simulink model "final"  (R2020a)
(part 7 of 10)

  "IW{1,1}(873,:)'" : Constant  Value=[-9.8027652668789784229375072754919528961181640625;-8.181515964342761293437433778308331966400146484375;5.7461951088779432694764182087965309619903564453125]
      mask Display: e = 0.06;c1 = [120 150 230]/255;c2 = ([120 150 230]+0)/383;c3 = ([120 150 230]+128)/383;patch([0 1 1 0],[0 0 1 1],c1);patch([0 1 1 1-e 1-e 0+e],[0 0 1 1-e 0+e 0+e],c2);patch([0 0 1 1-e 0+e 0+e],[0 1 1 1-e 1-e 0+e],c3);plot([0 1 1 0 0],[0 0 1 1 0]);disp('Weights');
  "IW{1,1}(874,:)'" : Constant  Value=[-5.7445898955294705245933073456399142742156982421875;11.1345368451311177437901278608478605747222900390625;-6.17189644151374494640549528412520885467529296875]
      mask Display: e = 0.06;c1 = [120 150 230]/255;c2 = ([120 150 230]+0)/383;c3 = ([120 150 230]+128)/383;patch([0 1 1 0],[0 0 1 1],c1);patch([0 1 1 1-e 1-e 0+e],[0 0 1 1-e 0+e 0+e],c2);patch([0 0 1 1-e 0+e 0+e],[0 1 1 1-e 1-e 0+e],c3);plot([0 1 1 0 0],[0 0 1 1 0]);disp('Weights');
  "IW{1,1}(875,:)'" : Constant  Value=[-10.2893978529146945533057078137062489986419677734375;4.09259600744367180169547282275743782520294189453125;8.5661448372303485854217797168530523777008056640625]
      mask Display: e = 0.06;c1 = [120 150 230]/255;c2 = ([120 150 230]+0)/383;c3 = ([120 150 230]+128)/383;patch([0 1 1 0],[0 0 1 1],c1);patch([0 1 1 1-e 1-e 0+e],[0 0 1 1-e 0+e 0+e],c2);patch([0 0 1 1-e 0+e 0+e],[0 1 1 1-e 1-e 0+e],c3);plot([0 1 1 0 0],[0 0 1 1 0]);disp('Weights');
  "IW{1,1}(876,:)'" : Constant  Value=[9.80930660810105337077402509748935699462890625;-6.20453554052230149551405702368356287479400634765625;-7.82823397239459506380399034242145717144012451171875]
      mask Display: e = 0.06;c1 = [120 150 230]/255;c2 = ([120 150 230]+0)/383;c3 = ([120 150 230]+128)/383;patch([0 1 1 0],[0 0 1 1],c1);patch([0 1 1 1-e 1-e 0+e],[0 0 1 1-e 0+e 0+e],c2);patch([0 0 1 1-e 0+e 0+e],[0 1 1 1-e 1-e 0+e],c3);plot([0 1 1 0 0],[0 0 1 1 0]);disp('Weights');
  "IW{1,1}(877,:)'" : Constant  Value=[2.200413892218112010823460877873003482818603515625;-8.73546808790955964241220499388873577117919921875;-10.7167992974565589037183599430136382579803466796875]
      mask Display: e = 0.06;c1 = [120 150 230]/255;c2 = ([120 150 230]+0)/383;c3 = ([120 150 230]+128)/383;patch([0 1 1 0],[0 0 1 1],c1);patch([0 1 1 1-e 1-e 0+e],[0 0 1 1-e 0+e 0+e],c2);patch([0 0 1 1-e 0+e 0+e],[0 1 1 1-e 1-e 0+e],c3);plot([0 1 1 0 0],[0 0 1 1 0]);disp('Weights');
  "IW{1,1}(878,:)'" : Constant  Value=[6.01489267863071130904017991269938647747039794921875;-12.1962535648401608767699144664220511913299560546875;-2.99566370474825927061601760215125977993011474609375]
      mask Display: e = 0.06;c1 = [120 150 230]/255;c2 = ([120 150 230]+0)/383;c3 = ([120 150 230]+128)/383;patch([0 1 1 0],[0 0 1 1],c1);patch([0 1 1 1-e 1-e 0+e],[0 0 1 1-e 0+e 0+e],c2);patch([0 0 1 1-e 0+e 0+e],[0 1 1 1-e 1-e 0+e],c3);plot([0 1 1 0 0],[0 0 1 1 0]);disp('Weights');
  "IW{1,1}(879,:)'" : Constant  Value=[-2.56788966638844495804505640990100800991058349609375;-2.485447747803971818569834795198403298854827880859375;13.5410023272345227951518609188497066497802734375]
      mask Display: e = 0.06;c1 = [120 150 230]/255;c2 = ([120 150 230]+0)/383;c3 = ([120 150 230]+128)/383;patch([0 1 1 0],[0 0 1 1],c1);patch([0 1 1 1-e 1-e 0+e],[0 0 1 1-e 0+e 0+e],c2);patch([0 0 1 1-e 0+e 0+e],[0 1 1 1-e 1-e 0+e],c3);plot([0 1 1 0 0],[0 0 1 1 0]);disp('Weights');
  "IW{1,1}(88,:)'" : Constant  Value=[-13.0007109058881713536948154796846210956573486328125;-4.45296506195250163528953635250218212604522705078125;-2.107556792437728088174253571196459233760833740234375]
      mask Display: e = 0.06;c1 = [120 150 230]/255;c2 = ([120 150 230]+0)/383;c3 = ([120 150 230]+128)/383;patch([0 1 1 0],[0 0 1 1],c1);patch([0 1 1 1-e 1-e 0+e],[0 0 1 1-e 0+e 0+e],c2);patch([0 0 1 1-e 0+e 0+e],[0 1 1 1-e 1-e 0+e],c3);plot([0 1 1 0 0],[0 0 1 1 0]);disp('Weights');
  "IW{1,1}(880,:)'" : Constant  Value=[-6.63574751930846051806156538077630102634429931640625;12.2681000579207282186189331696368753910064697265625;1.21885326286112682936391138355247676372528076171875]
      mask Display: e = 0.06;c1 = [120 150 230]/255;c2 = ([120 150 230]+0)/383;c3 = ([120 150 230]+128)/383;patch([0 1 1 0],[0 0 1 1],c1);patch([0 1 1 1-e 1-e 0+e],[0 0 1 1-e 0+e 0+e],c2);patch([0 0 1 1-e 0+e 0+e],[0 1 1 1-e 1-e 0+e],c3);plot([0 1 1 0 0],[0 0 1 1 0]);disp('Weights');
  "IW{1,1}(881,:)'" : Constant  Value=[-9.42565002354735526068907347507774829864501953125;7.09810269286810235911389099783264100551605224609375;-7.53811060296031687499862528056837618350982666015625]
      mask Display: e = 0.06;c1 = [120 150 230]/255;c2 = ([120 150 230]+0)/383;c3 = ([120 150 230]+128)/383;patch([0 1 1 0],[0 0 1 1],c1);patch([0 1 1 1-e 1-e 0+e],[0 0 1 1-e 0+e 0+e],c2);patch([0 0 1 1-e 0+e 0+e],[0 1 1 1-e 1-e 0+e],c3);plot([0 1 1 0 0],[0 0 1 1 0]);disp('Weights');
  "IW{1,1}(882,:)'" : Constant  Value=[-10.503026471660813712105664308182895183563232421875;7.87536749717003647930368970264680683612823486328125;4.86467625343957177364018207299523055553436279296875]
      mask Display: e = 0.06;c1 = [120 150 230]/255;c2 = ([120 150 230]+0)/383;c3 = ([120 150 230]+128)/383;patch([0 1 1 0],[0 0 1 1],c1);patch([0 1 1 1-e 1-e 0+e],[0 0 1 1-e 0+e 0+e],c2);patch([0 0 1 1-e 0+e 0+e],[0 1 1 1-e 1-e 0+e],c3);plot([0 1 1 0 0],[0 0 1 1 0]);disp('Weights');
  "IW{1,1}(883,:)'" : Constant  Value=[11.59889455159891014091044780798256397247314453125;-0.472588847062044459246266114860191009938716888427734375;7.90251551685965925031496226438321173191070556640625]
      mask Display: e = 0.06;c1 = [120 150 230]/255;c2 = ([120 150 230]+0)/383;c3 = ([120 150 230]+128)/383;patch([0 1 1 0],[0 0 1 1],c1);patch([0 1 1 1-e 1-e 0+e],[0 0 1 1-e 0+e 0+e],c2);patch([0 0 1 1-e 0+e 0+e],[0 1 1 1-e 1-e 0+e],c3);plot([0 1 1 0 0],[0 0 1 1 0]);disp('Weights');
  "IW{1,1}(884,:)'" : Constant  Value=[-7.8233264355279512614060877240262925624847412109375;-4.5123480679777987489842416835017502307891845703125;-10.6900295573040740038095464115031063556671142578125]
      mask Display: e = 0.06;c1 = [120 150 230]/255;c2 = ([120 150 230]+0)/383;c3 = ([120 150 230]+128)/383;patch([0 1 1 0],[0 0 1 1],c1);patch([0 1 1 1-e 1-e 0+e],[0 0 1 1-e 0+e 0+e],c2);patch([0 0 1 1-e 0+e 0+e],[0 1 1 1-e 1-e 0+e],c3);plot([0 1 1 0 0],[0 0 1 1 0]);disp('Weights');
  "IW{1,1}(885,:)'" : Constant  Value=[-10.0528205132678589706074490095488727092742919921875;2.28952938369679248609145361115224659442901611328125;9.47097011277430311793068540282547473907470703125]
      mask Display: e = 0.06;c1 = [120 150 230]/255;c2 = ([120 150 230]+0)/383;c3 = ([120 150 230]+128)/383;patch([0 1 1 0],[0 0 1 1],c1);patch([0 1 1 1-e 1-e 0+e],[0 0 1 1-e 0+e 0+e],c2);patch([0 0 1 1-e 0+e 0+e],[0 1 1 1-e 1-e 0+e],c3);plot([0 1 1 0 0],[0 0 1 1 0]);disp('Weights');
  "IW{1,1}(886,:)'" : Constant  Value=[5.18606746800024698274000911624170839786529541015625;12.4953529390770849971659117727540433406829833984375;3.601878552920694698258330390672199428081512451171875]
      mask Display: e = 0.06;c1 = [120 150 230]/255;c2 = ([120 150 230]+0)/383;c3 = ([120 150 230]+128)/383;patch([0 1 1 0],[0 0 1 1],c1);patch([0 1 1 1-e 1-e 0+e],[0 0 1 1-e 0+e 0+e],c2);patch([0 0 1 1-e 0+e 0+e],[0 1 1 1-e 1-e 0+e],c3);plot([0 1 1 0 0],[0 0 1 1 0]);disp('Weights');
  "IW{1,1}(887,:)'" : Constant  Value=[-1.6211095982892038680489577018306590616703033447265625;-8.6710083047681454360144925885833799839019775390625;10.8639394314123283180606449604965746402740478515625]
      mask Display: e = 0.06;c1 = [120 150 230]/255;c2 = ([120 150 230]+0)/383;c3 = ([120 150 230]+128)/383;patch([0 1 1 0],[0 0 1 1],c1);patch([0 1 1 1-e 1-e 0+e],[0 0 1 1-e 0+e 0+e],c2);patch([0 0 1 1-e 0+e 0+e],[0 1 1 1-e 1-e 0+e],c3);plot([0 1 1 0 0],[0 0 1 1 0]);disp('Weights');
  "IW{1,1}(888,:)'" : Constant  Value=[6.90013802371518192302346506039611995220184326171875;-12.139383490560522460555148427374660968780517578125;-1.010692573154347684294407372362911701202392578125]
      mask Display: e = 0.06;c1 = [120 150 230]/255;c2 = ([120 150 230]+0)/383;c3 = ([120 150 230]+128)/383;patch([0 1 1 0],[0 0 1 1],c1);patch([0 1 1 1-e 1-e 0+e],[0 0 1 1-e 0+e 0+e],c2);patch([0 0 1 1-e 0+e 0+e],[0 1 1 1-e 1-e 0+e],c3);plot([0 1 1 0 0],[0 0 1 1 0]);disp('Weights');
  "IW{1,1}(889,:)'" : Constant  Value=[-3.328354407273355075602694341796450316905975341796875;3.7640532156676496100544682121835649013519287109375;13.0622865083349051218419845099560916423797607421875]
      mask Display: e = 0.06;c1 = [120 150 230]/255;c2 = ([120 150 230]+0)/383;c3 = ([120 150 230]+128)/383;patch([0 1 1 0],[0 0 1 1],c1);patch([0 1 1 1-e 1-e 0+e],[0 0 1 1-e 0+e 0+e],c2);patch([0 0 1 1-e 0+e 0+e],[0 1 1 1-e 1-e 0+e],c3);plot([0 1 1 0 0],[0 0 1 1 0]);disp('Weights');
  "IW{1,1}(89,:)'" : Constant  Value=[-10.6442399539643215433670775382779538631439208984375;8.5703930102248619959937059320509433746337890625;3.03962852795012761220050379051826894283294677734375]
      mask Display: e = 0.06;c1 = [120 150 230]/255;c2 = ([120 150 230]+0)/383;c3 = ([120 150 230]+128)/383;patch([0 1 1 0],[0 0 1 1],c1);patch([0 1 1 1-e 1-e 0+e],[0 0 1 1-e 0+e 0+e],c2);patch([0 0 1 1-e 0+e 0+e],[0 1 1 1-e 1-e 0+e],c3);plot([0 1 1 0 0],[0 0 1 1 0]);disp('Weights');
  "IW{1,1}(890,:)'" : Constant  Value=[7.55991374883076705515350113273598253726959228515625;-11.169555353358713745137720252387225627899169921875;3.7468274148343372331737555214203894138336181640625]
      mask Display: e = 0.06;c1 = [120 150 230]/255;c2 = ([120 150 230]+0)/383;c3 = ([120 150 230]+128)/383;patch([0 1 1 0],[0 0 1 1],c1);patch([0 1 1 1-e 1-e 0+e],[0 0 1 1-e 0+e 0+e],c2);patch([0 0 1 1-e 0+e 0+e],[0 1 1 1-e 1-e 0+e],c3);plot([0 1 1 0 0],[0 0 1 1 0]);disp('Weights');
  "IW{1,1}(891,:)'" : Constant  Value=[-1.8380103381601846646020703701651655137538909912109375;13.92634572211004950759161147288978099822998046875;-1.2000628577076482006447122330428101122379302978515625]
      mask Display: e = 0.06;c1 = [120 150 230]/255;c2 = ([120 150 230]+0)/383;c3 = ([120 150 230]+128)/383;patch([0 1 1 0],[0 0 1 1],c1);patch([0 1 1 1-e 1-e 0+e],[0 0 1 1-e 0+e 0+e],c2);patch([0 0 1 1-e 0+e 0+e],[0 1 1 1-e 1-e 0+e],c3);plot([0 1 1 0 0],[0 0 1 1 0]);disp('Weights');
  "IW{1,1}(892,:)'" : Constant  Value=[7.488711085657055122055680840276181697845458984375;-4.72483464117714735408526394166983664035797119140625;-10.84817452639412493908821488730609416961669921875]
      mask Display: e = 0.06;c1 = [120 150 230]/255;c2 = ([120 150 230]+0)/383;c3 = ([120 150 230]+128)/383;patch([0 1 1 0],[0 0 1 1],c1);patch([0 1 1 1-e 1-e 0+e],[0 0 1 1-e 0+e 0+e],c2);patch([0 0 1 1-e 0+e 0+e],[0 1 1 1-e 1-e 0+e],c3);plot([0 1 1 0 0],[0 0 1 1 0]);disp('Weights');
  "IW{1,1}(893,:)'" : Constant  Value=[8.136717651057740141595786553807556629180908203125;-3.017278169304517643212193434010259807109832763671875;10.9859096183062536766783523489721119403839111328125]
      mask Display: e = 0.06;c1 = [120 150 230]/255;c2 = ([120 150 230]+0)/383;c3 = ([120 150 230]+128)/383;patch([0 1 1 0],[0 0 1 1],c1);patch([0 1 1 1-e 1-e 0+e],[0 0 1 1-e 0+e 0+e],c2);patch([0 0 1 1-e 0+e 0+e],[0 1 1 1-e 1-e 0+e],c3);plot([0 1 1 0 0],[0 0 1 1 0]);disp('Weights');
  "IW{1,1}(894,:)'" : Constant  Value=[-7.78308222446040343101003600168041884899139404296875;10.038484120077104222445996128953993320465087890625;5.89362524115581987160794597002677619457244873046875]
      mask Display: e = 0.06;c1 = [120 150 230]/255;c2 = ([120 150 230]+0)/383;c3 = ([120 150 230]+128)/383;patch([0 1 1 0],[0 0 1 1],c1);patch([0 1 1 1-e 1-e 0+e],[0 0 1 1-e 0+e 0+e],c2);patch([0 0 1 1-e 0+e 0+e],[0 1 1 1-e 1-e 0+e],c3);plot([0 1 1 0 0],[0 0 1 1 0]);disp('Weights');
  "IW{1,1}(895,:)'" : Constant  Value=[2.32278357868067519831356548820622265338897705078125;-3.56836155980005020893486289423890411853790283203125;-13.334159874566534398354633594863116741180419921875]
      mask Display: e = 0.06;c1 = [120 150 230]/255;c2 = ([120 150 230]+0)/383;c3 = ([120 150 230]+128)/383;patch([0 1 1 0],[0 0 1 1],c1);patch([0 1 1 1-e 1-e 0+e],[0 0 1 1-e 0+e 0+e],c2);patch([0 0 1 1-e 0+e 0+e],[0 1 1 1-e 1-e 0+e],c3);plot([0 1 1 0 0],[0 0 1 1 0]);disp('Weights');
  "IW{1,1}(896,:)'" : Constant  Value=[6.95827300629331713111014323658309876918792724609375;8.05468047049127022773973294533789157867431640625;9.094225364258061716782322037033736705780029296875]
      mask Display: e = 0.06;c1 = [120 150 230]/255;c2 = ([120 150 230]+0)/383;c3 = ([120 150 230]+128)/383;patch([0 1 1 0],[0 0 1 1],c1);patch([0 1 1 1-e 1-e 0+e],[0 0 1 1-e 0+e 0+e],c2);patch([0 0 1 1-e 0+e 0+e],[0 1 1 1-e 1-e 0+e],c3);plot([0 1 1 0 0],[0 0 1 1 0]);disp('Weights');
  "IW{1,1}(897,:)'" : Constant  Value=[-8.6136429828129923436108583700843155384063720703125;-10.879247295266527117973964777775108814239501953125;1.8607910188423684161307392059825360774993896484375]
      mask Display: e = 0.06;c1 = [120 150 230]/255;c2 = ([120 150 230]+0)/383;c3 = ([120 150 230]+128)/383;patch([0 1 1 0],[0 0 1 1],c1);patch([0 1 1 1-e 1-e 0+e],[0 0 1 1-e 0+e 0+e],c2);patch([0 0 1 1-e 0+e 0+e],[0 1 1 1-e 1-e 0+e],c3);plot([0 1 1 0 0],[0 0 1 1 0]);disp('Weights');
  "IW{1,1}(898,:)'" : Constant  Value=[-10.1648432915615014593413434340618550777435302734375;0.406442693144960343065719143851310946047306060791015625;9.6125764278742362733964910148642957210540771484375]
      mask Display: e = 0.06;c1 = [120 150 230]/255;c2 = ([120 150 230]+0)/383;c3 = ([120 150 230]+128)/383;patch([0 1 1 0],[0 0 1 1],c1);patch([0 1 1 1-e 1-e 0+e],[0 0 1 1-e 0+e 0+e],c2);patch([0 0 1 1-e 0+e 0+e],[0 1 1 1-e 1-e 0+e],c3);plot([0 1 1 0 0],[0 0 1 1 0]);disp('Weights');
  "IW{1,1}(899,:)'" : Constant  Value=[-0.390214419826295344506661422201432287693023681640625;-13.9942636404640143865663048927672207355499267578125;0.11990369897692454426163521929993294179439544677734375]
      mask Display: e = 0.06;c1 = [120 150 230]/255;c2 = ([120 150 230]+0)/383;c3 = ([120 150 230]+128)/383;patch([0 1 1 0],[0 0 1 1],c1);patch([0 1 1 1-e 1-e 0+e],[0 0 1 1-e 0+e 0+e],c2);patch([0 0 1 1-e 0+e 0+e],[0 1 1 1-e 1-e 0+e],c3);plot([0 1 1 0 0],[0 0 1 1 0]);disp('Weights');
  "IW{1,1}(9,:)'" : Constant  Value=[9.688376769642996322318140300922095775604248046875;-10.038655541071417331977499998174607753753662109375;1.1655779423384007298380993233877234160900115966796875]
      mask Display: e = 0.06;c1 = [120 150 230]/255;c2 = ([120 150 230]+0)/383;c3 = ([120 150 230]+128)/383;patch([0 1 1 0],[0 0 1 1],c1);patch([0 1 1 1-e 1-e 0+e],[0 0 1 1-e 0+e 0+e],c2);patch([0 0 1 1-e 0+e 0+e],[0 1 1 1-e 1-e 0+e],c3);plot([0 1 1 0 0],[0 0 1 1 0]);disp('Weights');
  "IW{1,1}(90,:)'" : Constant  Value=[6.53300337557219190642854300676845014095306396484375;-0.86259394507942588337101597062428481876850128173828125;-12.3525189506012811335722290095873177051544189453125]
      mask Display: e = 0.06;c1 = [120 150 230]/255;c2 = ([120 150 230]+0)/383;c3 = ([120 150 230]+128)/383;patch([0 1 1 0],[0 0 1 1],c1);patch([0 1 1 1-e 1-e 0+e],[0 0 1 1-e 0+e 0+e],c2);patch([0 0 1 1-e 0+e 0+e],[0 1 1 1-e 1-e 0+e],c3);plot([0 1 1 0 0],[0 0 1 1 0]);disp('Weights');
  "IW{1,1}(900,:)'" : Constant  Value=[-10.8025181840935058374952859594486653804779052734375;-3.368850064855162695920398618909530341625213623046875;8.24358075803985457241651602089405059814453125]
      mask Display: e = 0.06;c1 = [120 150 230]/255;c2 = ([120 150 230]+0)/383;c3 = ([120 150 230]+128)/383;patch([0 1 1 0],[0 0 1 1],c1);patch([0 1 1 1-e 1-e 0+e],[0 0 1 1-e 0+e 0+e],c2);patch([0 0 1 1-e 0+e 0+e],[0 1 1 1-e 1-e 0+e],c3);plot([0 1 1 0 0],[0 0 1 1 0]);disp('Weights');
  "IW{1,1}(901,:)'" : Constant  Value=[-0.76866160684172513128942227922379970550537109375;9.2111038925345294359203762724064290523529052734375;10.5149866903311863808312409673817455768585205078125]
      mask Display: e = 0.06;c1 = [120 150 230]/255;c2 = ([120 150 230]+0)/383;c3 = ([120 150 230]+128)/383;patch([0 1 1 0],[0 0 1 1],c1);patch([0 1 1 1-e 1-e 0+e],[0 0 1 1-e 0+e 0+e],c2);patch([0 0 1 1-e 0+e 0+e],[0 1 1 1-e 1-e 0+e],c3);plot([0 1 1 0 0],[0 0 1 1 0]);disp('Weights');
  "IW{1,1}(902,:)'" : Constant  Value=[-3.70479587984004776757274157716892659664154052734375;-5.5042567546616769647016553790308535099029541015625;12.3134688525722939544948530965484678745269775390625]
      mask Display: e = 0.06;c1 = [120 150 230]/255;c2 = ([120 150 230]+0)/383;c3 = ([120 150 230]+128)/383;patch([0 1 1 0],[0 0 1 1],c1);patch([0 1 1 1-e 1-e 0+e],[0 0 1 1-e 0+e 0+e],c2);patch([0 0 1 1-e 0+e 0+e],[0 1 1 1-e 1-e 0+e],c3);plot([0 1 1 0 0],[0 0 1 1 0]);disp('Weights');
  "IW{1,1}(903,:)'" : Constant  Value=[2.803501602330331632373372485744766891002655029296875;-13.474408161413379048099159263074398040771484375;-2.81160374085950959255342240794561803340911865234375]
      mask Display: e = 0.06;c1 = [120 150 230]/255;c2 = ([120 150 230]+0)/383;c3 = ([120 150 230]+128)/383;patch([0 1 1 0],[0 0 1 1],c1);patch([0 1 1 1-e 1-e 0+e],[0 0 1 1-e 0+e 0+e],c2);patch([0 0 1 1-e 0+e 0+e],[0 1 1 1-e 1-e 0+e],c3);plot([0 1 1 0 0],[0 0 1 1 0]);disp('Weights');
  "IW{1,1}(904,:)'" : Constant  Value=[-1.066780166753863223760845357901416718959808349609375;10.895749823181404281058348715305328369140625;8.7260825883228445576378362602554261684417724609375]
      mask Display: e = 0.06;c1 = [120 150 230]/255;c2 = ([120 150 230]+0)/383;c3 = ([120 150 230]+128)/383;patch([0 1 1 0],[0 0 1 1],c1);patch([0 1 1 1-e 1-e 0+e],[0 0 1 1-e 0+e 0+e],c2);patch([0 0 1 1-e 0+e 0+e],[0 1 1 1-e 1-e 0+e],c3);plot([0 1 1 0 0],[0 0 1 1 0]);disp('Weights');
  "IW{1,1}(905,:)'" : Constant  Value=[10.6968454989216059658474478055723011493682861328125;2.817139616075630126346140968962572515010833740234375;-8.5792652176447372625034404336474835872650146484375]
      mask Display: e = 0.06;c1 = [120 150 230]/255;c2 = ([120 150 230]+0)/383;c3 = ([120 150 230]+128)/383;patch([0 1 1 0],[0 0 1 1],c1);patch([0 1 1 1-e 1-e 0+e],[0 0 1 1-e 0+e 0+e],c2);patch([0 0 1 1-e 0+e 0+e],[0 1 1 1-e 1-e 0+e],c3);plot([0 1 1 0 0],[0 0 1 1 0]);disp('Weights');
  "IW{1,1}(906,:)'" : Constant  Value=[-3.1491781345618559129206914803944528102874755859375;-2.768592637041312087831101962365210056304931640625;13.3104424411612658474268755526281893253326416015625]
      mask Display: e = 0.06;c1 = [120 150 230]/255;c2 = ([120 150 230]+0)/383;c3 = ([120 150 230]+128)/383;patch([0 1 1 0],[0 0 1 1],c1);patch([0 1 1 1-e 1-e 0+e],[0 0 1 1-e 0+e 0+e],c2);patch([0 0 1 1-e 0+e 0+e],[0 1 1 1-e 1-e 0+e],c3);plot([0 1 1 0 0],[0 0 1 1 0]);disp('Weights');
  "IW{1,1}(907,:)'" : Constant  Value=[1.6069139472749707220344816960277967154979705810546875;9.14982282195177987205170211382210254669189453125;10.472493515332050861843526945449411869049072265625]
      mask Display: e = 0.06;c1 = [120 150 230]/255;c2 = ([120 150 230]+0)/383;c3 = ([120 150 230]+128)/383;patch([0 1 1 0],[0 0 1 1],c1);patch([0 1 1 1-e 1-e 0+e],[0 0 1 1-e 0+e 0+e],c2);patch([0 0 1 1-e 0+e 0+e],[0 1 1 1-e 1-e 0+e],c3);plot([0 1 1 0 0],[0 0 1 1 0]);disp('Weights');
  "IW{1,1}(908,:)'" : Constant  Value=[11.2693052845972747633140897960402071475982666015625;7.867863309541196059626599890179932117462158203125;2.654025860023144556265606297529302537441253662109375]
      mask Display: e = 0.06;c1 = [120 150 230]/255;c2 = ([120 150 230]+0)/383;c3 = ([120 150 230]+128)/383;patch([0 1 1 0],[0 0 1 1],c1);patch([0 1 1 1-e 1-e 0+e],[0 0 1 1-e 0+e 0+e],c2);patch([0 0 1 1-e 0+e 0+e],[0 1 1 1-e 1-e 0+e],c3);plot([0 1 1 0 0],[0 0 1 1 0]);disp('Weights');
  "IW{1,1}(909,:)'" : Constant  Value=[8.4700836988912744374147223425097763538360595703125;8.9019279561255615362824755720794200897216796875;-6.73020319532403465956349464249797165393829345703125]
      mask Display: e = 0.06;c1 = [120 150 230]/255;c2 = ([120 150 230]+0)/383;c3 = ([120 150 230]+128)/383;patch([0 1 1 0],[0 0 1 1],c1);patch([0 1 1 1-e 1-e 0+e],[0 0 1 1-e 0+e 0+e],c2);patch([0 0 1 1-e 0+e 0+e],[0 1 1 1-e 1-e 0+e],c3);plot([0 1 1 0 0],[0 0 1 1 0]);disp('Weights');
  "IW{1,1}(91,:)'" : Constant  Value=[9.685584545070614836959066451527178287506103515625;8.6939351024627189445936892298050224781036376953125;5.1640799118561222513790198718197643756866455078125]
      mask Display: e = 0.06;c1 = [120 150 230]/255;c2 = ([120 150 230]+0)/383;c3 = ([120 150 230]+128)/383;patch([0 1 1 0],[0 0 1 1],c1);patch([0 1 1 1-e 1-e 0+e],[0 0 1 1-e 0+e 0+e],c2);patch([0 0 1 1-e 0+e 0+e],[0 1 1 1-e 1-e 0+e],c3);plot([0 1 1 0 0],[0 0 1 1 0]);disp('Weights');
  "IW{1,1}(910,:)'" : Constant  Value=[1.2397532912573734353856025336426682770252227783203125;-12.3610048970112398336596015724353492259979248046875;6.4523855454746676940658289822749793529510498046875]
      mask Display: e = 0.06;c1 = [120 150 230]/255;c2 = ([120 150 230]+0)/383;c3 = ([120 150 230]+128)/383;patch([0 1 1 0],[0 0 1 1],c1);patch([0 1 1 1-e 1-e 0+e],[0 0 1 1-e 0+e 0+e],c2);patch([0 0 1 1-e 0+e 0+e],[0 1 1 1-e 1-e 0+e],c3);plot([0 1 1 0 0],[0 0 1 1 0]);disp('Weights');
  "IW{1,1}(911,:)'" : Constant  Value=[-5.924831144793220261135502369143068790435791015625;8.2445246882423521839200475369580090045928955078125;-9.6147247852049151362052725744433701038360595703125]
      mask Display: e = 0.06;c1 = [120 150 230]/255;c2 = ([120 150 230]+0)/383;c3 = ([120 150 230]+128)/383;patch([0 1 1 0],[0 0 1 1],c1);patch([0 1 1 1-e 1-e 0+e],[0 0 1 1-e 0+e 0+e],c2);patch([0 0 1 1-e 0+e 0+e],[0 1 1 1-e 1-e 0+e],c3);plot([0 1 1 0 0],[0 0 1 1 0]);disp('Weights');
  "IW{1,1}(912,:)'" : Constant  Value=[-3.653212682315569281854550354182720184326171875;9.056267292606111851682726410217583179473876953125;10.0318341443112064581555387121625244617462158203125]
      mask Display: e = 0.06;c1 = [120 150 230]/255;c2 = ([120 150 230]+0)/383;c3 = ([120 150 230]+128)/383;patch([0 1 1 0],[0 0 1 1],c1);patch([0 1 1 1-e 1-e 0+e],[0 0 1 1-e 0+e 0+e],c2);patch([0 0 1 1-e 0+e 0+e],[0 1 1 1-e 1-e 0+e],c3);plot([0 1 1 0 0],[0 0 1 1 0]);disp('Weights');
  "IW{1,1}(913,:)'" : Constant  Value=[7.11187516767271432627239846624433994293212890625;-2.889804948245539240048174178809858858585357666015625;11.7073213071604964596872378024272620677947998046875]
      mask Display: e = 0.06;c1 = [120 150 230]/255;c2 = ([120 150 230]+0)/383;c3 = ([120 150 230]+128)/383;patch([0 1 1 0],[0 0 1 1],c1);patch([0 1 1 1-e 1-e 0+e],[0 0 1 1-e 0+e 0+e],c2);patch([0 0 1 1-e 0+e 0+e],[0 1 1 1-e 1-e 0+e],c3);plot([0 1 1 0 0],[0 0 1 1 0]);disp('Weights');
  "IW{1,1}(914,:)'" : Constant  Value=[11.525345665528529792709377943538129329681396484375;-0.614496525731584863905254678684286773204803466796875;-7.92530564785023017293497105129063129425048828125]
      mask Display: e = 0.06;c1 = [120 150 230]/255;c2 = ([120 150 230]+0)/383;c3 = ([120 150 230]+128)/383;patch([0 1 1 0],[0 0 1 1],c1);patch([0 1 1 1-e 1-e 0+e],[0 0 1 1-e 0+e 0+e],c2);patch([0 0 1 1-e 0+e 0+e],[0 1 1 1-e 1-e 0+e],c3);plot([0 1 1 0 0],[0 0 1 1 0]);disp('Weights');
  "IW{1,1}(915,:)'" : Constant  Value=[-0.9905336661941586129387360415421426296234130859375;-12.2117643064288170506870301323942840099334716796875;6.77484823617582687660387819050811231136322021484375]
      mask Display: e = 0.06;c1 = [120 150 230]/255;c2 = ([120 150 230]+0)/383;c3 = ([120 150 230]+128)/383;patch([0 1 1 0],[0 0 1 1],c1);patch([0 1 1 1-e 1-e 0+e],[0 0 1 1-e 0+e 0+e],c2);patch([0 0 1 1-e 0+e 0+e],[0 1 1 1-e 1-e 0+e],c3);plot([0 1 1 0 0],[0 0 1 1 0]);disp('Weights');
  "IW{1,1}(916,:)'" : Constant  Value=[10.9259783267315828680921185878105461597442626953125;-2.155774361408119066396693597198463976383209228515625;8.483241762343144642954939627088606357574462890625]
      mask Display: e = 0.06;c1 = [120 150 230]/255;c2 = ([120 150 230]+0)/383;c3 = ([120 150 230]+128)/383;patch([0 1 1 0],[0 0 1 1],c1);patch([0 1 1 1-e 1-e 0+e],[0 0 1 1-e 0+e 0+e],c2);patch([0 0 1 1-e 0+e 0+e],[0 1 1 1-e 1-e 0+e],c3);plot([0 1 1 0 0],[0 0 1 1 0]);disp('Weights');
  "IW{1,1}(917,:)'" : Constant  Value=[-1.5145512795781110870763086495571769773960113525390625;8.1430708152556849910297387395985424518585205078125;-11.2907473797893356248778218287043273448944091796875]
      mask Display: e = 0.06;c1 = [120 150 230]/255;c2 = ([120 150 230]+0)/383;c3 = ([120 150 230]+128)/383;patch([0 1 1 0],[0 0 1 1],c1);patch([0 1 1 1-e 1-e 0+e],[0 0 1 1-e 0+e 0+e],c2);patch([0 0 1 1-e 0+e 0+e],[0 1 1 1-e 1-e 0+e],c3);plot([0 1 1 0 0],[0 0 1 1 0]);disp('Weights');
  "IW{1,1}(918,:)'" : Constant  Value=[-11.5802204299811677401521592400968074798583984375;-5.7988101601208033031298327841795980930328369140625;5.24684290791995433522743041976355016231536865234375]
      mask Display: e = 0.06;c1 = [120 150 230]/255;c2 = ([120 150 230]+0)/383;c3 = ([120 150 230]+128)/383;patch([0 1 1 0],[0 0 1 1],c1);patch([0 1 1 1-e 1-e 0+e],[0 0 1 1-e 0+e 0+e],c2);patch([0 0 1 1-e 0+e 0+e],[0 1 1 1-e 1-e 0+e],c3);plot([0 1 1 0 0],[0 0 1 1 0]);disp('Weights');
  "IW{1,1}(919,:)'" : Constant  Value=[-10.4195268211922158485549516626633703708648681640625;-2.619403194665216094705328941927291452884674072265625;-8.9425686567243598545928762177936732769012451171875]
      mask Display: e = 0.06;c1 = [120 150 230]/255;c2 = ([120 150 230]+0)/383;c3 = ([120 150 230]+128)/383;patch([0 1 1 0],[0 0 1 1],c1);patch([0 1 1 1-e 1-e 0+e],[0 0 1 1-e 0+e 0+e],c2);patch([0 0 1 1-e 0+e 0+e],[0 1 1 1-e 1-e 0+e],c3);plot([0 1 1 0 0],[0 0 1 1 0]);disp('Weights');
  "IW{1,1}(92,:)'" : Constant  Value=[3.697169645974185403503042834927327930927276611328125;9.43340525091827686310352873988449573516845703125;-9.661357896094411756848785444162786006927490234375]
      mask Display: e = 0.06;c1 = [120 150 230]/255;c2 = ([120 150 230]+0)/383;c3 = ([120 150 230]+128)/383;patch([0 1 1 0],[0 0 1 1],c1);patch([0 1 1 1-e 1-e 0+e],[0 0 1 1-e 0+e 0+e],c2);patch([0 0 1 1-e 0+e 0+e],[0 1 1 1-e 1-e 0+e],c3);plot([0 1 1 0 0],[0 0 1 1 0]);disp('Weights');
  "IW{1,1}(920,:)'" : Constant  Value=[-4.5356686788240363483737382921390235424041748046875;-11.3963221737081408235781054827384650707244873046875;6.783471210860216871196826105006039142608642578125]
      mask Display: e = 0.06;c1 = [120 150 230]/255;c2 = ([120 150 230]+0)/383;c3 = ([120 150 230]+128)/383;patch([0 1 1 0],[0 0 1 1],c1);patch([0 1 1 1-e 1-e 0+e],[0 0 1 1-e 0+e 0+e],c2);patch([0 0 1 1-e 0+e 0+e],[0 1 1 1-e 1-e 0+e],c3);plot([0 1 1 0 0],[0 0 1 1 0]);disp('Weights');
  "IW{1,1}(921,:)'" : Constant  Value=[7.5673434272360555752356958691962063312530517578125;10.70721326099781123275533900596201419830322265625;4.86442063186388917728208980406634509563446044921875]
      mask Display: e = 0.06;c1 = [120 150 230]/255;c2 = ([120 150 230]+0)/383;c3 = ([120 150 230]+128)/383;patch([0 1 1 0],[0 0 1 1],c1);patch([0 1 1 1-e 1-e 0+e],[0 0 1 1-e 0+e 0+e],c2);patch([0 0 1 1-e 0+e 0+e],[0 1 1 1-e 1-e 0+e],c3);plot([0 1 1 0 0],[0 0 1 1 0]);disp('Weights');
  "IW{1,1}(922,:)'" : Constant  Value=[-8.474813930141568363296755705960094928741455078125;-8.6597167780356247845929829054512083530426025390625;-7.0132671053710975428430174360983073711395263671875]
      mask Display: e = 0.06;c1 = [120 150 230]/255;c2 = ([120 150 230]+0)/383;c3 = ([120 150 230]+128)/383;patch([0 1 1 0],[0 0 1 1],c1);patch([0 1 1 1-e 1-e 0+e],[0 0 1 1-e 0+e 0+e],c2);patch([0 0 1 1-e 0+e 0+e],[0 1 1 1-e 1-e 0+e],c3);plot([0 1 1 0 0],[0 0 1 1 0]);disp('Weights');
  "IW{1,1}(923,:)'" : Constant  Value=[12.781316439431204656784757389687001705169677734375;-1.0139294360035695508059916392085142433643341064453125;-5.49759165655075943135443594655953347682952880859375]
      mask Display: e = 0.06;c1 = [120 150 230]/255;c2 = ([120 150 230]+0)/383;c3 = ([120 150 230]+128)/383;patch([0 1 1 0],[0 0 1 1],c1);patch([0 1 1 1-e 1-e 0+e],[0 0 1 1-e 0+e 0+e],c2);patch([0 0 1 1-e 0+e 0+e],[0 1 1 1-e 1-e 0+e],c3);plot([0 1 1 0 0],[0 0 1 1 0]);disp('Weights');
  "IW{1,1}(924,:)'" : Constant  Value=[-3.680484384278277953939095823443494737148284912109375;-12.7545399399119094852039779652841389179229736328125;-4.44714219913414421370134732569567859172821044921875]
      mask Display: e = 0.06;c1 = [120 150 230]/255;c2 = ([120 150 230]+0)/383;c3 = ([120 150 230]+128)/383;patch([0 1 1 0],[0 0 1 1],c1);patch([0 1 1 1-e 1-e 0+e],[0 0 1 1-e 0+e 0+e],c2);patch([0 0 1 1-e 0+e 0+e],[0 1 1 1-e 1-e 0+e],c3);plot([0 1 1 0 0],[0 0 1 1 0]);disp('Weights');
  "IW{1,1}(925,:)'" : Constant  Value=[7.16499115985981749332722756662406027317047119140625;-9.9246306787782341274350983439944684505462646484375;-6.7902089757849797280186976422555744647979736328125]
      mask Display: e = 0.06;c1 = [120 150 230]/255;c2 = ([120 150 230]+0)/383;c3 = ([120 150 230]+128)/383;patch([0 1 1 0],[0 0 1 1],c1);patch([0 1 1 1-e 1-e 0+e],[0 0 1 1-e 0+e 0+e],c2);patch([0 0 1 1-e 0+e 0+e],[0 1 1 1-e 1-e 0+e],c3);plot([0 1 1 0 0],[0 0 1 1 0]);disp('Weights');
  "IW{1,1}(926,:)'" : Constant  Value=[-6.93633441218447188703066785819828510284423828125;-1.5119477301327821638921022895374335348606109619140625;12.066459604768471791658157599158585071563720703125]
      mask Display: e = 0.06;c1 = [120 150 230]/255;c2 = ([120 150 230]+0)/383;c3 = ([120 150 230]+128)/383;patch([0 1 1 0],[0 0 1 1],c1);patch([0 1 1 1-e 1-e 0+e],[0 0 1 1-e 0+e 0+e],c2);patch([0 0 1 1-e 0+e 0+e],[0 1 1 1-e 1-e 0+e],c3);plot([0 1 1 0 0],[0 0 1 1 0]);disp('Weights');
  "IW{1,1}(927,:)'" : Constant  Value=[4.01548700812378012159342688391916453838348388671875;5.47349129554760427396331579075194895267486572265625;-12.207766596957302596138106309808790683746337890625]
      mask Display: e = 0.06;c1 = [120 150 230]/255;c2 = ([120 150 230]+0)/383;c3 = ([120 150 230]+128)/383;patch([0 1 1 0],[0 0 1 1],c1);patch([0 1 1 1-e 1-e 0+e],[0 0 1 1-e 0+e 0+e],c2);patch([0 0 1 1-e 0+e 0+e],[0 1 1 1-e 1-e 0+e],c3);plot([0 1 1 0 0],[0 0 1 1 0]);disp('Weights');
  "IW{1,1}(928,:)'" : Constant  Value=[7.3154305425002377205601078458130359649658203125;-7.590445547334088161051113274879753589630126953125;-9.21170254208840333376429043710231781005859375]
      mask Display: e = 0.06;c1 = [120 150 230]/255;c2 = ([120 150 230]+0)/383;c3 = ([120 150 230]+128)/383;patch([0 1 1 0],[0 0 1 1],c1);patch([0 1 1 1-e 1-e 0+e],[0 0 1 1-e 0+e 0+e],c2);patch([0 0 1 1-e 0+e 0+e],[0 1 1 1-e 1-e 0+e],c3);plot([0 1 1 0 0],[0 0 1 1 0]);disp('Weights');
  "IW{1,1}(929,:)'" : Constant  Value=[-3.8517529529626610695913768722675740718841552734375;-10.2855173528930965431982258451171219348907470703125;-8.7019707211736250229705547099001705646514892578125]
      mask Display: e = 0.06;c1 = [120 150 230]/255;c2 = ([120 150 230]+0)/383;c3 = ([120 150 230]+128)/383;patch([0 1 1 0],[0 0 1 1],c1);patch([0 1 1 1-e 1-e 0+e],[0 0 1 1-e 0+e 0+e],c2);patch([0 0 1 1-e 0+e 0+e],[0 1 1 1-e 1-e 0+e],c3);plot([0 1 1 0 0],[0 0 1 1 0]);disp('Weights');
  "IW{1,1}(93,:)'" : Constant  Value=[-5.79945408804851059159091164474375545978546142578125;2.05254933921406834684830755577422678470611572265625;12.57630390558579591697707655839622020721435546875]
      mask Display: e = 0.06;c1 = [120 150 230]/255;c2 = ([120 150 230]+0)/383;c3 = ([120 150 230]+128)/383;patch([0 1 1 0],[0 0 1 1],c1);patch([0 1 1 1-e 1-e 0+e],[0 0 1 1-e 0+e 0+e],c2);patch([0 0 1 1-e 0+e 0+e],[0 1 1 1-e 1-e 0+e],c3);plot([0 1 1 0 0],[0 0 1 1 0]);disp('Weights');
  "IW{1,1}(930,:)'" : Constant  Value=[-6.80356971503967589143258010153658688068389892578125;9.2142956760537941818256513215601444244384765625;8.060977350672768437789272866211831569671630859375]
      mask Display: e = 0.06;c1 = [120 150 230]/255;c2 = ([120 150 230]+0)/383;c3 = ([120 150 230]+128)/383;patch([0 1 1 0],[0 0 1 1],c1);patch([0 1 1 1-e 1-e 0+e],[0 0 1 1-e 0+e 0+e],c2);patch([0 0 1 1-e 0+e 0+e],[0 1 1 1-e 1-e 0+e],c3);plot([0 1 1 0 0],[0 0 1 1 0]);disp('Weights');
  "IW{1,1}(931,:)'" : Constant  Value=[13.1151471006181878919960581697523593902587890625;4.73336813536885703257439672597683966159820556640625;-1.12578837776077733678903314284980297088623046875]
      mask Display: e = 0.06;c1 = [120 150 230]/255;c2 = ([120 150 230]+0)/383;c3 = ([120 150 230]+128)/383;patch([0 1 1 0],[0 0 1 1],c1);patch([0 1 1 1-e 1-e 0+e],[0 0 1 1-e 0+e 0+e],c2);patch([0 0 1 1-e 0+e 0+e],[0 1 1 1-e 1-e 0+e],c3);plot([0 1 1 0 0],[0 0 1 1 0]);disp('Weights');
  "IW{1,1}(932,:)'" : Constant  Value=[-5.52401554301332264884649703162722289562225341796875;11.2878394977545344346481215325184166431427001953125;6.08124620630011225586031287093646824359893798828125]
      mask Display: e = 0.06;c1 = [120 150 230]/255;c2 = ([120 150 230]+0)/383;c3 = ([120 150 230]+128)/383;patch([0 1 1 0],[0 0 1 1],c1);patch([0 1 1 1-e 1-e 0+e],[0 0 1 1-e 0+e 0+e],c2);patch([0 0 1 1-e 0+e 0+e],[0 1 1 1-e 1-e 0+e],c3);plot([0 1 1 0 0],[0 0 1 1 0]);disp('Weights');
  "IW{1,1}(933,:)'" : Constant  Value=[-7.64265844916061443115040674456395208835601806640625;9.6460448426971669988461144384928047657012939453125;6.6734026681342459852430692990310490131378173828125]
      mask Display: e = 0.06;c1 = [120 150 230]/255;c2 = ([120 150 230]+0)/383;c3 = ([120 150 230]+128)/383;patch([0 1 1 0],[0 0 1 1],c1);patch([0 1 1 1-e 1-e 0+e],[0 0 1 1-e 0+e 0+e],c2);patch([0 0 1 1-e 0+e 0+e],[0 1 1 1-e 1-e 0+e],c3);plot([0 1 1 0 0],[0 0 1 1 0]);disp('Weights');
  "IW{1,1}(934,:)'" : Constant  Value=[3.726440911476270212432382322731427848339080810546875;3.870757082153959860448821928002871572971343994140625;12.927925352635060818329293397255241870880126953125]
      mask Display: e = 0.06;c1 = [120 150 230]/255;c2 = ([120 150 230]+0)/383;c3 = ([120 150 230]+128)/383;patch([0 1 1 0],[0 0 1 1],c1);patch([0 1 1 1-e 1-e 0+e],[0 0 1 1-e 0+e 0+e],c2);patch([0 0 1 1-e 0+e 0+e],[0 1 1 1-e 1-e 0+e],c3);plot([0 1 1 0 0],[0 0 1 1 0]);disp('Weights');
  "IW{1,1}(935,:)'" : Constant  Value=[2.3376881038063803686100072809495031833648681640625;-13.7787745695464156625575924408622086048126220703125;-1.1998179413161607076432346730143763124942779541015625]
      mask Display: e = 0.06;c1 = [120 150 230]/255;c2 = ([120 150 230]+0)/383;c3 = ([120 150 230]+128)/383;patch([0 1 1 0],[0 0 1 1],c1);patch([0 1 1 1-e 1-e 0+e],[0 0 1 1-e 0+e 0+e],c2);patch([0 0 1 1-e 0+e 0+e],[0 1 1 1-e 1-e 0+e],c3);plot([0 1 1 0 0],[0 0 1 1 0]);disp('Weights');
  "IW{1,1}(936,:)'" : Constant  Value=[-0.869837296885993094264222236233763396739959716796875;-10.712564666585702610746011487208306789398193359375;-8.99076670371186992269940674304962158203125]
      mask Display: e = 0.06;c1 = [120 150 230]/255;c2 = ([120 150 230]+0)/383;c3 = ([120 150 230]+128)/383;patch([0 1 1 0],[0 0 1 1],c1);patch([0 1 1 1-e 1-e 0+e],[0 0 1 1-e 0+e 0+e],c2);patch([0 0 1 1-e 0+e 0+e],[0 1 1 1-e 1-e 0+e],c3);plot([0 1 1 0 0],[0 0 1 1 0]);disp('Weights');
  "IW{1,1}(937,:)'" : Constant  Value=[-9.8853570318157011342918849550187587738037109375;-9.4968230248517375713390720193274319171905517578125;2.8443825414661016992567965644411742687225341796875]
      mask Display: e = 0.06;c1 = [120 150 230]/255;c2 = ([120 150 230]+0)/383;c3 = ([120 150 230]+128)/383;patch([0 1 1 0],[0 0 1 1],c1);patch([0 1 1 1-e 1-e 0+e],[0 0 1 1-e 0+e 0+e],c2);patch([0 0 1 1-e 0+e 0+e],[0 1 1 1-e 1-e 0+e],c3);plot([0 1 1 0 0],[0 0 1 1 0]);disp('Weights');
  "IW{1,1}(938,:)'" : Constant  Value=[0.485148563697484380696778316632844507694244384765625;-4.8896183463110585165622978820465505123138427734375;13.105373448596441932068046298809349536895751953125]
      mask Display: e = 0.06;c1 = [120 150 230]/255;c2 = ([120 150 230]+0)/383;c3 = ([120 150 230]+128)/383;patch([0 1 1 0],[0 0 1 1],c1);patch([0 1 1 1-e 1-e 0+e],[0 0 1 1-e 0+e 0+e],c2);patch([0 0 1 1-e 0+e 0+e],[0 1 1 1-e 1-e 0+e],c3);plot([0 1 1 0 0],[0 0 1 1 0]);disp('Weights');
  "IW{1,1}(939,:)'" : Constant  Value=[-9.1494805089451975987913101562298834323883056640625;-10.4115395269174424441871451563201844692230224609375;1.9714888034109383507797019774443469941616058349609375]
      mask Display: e = 0.06;c1 = [120 150 230]/255;c2 = ([120 150 230]+0)/383;c3 = ([120 150 230]+128)/383;patch([0 1 1 0],[0 0 1 1],c1);patch([0 1 1 1-e 1-e 0+e],[0 0 1 1-e 0+e 0+e],c2);patch([0 0 1 1-e 0+e 0+e],[0 1 1 1-e 1-e 0+e],c3);plot([0 1 1 0 0],[0 0 1 1 0]);disp('Weights');
  "IW{1,1}(94,:)'" : Constant  Value=[-7.43277876426049743940893677063286304473876953125;-9.2285918214847928453536951565183699131011962890625;7.4130998663877267773614221368916332721710205078125]
      mask Display: e = 0.06;c1 = [120 150 230]/255;c2 = ([120 150 230]+0)/383;c3 = ([120 150 230]+128)/383;patch([0 1 1 0],[0 0 1 1],c1);patch([0 1 1 1-e 1-e 0+e],[0 0 1 1-e 0+e 0+e],c2);patch([0 0 1 1-e 0+e 0+e],[0 1 1 1-e 1-e 0+e],c3);plot([0 1 1 0 0],[0 0 1 1 0]);disp('Weights');
  "IW{1,1}(940,:)'" : Constant  Value=[-7.3050357007082329374725304660387337207794189453125;-8.669837521361490217941536684520542621612548828125;-8.2142810390229410444362656562589108943939208984375]
      mask Display: e = 0.06;c1 = [120 150 230]/255;c2 = ([120 150 230]+0)/383;c3 = ([120 150 230]+128)/383;patch([0 1 1 0],[0 0 1 1],c1);patch([0 1 1 1-e 1-e 0+e],[0 0 1 1-e 0+e 0+e],c2);patch([0 0 1 1-e 0+e 0+e],[0 1 1 1-e 1-e 0+e],c3);plot([0 1 1 0 0],[0 0 1 1 0]);disp('Weights');
  "IW{1,1}(941,:)'" : Constant  Value=[0.564881880843600914232638388057239353656768798828125;13.6131061980209739914471356314606964588165283203125;-3.22038092123971164681961454334668815135955810546875]
      mask Display: e = 0.06;c1 = [120 150 230]/255;c2 = ([120 150 230]+0)/383;c3 = ([120 150 230]+128)/383;patch([0 1 1 0],[0 0 1 1],c1);patch([0 1 1 1-e 1-e 0+e],[0 0 1 1-e 0+e 0+e],c2);patch([0 0 1 1-e 0+e 0+e],[0 1 1 1-e 1-e 0+e],c3);plot([0 1 1 0 0],[0 0 1 1 0]);disp('Weights');
  "IW{1,1}(942,:)'" : Constant  Value=[13.193773490384383961782077676616609096527099609375;-0.48129504747560358790536838569096289575099945068359375;-4.5173118423758413797486355178989470005035400390625]
      mask Display: e = 0.06;c1 = [120 150 230]/255;c2 = ([120 150 230]+0)/383;c3 = ([120 150 230]+128)/383;patch([0 1 1 0],[0 0 1 1],c1);patch([0 1 1 1-e 1-e 0+e],[0 0 1 1-e 0+e 0+e],c2);patch([0 0 1 1-e 0+e 0+e],[0 1 1 1-e 1-e 0+e],c3);plot([0 1 1 0 0],[0 0 1 1 0]);disp('Weights');
  "IW{1,1}(943,:)'" : Constant  Value=[-6.02649623048657989698995152139104902744293212890625;-10.492334964578443390337270102463662624359130859375;7.02482305802035256192539236508309841156005859375]
      mask Display: e = 0.06;c1 = [120 150 230]/255;c2 = ([120 150 230]+0)/383;c3 = ([120 150 230]+128)/383;patch([0 1 1 0],[0 0 1 1],c1);patch([0 1 1 1-e 1-e 0+e],[0 0 1 1-e 0+e 0+e],c2);patch([0 0 1 1-e 0+e 0+e],[0 1 1 1-e 1-e 0+e],c3);plot([0 1 1 0 0],[0 0 1 1 0]);disp('Weights');
  "IW{1,1}(944,:)'" : Constant  Value=[-9.624994717840838376332612824626266956329345703125;-5.52106344860899067583659416413865983486175537109375;-8.5418010255466665370249756961129605770111083984375]
      mask Display: e = 0.06;c1 = [120 150 230]/255;c2 = ([120 150 230]+0)/383;c3 = ([120 150 230]+128)/383;patch([0 1 1 0],[0 0 1 1],c1);patch([0 1 1 1-e 1-e 0+e],[0 0 1 1-e 0+e 0+e],c2);patch([0 0 1 1-e 0+e 0+e],[0 1 1 1-e 1-e 0+e],c3);plot([0 1 1 0 0],[0 0 1 1 0]);disp('Weights');
  "IW{1,1}(945,:)'" : Constant  Value=[-8.46351659960472346710957936011254787445068359375;-10.24129231161145270334600354544818401336669921875;4.42061236514401745267832666286267340183258056640625]
      mask Display: e = 0.06;c1 = [120 150 230]/255;c2 = ([120 150 230]+0)/383;c3 = ([120 150 230]+128)/383;patch([0 1 1 0],[0 0 1 1],c1);patch([0 1 1 1-e 1-e 0+e],[0 0 1 1-e 0+e 0+e],c2);patch([0 0 1 1-e 0+e 0+e],[0 1 1 1-e 1-e 0+e],c3);plot([0 1 1 0 0],[0 0 1 1 0]);disp('Weights');
  "IW{1,1}(946,:)'" : Constant  Value=[-9.7125431665115780077712770435027778148651123046875;8.9229474247134472619791267788968980312347412109375;-4.686541158912238103084746398963034152984619140625]
      mask Display: e = 0.06;c1 = [120 150 230]/255;c2 = ([120 150 230]+0)/383;c3 = ([120 150 230]+128)/383;patch([0 1 1 0],[0 0 1 1],c1);patch([0 1 1 1-e 1-e 0+e],[0 0 1 1-e 0+e 0+e],c2);patch([0 0 1 1-e 0+e 0+e],[0 1 1 1-e 1-e 0+e],c3);plot([0 1 1 0 0],[0 0 1 1 0]);disp('Weights');
  "IW{1,1}(947,:)'" : Constant  Value=[-2.220228550627661778804622372263111174106597900390625;-9.5068491357218878334833789267577230930328369140625;-10.087857712076992555694232578389346599578857421875]
      mask Display: e = 0.06;c1 = [120 150 230]/255;c2 = ([120 150 230]+0)/383;c3 = ([120 150 230]+128)/383;patch([0 1 1 0],[0 0 1 1],c1);patch([0 1 1 1-e 1-e 0+e],[0 0 1 1-e 0+e 0+e],c2);patch([0 0 1 1-e 0+e 0+e],[0 1 1 1-e 1-e 0+e],c3);plot([0 1 1 0 0],[0 0 1 1 0]);disp('Weights');
  "IW{1,1}(948,:)'" : Constant  Value=[3.162102476540123330295273262890987098217010498046875;13.4773975966344181642853072844445705413818359375;2.089504771641769398371479837805964052677154541015625]
      mask Display: e = 0.06;c1 = [120 150 230]/255;c2 = ([120 150 230]+0)/383;c3 = ([120 150 230]+128)/383;patch([0 1 1 0],[0 0 1 1],c1);patch([0 1 1 1-e 1-e 0+e],[0 0 1 1-e 0+e 0+e],c2);patch([0 0 1 1-e 0+e 0+e],[0 1 1 1-e 1-e 0+e],c3);plot([0 1 1 0 0],[0 0 1 1 0]);disp('Weights');
  "IW{1,1}(949,:)'" : Constant  Value=[2.573684164112929551038178033195436000823974609375;8.4026412825643461701474734582006931304931640625;10.910772071987754117117219720967113971710205078125]
      mask Display: e = 0.06;c1 = [120 150 230]/255;c2 = ([120 150 230]+0)/383;c3 = ([120 150 230]+128)/383;patch([0 1 1 0],[0 0 1 1],c1);patch([0 1 1 1-e 1-e 0+e],[0 0 1 1-e 0+e 0+e],c2);patch([0 0 1 1-e 0+e 0+e],[0 1 1 1-e 1-e 0+e],c3);plot([0 1 1 0 0],[0 0 1 1 0]);disp('Weights');
  "IW{1,1}(95,:)'" : Constant  Value=[-10.2503068154948291379469083040021359920501708984375;7.6384682744860636915973373106680810451507568359375;-5.70018506474521213789330431609414517879486083984375]
      mask Display: e = 0.06;c1 = [120 150 230]/255;c2 = ([120 150 230]+0)/383;c3 = ([120 150 230]+128)/383;patch([0 1 1 0],[0 0 1 1],c1);patch([0 1 1 1-e 1-e 0+e],[0 0 1 1-e 0+e 0+e],c2);patch([0 0 1 1-e 0+e 0+e],[0 1 1 1-e 1-e 0+e],c3);plot([0 1 1 0 0],[0 0 1 1 0]);disp('Weights');
  "IW{1,1}(950,:)'" : Constant  Value=[2.092468103760958708647876846953295171260833740234375;-0.472062413630418842291902592478436417877674102783203125;13.8229389195747405238989813369698822498321533203125]
      mask Display: e = 0.06;c1 = [120 150 230]/255;c2 = ([120 150 230]+0)/383;c3 = ([120 150 230]+128)/383;patch([0 1 1 0],[0 0 1 1],c1);patch([0 1 1 1-e 1-e 0+e],[0 0 1 1-e 0+e 0+e],c2);patch([0 0 1 1-e 0+e 0+e],[0 1 1 1-e 1-e 0+e],c3);plot([0 1 1 0 0],[0 0 1 1 0]);disp('Weights');
  "IW{1,1}(951,:)'" : Constant  Value=[-12.9669590134701433470354459132067859172821044921875;4.273578065338927700622662086971104145050048828125;-3.149778442887320561993647061171941459178924560546875]
      mask Display: e = 0.06;c1 = [120 150 230]/255;c2 = ([120 150 230]+0)/383;c3 = ([120 150 230]+128)/383;patch([0 1 1 0],[0 0 1 1],c1);patch([0 1 1 1-e 1-e 0+e],[0 0 1 1-e 0+e 0+e],c2);patch([0 0 1 1-e 0+e 0+e],[0 1 1 1-e 1-e 0+e],c3);plot([0 1 1 0 0],[0 0 1 1 0]);disp('Weights');
  "IW{1,1}(952,:)'" : Constant  Value=[-10.254106459530181183481545303948223590850830078125;-9.24230602324272609848776482976973056793212890625;-2.188069176916740854466070231865160167217254638671875]
      mask Display: e = 0.06;c1 = [120 150 230]/255;c2 = ([120 150 230]+0)/383;c3 = ([120 150 230]+128)/383;patch([0 1 1 0],[0 0 1 1],c1);patch([0 1 1 1-e 1-e 0+e],[0 0 1 1-e 0+e 0+e],c2);patch([0 0 1 1-e 0+e 0+e],[0 1 1 1-e 1-e 0+e],c3);plot([0 1 1 0 0],[0 0 1 1 0]);disp('Weights');
  "IW{1,1}(953,:)'" : Constant  Value=[10.35171579011882414533829432912170886993408203125;-3.22306527132439324390134061104618012905120849609375;-8.857415587568976178545199218206107616424560546875]
      mask Display: e = 0.06;c1 = [120 150 230]/255;c2 = ([120 150 230]+0)/383;c3 = ([120 150 230]+128)/383;patch([0 1 1 0],[0 0 1 1],c1);patch([0 1 1 1-e 1-e 0+e],[0 0 1 1-e 0+e 0+e],c2);patch([0 0 1 1-e 0+e 0+e],[0 1 1 1-e 1-e 0+e],c3);plot([0 1 1 0 0],[0 0 1 1 0]);disp('Weights');
  "IW{1,1}(954,:)'" : Constant  Value=[2.213432017844668475703429066925309598445892333984375;8.0742309387535815545788864255882799625396728515625;11.1908144528279382967639321577735245227813720703125]
      mask Display: e = 0.06;c1 = [120 150 230]/255;c2 = ([120 150 230]+0)/383;c3 = ([120 150 230]+128)/383;patch([0 1 1 0],[0 0 1 1],c1);patch([0 1 1 1-e 1-e 0+e],[0 0 1 1-e 0+e 0+e],c2);patch([0 0 1 1-e 0+e 0+e],[0 1 1 1-e 1-e 0+e],c3);plot([0 1 1 0 0],[0 0 1 1 0]);disp('Weights');
  "IW{1,1}(955,:)'" : Constant  Value=[-8.3521142123529017453620326705276966094970703125;-4.2918624852432589733552958932705223560333251953125;-10.417944601136067461766288033686578273773193359375]
      mask Display: e = 0.06;c1 = [120 150 230]/255;c2 = ([120 150 230]+0)/383;c3 = ([120 150 230]+128)/383;patch([0 1 1 0],[0 0 1 1],c1);patch([0 1 1 1-e 1-e 0+e],[0 0 1 1-e 0+e 0+e],c2);patch([0 0 1 1-e 0+e 0+e],[0 1 1 1-e 1-e 0+e],c3);plot([0 1 1 0 0],[0 0 1 1 0]);disp('Weights');
  "IW{1,1}(956,:)'" : Constant  Value=[-6.32468894519089186445626182830892503261566162109375;9.320159674629739043894005590118467807769775390625;-8.3017449023471971969456717488355934619903564453125]
      mask Display: e = 0.06;c1 = [120 150 230]/255;c2 = ([120 150 230]+0)/383;c3 = ([120 150 230]+128)/383;patch([0 1 1 0],[0 0 1 1],c1);patch([0 1 1 1-e 1-e 0+e],[0 0 1 1-e 0+e 0+e],c2);patch([0 0 1 1-e 0+e 0+e],[0 1 1 1-e 1-e 0+e],c3);plot([0 1 1 0 0],[0 0 1 1 0]);disp('Weights');
  "IW{1,1}(957,:)'" : Constant  Value=[2.14086711231366155772093406994827091693878173828125;-13.773480047003136661487587844021618366241455078125;1.4110522375625877966598409329890273511409759521484375]
      mask Display: e = 0.06;c1 = [120 150 230]/255;c2 = ([120 150 230]+0)/383;c3 = ([120 150 230]+128)/383;patch([0 1 1 0],[0 0 1 1],c1);patch([0 1 1 1-e 1-e 0+e],[0 0 1 1-e 0+e 0+e],c2);patch([0 0 1 1-e 0+e 0+e],[0 1 1 1-e 1-e 0+e],c3);plot([0 1 1 0 0],[0 0 1 1 0]);disp('Weights');
  "IW{1,1}(958,:)'" : Constant  Value=[-7.2605625027462270537625954602845013141632080078125;11.7945070341616204956380897783674299716949462890625;2.042936511855849790464390025590546429157257080078125]
      mask Display: e = 0.06;c1 = [120 150 230]/255;c2 = ([120 150 230]+0)/383;c3 = ([120 150 230]+128)/383;patch([0 1 1 0],[0 0 1 1],c1);patch([0 1 1 1-e 1-e 0+e],[0 0 1 1-e 0+e 0+e],c2);patch([0 0 1 1-e 0+e 0+e],[0 1 1 1-e 1-e 0+e],c3);plot([0 1 1 0 0],[0 0 1 1 0]);disp('Weights');
  "IW{1,1}(959,:)'" : Constant  Value=[1.561190850570778554384787639719434082508087158203125;1.336005458454973204851512491586618125438690185546875;13.8561456670244655953183610108681023120880126953125]
      mask Display: e = 0.06;c1 = [120 150 230]/255;c2 = ([120 150 230]+0)/383;c3 = ([120 150 230]+128)/383;patch([0 1 1 0],[0 0 1 1],c1);patch([0 1 1 1-e 1-e 0+e],[0 0 1 1-e 0+e 0+e],c2);patch([0 0 1 1-e 0+e 0+e],[0 1 1 1-e 1-e 0+e],c3);plot([0 1 1 0 0],[0 0 1 1 0]);disp('Weights');
  "IW{1,1}(96,:)'" : Constant  Value=[7.99021824572595473767933071940205991268157958984375;7.89160831678095053831611949135549366474151611328125;8.3593624059695770256439573131501674652099609375]
      mask Display: e = 0.06;c1 = [120 150 230]/255;c2 = ([120 150 230]+0)/383;c3 = ([120 150 230]+128)/383;patch([0 1 1 0],[0 0 1 1],c1);patch([0 1 1 1-e 1-e 0+e],[0 0 1 1-e 0+e 0+e],c2);patch([0 0 1 1-e 0+e 0+e],[0 1 1 1-e 1-e 0+e],c3);plot([0 1 1 0 0],[0 0 1 1 0]);disp('Weights');
  "IW{1,1}(960,:)'" : Constant  Value=[-4.279271439381613362229472841136157512664794921875;8.6514891738825934197620881604962050914764404296875;-10.08670334232078147351785446517169475555419921875]
      mask Display: e = 0.06;c1 = [120 150 230]/255;c2 = ([120 150 230]+0)/383;c3 = ([120 150 230]+128)/383;patch([0 1 1 0],[0 0 1 1],c1);patch([0 1 1 1-e 1-e 0+e],[0 0 1 1-e 0+e 0+e],c2);patch([0 0 1 1-e 0+e 0+e],[0 1 1 1-e 1-e 0+e],c3);plot([0 1 1 0 0],[0 0 1 1 0]);disp('Weights');
  "IW{1,1}(961,:)'" : Constant  Value=[-5.7233798808120894818785018287599086761474609375;-11.49486381068663121141071314923465251922607421875;5.6014116952276964411794324405491352081298828125]
      mask Display: e = 0.06;c1 = [120 150 230]/255;c2 = ([120 150 230]+0)/383;c3 = ([120 150 230]+128)/383;patch([0 1 1 0],[0 0 1 1],c1);patch([0 1 1 1-e 1-e 0+e],[0 0 1 1-e 0+e 0+e],c2);patch([0 0 1 1-e 0+e 0+e],[0 1 1 1-e 1-e 0+e],c3);plot([0 1 1 0 0],[0 0 1 1 0]);disp('Weights');
  "IW{1,1}(962,:)'" : Constant  Value=[-4.2223334006116743921666056849062442779541015625;-13.273286421278580604621311067603528499603271484375;1.441260108894922620237366572837345302104949951171875]
      mask Display: e = 0.06;c1 = [120 150 230]/255;c2 = ([120 150 230]+0)/383;c3 = ([120 150 230]+128)/383;patch([0 1 1 0],[0 0 1 1],c1);patch([0 1 1 1-e 1-e 0+e],[0 0 1 1-e 0+e 0+e],c2);patch([0 0 1 1-e 0+e 0+e],[0 1 1 1-e 1-e 0+e],c3);plot([0 1 1 0 0],[0 0 1 1 0]);disp('Weights');
  "IW{1,1}(963,:)'" : Constant  Value=[-7.19238093744871687107433899655006825923919677734375;10.0202167954885990042157573043368756771087646484375;6.62238486617158006453109919675625860691070556640625]
      mask Display: e = 0.06;c1 = [120 150 230]/255;c2 = ([120 150 230]+0)/383;c3 = ([120 150 230]+128)/383;patch([0 1 1 0],[0 0 1 1],c1);patch([0 1 1 1-e 1-e 0+e],[0 0 1 1-e 0+e 0+e],c2);patch([0 0 1 1-e 0+e 0+e],[0 1 1 1-e 1-e 0+e],c3);plot([0 1 1 0 0],[0 0 1 1 0]);disp('Weights');
  "IW{1,1}(964,:)'" : Constant  Value=[8.7600864159361861993602360598742961883544921875;4.8429679038274731084356972132809460163116455078125;9.75895419743645931021092110313475131988525390625]
      mask Display: e = 0.06;c1 = [120 150 230]/255;c2 = ([120 150 230]+0)/383;c3 = ([120 150 230]+128)/383;patch([0 1 1 0],[0 0 1 1],c1);patch([0 1 1 1-e 1-e 0+e],[0 0 1 1-e 0+e 0+e],c2);patch([0 0 1 1-e 0+e 0+e],[0 1 1 1-e 1-e 0+e],c3);plot([0 1 1 0 0],[0 0 1 1 0]);disp('Weights');
  "IW{1,1}(965,:)'" : Constant  Value=[7.7747860665158423643106289091520011425018310546875;-0.2452317718864230611242049917564145289361476898193359375;11.6366131424439007702176240854896605014801025390625]
      mask Display: e = 0.06;c1 = [120 150 230]/255;c2 = ([120 150 230]+0)/383;c3 = ([120 150 230]+128)/383;patch([0 1 1 0],[0 0 1 1],c1);patch([0 1 1 1-e 1-e 0+e],[0 0 1 1-e 0+e 0+e],c2);patch([0 0 1 1-e 0+e 0+e],[0 1 1 1-e 1-e 0+e],c3);plot([0 1 1 0 0],[0 0 1 1 0]);disp('Weights');
  "IW{1,1}(966,:)'" : Constant  Value=[9.415611847847532800415137899108231067657470703125;-2.759727184140187805638788631767965853214263916015625;-9.98649933621960173013576422818005084991455078125]
      mask Display: e = 0.06;c1 = [120 150 230]/255;c2 = ([120 150 230]+0)/383;c3 = ([120 150 230]+128)/383;patch([0 1 1 0],[0 0 1 1],c1);patch([0 1 1 1-e 1-e 0+e],[0 0 1 1-e 0+e 0+e],c2);patch([0 0 1 1-e 0+e 0+e],[0 1 1 1-e 1-e 0+e],c3);plot([0 1 1 0 0],[0 0 1 1 0]);disp('Weights');
  "IW{1,1}(967,:)'" : Constant  Value=[-1.4766613606056127050436543868272565305233001708984375;8.63523894075978404316629166714847087860107421875;-10.9311461277167563110879200394265353679656982421875]
      mask Display: e = 0.06;c1 = [120 150 230]/255;c2 = ([120 150 230]+0)/383;c3 = ([120 150 230]+128)/383;patch([0 1 1 0],[0 0 1 1],c1);patch([0 1 1 1-e 1-e 0+e],[0 0 1 1-e 0+e 0+e],c2);patch([0 0 1 1-e 0+e 0+e],[0 1 1 1-e 1-e 0+e],c3);plot([0 1 1 0 0],[0 0 1 1 0]);disp('Weights');
  "IW{1,1}(968,:)'" : Constant  Value=[-3.227736530736148079512304320815019309520721435546875;-6.347750161633900489732695859856903553009033203125;11.9808313789040301600152815808542072772979736328125]
      mask Display: e = 0.06;c1 = [120 150 230]/255;c2 = ([120 150 230]+0)/383;c3 = ([120 150 230]+128)/383;patch([0 1 1 0],[0 0 1 1],c1);patch([0 1 1 1-e 1-e 0+e],[0 0 1 1-e 0+e 0+e],c2);patch([0 0 1 1-e 0+e 0+e],[0 1 1 1-e 1-e 0+e],c3);plot([0 1 1 0 0],[0 0 1 1 0]);disp('Weights');
  "IW{1,1}(969,:)'" : Constant  Value=[5.0231887346260606364012346602976322174072265625;7.94589771545648826389651731005869805812835693359375;10.330561395517303679980614106170833110809326171875]
      mask Display: e = 0.06;c1 = [120 150 230]/255;c2 = ([120 150 230]+0)/383;c3 = ([120 150 230]+128)/383;patch([0 1 1 0],[0 0 1 1],c1);patch([0 1 1 1-e 1-e 0+e],[0 0 1 1-e 0+e 0+e],c2);patch([0 0 1 1-e 0+e 0+e],[0 1 1 1-e 1-e 0+e],c3);plot([0 1 1 0 0],[0 0 1 1 0]);disp('Weights');
  "IW{1,1}(97,:)'" : Constant  Value=[-8.9188976210585249049245248897932469844818115234375;-0.052737104276164160909790012965459027327597141265869140625;10.79026596502352930428969557397067546844482421875]
      mask Display: e = 0.06;c1 = [120 150 230]/255;c2 = ([120 150 230]+0)/383;c3 = ([120 150 230]+128)/383;patch([0 1 1 0],[0 0 1 1],c1);patch([0 1 1 1-e 1-e 0+e],[0 0 1 1-e 0+e 0+e],c2);patch([0 0 1 1-e 0+e 0+e],[0 1 1 1-e 1-e 0+e],c3);plot([0 1 1 0 0],[0 0 1 1 0]);disp('Weights');
  "IW{1,1}(970,:)'" : Constant  Value=[10.7486461624296811834256004658527672290802001953125;1.13772433057638533426825233618728816509246826171875;-8.9024480383470407929280554526485502719879150390625]
      mask Display: e = 0.06;c1 = [120 150 230]/255;c2 = ([120 150 230]+0)/383;c3 = ([120 150 230]+128)/383;patch([0 1 1 0],[0 0 1 1],c1);patch([0 1 1 1-e 1-e 0+e],[0 0 1 1-e 0+e 0+e],c2);patch([0 0 1 1-e 0+e 0+e],[0 1 1 1-e 1-e 0+e],c3);plot([0 1 1 0 0],[0 0 1 1 0]);disp('Weights');
  "IW{1,1}(971,:)'" : Constant  Value=[5.74839425562245676104566882713697850704193115234375;10.9207276192839852768656783155165612697601318359375;-6.61116944334044109865544669446535408496856689453125]
      mask Display: e = 0.06;c1 = [120 150 230]/255;c2 = ([120 150 230]+0)/383;c3 = ([120 150 230]+128)/383;patch([0 1 1 0],[0 0 1 1],c1);patch([0 1 1 1-e 1-e 0+e],[0 0 1 1-e 0+e 0+e],c2);patch([0 0 1 1-e 0+e 0+e],[0 1 1 1-e 1-e 0+e],c3);plot([0 1 1 0 0],[0 0 1 1 0]);disp('Weights');
  "IW{1,1}(972,:)'" : Constant  Value=[-7.24194694230854718597356622922234237194061279296875;4.57309198840666564223056411719880998134613037109375;-11.073121721164792319314074120484292507171630859375]
      mask Display: e = 0.06;c1 = [120 150 230]/255;c2 = ([120 150 230]+0)/383;c3 = ([120 150 230]+128)/383;patch([0 1 1 0],[0 0 1 1],c1);patch([0 1 1 1-e 1-e 0+e],[0 0 1 1-e 0+e 0+e],c2);patch([0 0 1 1-e 0+e 0+e],[0 1 1 1-e 1-e 0+e],c3);plot([0 1 1 0 0],[0 0 1 1 0]);disp('Weights');
  "IW{1,1}(973,:)'" : Constant  Value=[-1.7626328479272894700358165209763683378696441650390625;3.884732523540374682369247238966636359691619873046875;13.3177712775107384146622280240990221500396728515625]
      mask Display: e = 0.06;c1 = [120 150 230]/255;c2 = ([120 150 230]+0)/383;c3 = ([120 150 230]+128)/383;patch([0 1 1 0],[0 0 1 1],c1);patch([0 1 1 1-e 1-e 0+e],[0 0 1 1-e 0+e 0+e],c2);patch([0 0 1 1-e 0+e 0+e],[0 1 1 1-e 1-e 0+e],c3);plot([0 1 1 0 0],[0 0 1 1 0]);disp('Weights');
  "IW{1,1}(974,:)'" : Constant  Value=[4.31850836584723030142640709527768194675445556640625;-7.00471432249493464183842661441303789615631103515625;11.34444030034430994646754697896540164947509765625]
      mask Display: e = 0.06;c1 = [120 150 230]/255;c2 = ([120 150 230]+0)/383;c3 = ([120 150 230]+128)/383;patch([0 1 1 0],[0 0 1 1],c1);patch([0 1 1 1-e 1-e 0+e],[0 0 1 1-e 0+e 0+e],c2);patch([0 0 1 1-e 0+e 0+e],[0 1 1 1-e 1-e 0+e],c3);plot([0 1 1 0 0],[0 0 1 1 0]);disp('Weights');
  "IW{1,1}(975,:)'" : Constant  Value=[-9.087636226079897738827639841474592685699462890625;-8.5690901429797268207266824902035295963287353515625;6.32353700862198753185339228366501629352569580078125]
      mask Display: e = 0.06;c1 = [120 150 230]/255;c2 = ([120 150 230]+0)/383;c3 = ([120 150 230]+128)/383;patch([0 1 1 0],[0 0 1 1],c1);patch([0 1 1 1-e 1-e 0+e],[0 0 1 1-e 0+e 0+e],c2);patch([0 0 1 1-e 0+e 0+e],[0 1 1 1-e 1-e 0+e],c3);plot([0 1 1 0 0],[0 0 1 1 0]);disp('Weights');
  "IW{1,1}(976,:)'" : Constant  Value=[3.178228301883162743024513474665582180023193359375;5.59864826256277847704723171773366630077362060546875;-12.476391166542189381516436696983873844146728515625]
      mask Display: e = 0.06;c1 = [120 150 230]/255;c2 = ([120 150 230]+0)/383;c3 = ([120 150 230]+128)/383;patch([0 1 1 0],[0 0 1 1],c1);patch([0 1 1 1-e 1-e 0+e],[0 0 1 1-e 0+e 0+e],c2);patch([0 0 1 1-e 0+e 0+e],[0 1 1 1-e 1-e 0+e],c3);plot([0 1 1 0 0],[0 0 1 1 0]);disp('Weights');
  "IW{1,1}(977,:)'" : Constant  Value=[4.3720640471681218031108073773793876171112060546875;-7.16073023239321759803033273783512413501739501953125;-11.1978542599597172824132940149866044521331787109375]
      mask Display: e = 0.06;c1 = [120 150 230]/255;c2 = ([120 150 230]+0)/383;c3 = ([120 150 230]+128)/383;patch([0 1 1 0],[0 0 1 1],c1);patch([0 1 1 1-e 1-e 0+e],[0 0 1 1-e 0+e 0+e],c2);patch([0 0 1 1-e 0+e 0+e],[0 1 1 1-e 1-e 0+e],c3);plot([0 1 1 0 0],[0 0 1 1 0]);disp('Weights');
  "IW{1,1}(978,:)'" : Constant  Value=[-4.028201287575658540163203724659979343414306640625;13.3833132808669201807560966699384152889251708984375;-0.702762634883340009395169545314274728298187255859375]
      mask Display: e = 0.06;c1 = [120 150 230]/255;c2 = ([120 150 230]+0)/383;c3 = ([120 150 230]+128)/383;patch([0 1 1 0],[0 0 1 1],c1);patch([0 1 1 1-e 1-e 0+e],[0 0 1 1-e 0+e 0+e],c2);patch([0 0 1 1-e 0+e 0+e],[0 1 1 1-e 1-e 0+e],c3);plot([0 1 1 0 0],[0 0 1 1 0]);disp('Weights');
  "IW{1,1}(979,:)'" : Constant  Value=[1.09028105196910995999814986134879291057586669921875;-2.592834729772541368930660610203631222248077392578125;-13.582312744445335539467123453505337238311767578125]
      mask Display: e = 0.06;c1 = [120 150 230]/255;c2 = ([120 150 230]+0)/383;c3 = ([120 150 230]+128)/383;patch([0 1 1 0],[0 0 1 1],c1);patch([0 1 1 1-e 1-e 0+e],[0 0 1 1-e 0+e 0+e],c2);patch([0 0 1 1-e 0+e 0+e],[0 1 1 1-e 1-e 0+e],c3);plot([0 1 1 0 0],[0 0 1 1 0]);disp('Weights');
  "IW{1,1}(98,:)'" : Constant  Value=[-9.2523008891750908588846868951804935932159423828125;-6.17056965937887635931247132248245179653167724609375;-8.504157785230301414003406534902751445770263671875]
      mask Display: e = 0.06;c1 = [120 150 230]/255;c2 = ([120 150 230]+0)/383;c3 = ([120 150 230]+128)/383;patch([0 1 1 0],[0 0 1 1],c1);patch([0 1 1 1-e 1-e 0+e],[0 0 1 1-e 0+e 0+e],c2);patch([0 0 1 1-e 0+e 0+e],[0 1 1 1-e 1-e 0+e],c3);plot([0 1 1 0 0],[0 0 1 1 0]);disp('Weights');
  "IW{1,1}(980,:)'" : Constant  Value=[-9.190033205783837644275990896858274936676025390625;-6.8201748933675236941098773968406021595001220703125;8.0603740911418118031406265799887478351593017578125]
      mask Display: e = 0.06;c1 = [120 150 230]/255;c2 = ([120 150 230]+0)/383;c3 = ([120 150 230]+128)/383;patch([0 1 1 0],[0 0 1 1],c1);patch([0 1 1 1-e 1-e 0+e],[0 0 1 1-e 0+e 0+e],c2);patch([0 0 1 1-e 0+e 0+e],[0 1 1 1-e 1-e 0+e],c3);plot([0 1 1 0 0],[0 0 1 1 0]);disp('Weights');
  "IW{1,1}(981,:)'" : Constant  Value=[-12.3267619995172008628969706478528678417205810546875;4.66074037646290406655680271796882152557373046875;4.7252965901331602793788988492451608180999755859375]
      mask Display: e = 0.06;c1 = [120 150 230]/255;c2 = ([120 150 230]+0)/383;c3 = ([120 150 230]+128)/383;patch([0 1 1 0],[0 0 1 1],c1);patch([0 1 1 1-e 1-e 0+e],[0 0 1 1-e 0+e 0+e],c2);patch([0 0 1 1-e 0+e 0+e],[0 1 1 1-e 1-e 0+e],c3);plot([0 1 1 0 0],[0 0 1 1 0]);disp('Weights');
  "IW{1,1}(982,:)'" : Constant  Value=[-11.63839528962915181864445912651717662811279296875;-6.88843884937994754835699495743028819561004638671875;3.637886772037103977339711491367779672145843505859375]
      mask Display: e = 0.06;c1 = [120 150 230]/255;c2 = ([120 150 230]+0)/383;c3 = ([120 150 230]+128)/383;patch([0 1 1 0],[0 0 1 1],c1);patch([0 1 1 1-e 1-e 0+e],[0 0 1 1-e 0+e 0+e],c2);patch([0 0 1 1-e 0+e 0+e],[0 1 1 1-e 1-e 0+e],c3);plot([0 1 1 0 0],[0 0 1 1 0]);disp('Weights');
  "IW{1,1}(983,:)'" : Constant  Value=[-2.743220221673001280038306504138745367527008056640625;-13.6147606017818052492884817183949053287506103515625;-1.7636219792848619736247428591013886034488677978515625]
      mask Display: e = 0.06;c1 = [120 150 230]/255;c2 = ([120 150 230]+0)/383;c3 = ([120 150 230]+128)/383;patch([0 1 1 0],[0 0 1 1],c1);patch([0 1 1 1-e 1-e 0+e],[0 0 1 1-e 0+e 0+e],c2);patch([0 0 1 1-e 0+e 0+e],[0 1 1 1-e 1-e 0+e],c3);plot([0 1 1 0 0],[0 0 1 1 0]);disp('Weights');
  "IW{1,1}(984,:)'" : Constant  Value=[2.906647163207597639456025717663578689098358154296875;-9.91201491364953568563578301109373569488525390625;9.49340592160475438276989734731614589691162109375]
      mask Display: e = 0.06;c1 = [120 150 230]/255;c2 = ([120 150 230]+0)/383;c3 = ([120 150 230]+128)/383;patch([0 1 1 0],[0 0 1 1],c1);patch([0 1 1 1-e 1-e 0+e],[0 0 1 1-e 0+e 0+e],c2);patch([0 0 1 1-e 0+e 0+e],[0 1 1 1-e 1-e 0+e],c3);plot([0 1 1 0 0],[0 0 1 1 0]);disp('Weights');
  "IW{1,1}(985,:)'" : Constant  Value=[-8.1281047964410380046729187597520649433135986328125;-10.2480401688501725487867588526569306850433349609375;5.11249184006183821082913709688000380992889404296875]
      mask Display: e = 0.06;c1 = [120 150 230]/255;c2 = ([120 150 230]+0)/383;c3 = ([120 150 230]+128)/383;patch([0 1 1 0],[0 0 1 1],c1);patch([0 1 1 1-e 1-e 0+e],[0 0 1 1-e 0+e 0+e],c2);patch([0 0 1 1-e 0+e 0+e],[0 1 1 1-e 1-e 0+e],c3);plot([0 1 1 0 0],[0 0 1 1 0]);disp('Weights');
  "IW{1,1}(986,:)'" : Constant  Value=[-9.076821616073647902567245182581245899200439453125;-5.70930529834906064223787325317971408367156982421875;-8.9640851594675314828464252059347927570343017578125]
      mask Display: e = 0.06;c1 = [120 150 230]/255;c2 = ([120 150 230]+0)/383;c3 = ([120 150 230]+128)/383;patch([0 1 1 0],[0 0 1 1],c1);patch([0 1 1 1-e 1-e 0+e],[0 0 1 1-e 0+e 0+e],c2);patch([0 0 1 1-e 0+e 0+e],[0 1 1 1-e 1-e 0+e],c3);plot([0 1 1 0 0],[0 0 1 1 0]);disp('Weights');
  "IW{1,1}(987,:)'" : Constant  Value=[-1.0874634167096617343162279212265275418758392333984375;-3.099542179516940887396003745379857718944549560546875;-13.5997627628626513995868663187138736248016357421875]
      mask Display: e = 0.06;c1 = [120 150 230]/255;c2 = ([120 150 230]+0)/383;c3 = ([120 150 230]+128)/383;patch([0 1 1 0],[0 0 1 1],c1);patch([0 1 1 1-e 1-e 0+e],[0 0 1 1-e 0+e 0+e],c2);patch([0 0 1 1-e 0+e 0+e],[0 1 1 1-e 1-e 0+e],c3);plot([0 1 1 0 0],[0 0 1 1 0]);disp('Weights');
  "IW{1,1}(988,:)'" : Constant  Value=[-9.3517396176932976459283963777124881744384765625;-4.1655249890570740234352342667989432811737060546875;9.5114650653776049438192785601131618022918701171875]
      mask Display: e = 0.06;c1 = [120 150 230]/255;c2 = ([120 150 230]+0)/383;c3 = ([120 150 230]+128)/383;patch([0 1 1 0],[0 0 1 1],c1);patch([0 1 1 1-e 1-e 0+e],[0 0 1 1-e 0+e 0+e],c2);patch([0 0 1 1-e 0+e 0+e],[0 1 1 1-e 1-e 0+e],c3);plot([0 1 1 0 0],[0 0 1 1 0]);disp('Weights');
  "IW{1,1}(989,:)'" : Constant  Value=[-10.1136727457241288874456586199812591075897216796875;2.84589536496274408960971413762308657169342041015625;-9.2527643191561086410956704639829695224761962890625]
      mask Display: e = 0.06;c1 = [120 150 230]/255;c2 = ([120 150 230]+0)/383;c3 = ([120 150 230]+128)/383;patch([0 1 1 0],[0 0 1 1],c1);patch([0 1 1 1-e 1-e 0+e],[0 0 1 1-e 0+e 0+e],c2);patch([0 0 1 1-e 0+e 0+e],[0 1 1 1-e 1-e 0+e],c3);plot([0 1 1 0 0],[0 0 1 1 0]);disp('Weights');
  "IW{1,1}(99,:)'" : Constant  Value=[5.37902228575958130107892429805360734462738037109375;-5.842285206625557947290872107259929180145263671875;-11.5017842718597460560658873873762786388397216796875]
      mask Display: e = 0.06;c1 = [120 150 230]/255;c2 = ([120 150 230]+0)/383;c3 = ([120 150 230]+128)/383;patch([0 1 1 0],[0 0 1 1],c1);patch([0 1 1 1-e 1-e 0+e],[0 0 1 1-e 0+e 0+e],c2);patch([0 0 1 1-e 0+e 0+e],[0 1 1 1-e 1-e 0+e],c3);plot([0 1 1 0 0],[0 0 1 1 0]);disp('Weights');
  "IW{1,1}(990,:)'" : Constant  Value=[10.4296469460281766572506967349909245967864990234375;5.96447931747435955429637033375911414623260498046875;7.18983781648460595903316061594523489475250244140625]
      mask Display: e = 0.06;c1 = [120 150 230]/255;c2 = ([120 150 230]+0)/383;c3 = ([120 150 230]+128)/383;patch([0 1 1 0],[0 0 1 1],c1);patch([0 1 1 1-e 1-e 0+e],[0 0 1 1-e 0+e 0+e],c2);patch([0 0 1 1-e 0+e 0+e],[0 1 1 1-e 1-e 0+e],c3);plot([0 1 1 0 0],[0 0 1 1 0]);disp('Weights');
  "IW{1,1}(991,:)'" : Constant  Value=[7.01482174876300224042324771289713680744171142578125;-7.7079803678530378618916074628941714763641357421875;9.3472432902113524733067606575787067413330078125]
      mask Display: e = 0.06;c1 = [120 150 230]/255;c2 = ([120 150 230]+0)/383;c3 = ([120 150 230]+128)/383;patch([0 1 1 0],[0 0 1 1],c1);patch([0 1 1 1-e 1-e 0+e],[0 0 1 1-e 0+e 0+e],c2);patch([0 0 1 1-e 0+e 0+e],[0 1 1 1-e 1-e 0+e],c3);plot([0 1 1 0 0],[0 0 1 1 0]);disp('Weights');
  "IW{1,1}(992,:)'" : Constant  Value=[-11.91031636705891827432424179278314113616943359375;6.54732885779984830065814094268716871738433837890625;-3.28521421192799589761079914751462638378143310546875]
      mask Display: e = 0.06;c1 = [120 150 230]/255;c2 = ([120 150 230]+0)/383;c3 = ([120 150 230]+128)/383;patch([0 1 1 0],[0 0 1 1],c1);patch([0 1 1 1-e 1-e 0+e],[0 0 1 1-e 0+e 0+e],c2);patch([0 0 1 1-e 0+e 0+e],[0 1 1 1-e 1-e 0+e],c3);plot([0 1 1 0 0],[0 0 1 1 0]);disp('Weights');
  "IW{1,1}(993,:)'" : Constant  Value=[10.8816642606544125015943791368044912815093994140625;-3.7179839928613791499856233713217079639434814453125;7.99228619232222836643586560967378318309783935546875]
      mask Display: e = 0.06;c1 = [120 150 230]/255;c2 = ([120 150 230]+0)/383;c3 = ([120 150 230]+128)/383;patch([0 1 1 0],[0 0 1 1],c1);patch([0 1 1 1-e 1-e 0+e],[0 0 1 1-e 0+e 0+e],c2);patch([0 0 1 1-e 0+e 0+e],[0 1 1 1-e 1-e 0+e],c3);plot([0 1 1 0 0],[0 0 1 1 0]);disp('Weights');
  "IW{1,1}(994,:)'" : Constant  Value=[-1.7748512096031940910023649848881177604198455810546875;2.873986877751303570249774566036649048328399658203125;13.4608978726893457888991179061122238636016845703125]
      mask Display: e = 0.06;c1 = [120 150 230]/255;c2 = ([120 150 230]+0)/383;c3 = ([120 150 230]+128)/383;patch([0 1 1 0],[0 0 1 1],c1);patch([0 1 1 1-e 1-e 0+e],[0 0 1 1-e 0+e 0+e],c2);patch([0 0 1 1-e 0+e 0+e],[0 1 1 1-e 1-e 0+e],c3);plot([0 1 1 0 0],[0 0 1 1 0]);disp('Weights');
  "IW{1,1}(995,:)'" : Constant  Value=[-4.16383280783248199696799929370172321796417236328125;-10.40804576284276805608897120691835880279541015625;-8.402478424781865129489233368076384067535400390625]
      mask Display: e = 0.06;c1 = [120 150 230]/255;c2 = ([120 150 230]+0)/383;c3 = ([120 150 230]+128)/383;patch([0 1 1 0],[0 0 1 1],c1);patch([0 1 1 1-e 1-e 0+e],[0 0 1 1-e 0+e 0+e],c2);patch([0 0 1 1-e 0+e 0+e],[0 1 1 1-e 1-e 0+e],c3);plot([0 1 1 0 0],[0 0 1 1 0]);disp('Weights');
  "IW{1,1}(996,:)'" : Constant  Value=[-8.519940558079650116951597738079726696014404296875;8.484939349476146475126370205543935298919677734375;-7.16236074544130740804348533856682479381561279296875]
      mask Display: e = 0.06;c1 = [120 150 230]/255;c2 = ([120 150 230]+0)/383;c3 = ([120 150 230]+128)/383;patch([0 1 1 0],[0 0 1 1],c1);patch([0 1 1 1-e 1-e 0+e],[0 0 1 1-e 0+e 0+e],c2);patch([0 0 1 1-e 0+e 0+e],[0 1 1 1-e 1-e 0+e],c3);plot([0 1 1 0 0],[0 0 1 1 0]);disp('Weights');
  "IW{1,1}(997,:)'" : Constant  Value=[-3.388134165333909653128330319304950535297393798828125;-8.4846220126017346530034046736545860767364501953125;10.5667996596707514100899061304517090320587158203125]
      mask Display: e = 0.06;c1 = [120 150 230]/255;c2 = ([120 150 230]+0)/383;c3 = ([120 150 230]+128)/383;patch([0 1 1 0],[0 0 1 1],c1);patch([0 1 1 1-e 1-e 0+e],[0 0 1 1-e 0+e 0+e],c2);patch([0 0 1 1-e 0+e 0+e],[0 1 1 1-e 1-e 0+e],c3);plot([0 1 1 0 0],[0 0 1 1 0]);disp('Weights');
  "IW{1,1}(998,:)'" : Constant  Value=[7.67908293778316330957522950484417378902435302734375;4.48506536376214892669622713583521544933319091796875;10.81111172118220764559737290255725383758544921875]
      mask Display: e = 0.06;c1 = [120 150 230]/255;c2 = ([120 150 230]+0)/383;c3 = ([120 150 230]+128)/383;patch([0 1 1 0],[0 0 1 1],c1);patch([0 1 1 1-e 1-e 0+e],[0 0 1 1-e 0+e 0+e],c2);patch([0 0 1 1-e 0+e 0+e],[0 1 1 1-e 1-e 0+e],c3);plot([0 1 1 0 0],[0 0 1 1 0]);disp('Weights');
  "IW{1,1}(999,:)'" : Constant  Value=[-5.22640283694893081900545439566485583782196044921875;11.411696139749000877827711519785225391387939453125;-6.19908839369966369048370324890129268169403076171875]
      mask Display: e = 0.06;c1 = [120 150 230]/255;c2 = ([120 150 230]+0)/383;c3 = ([120 150 230]+128)/383;patch([0 1 1 0],[0 0 1 1],c1);patch([0 1 1 1-e 1-e 0+e],[0 0 1 1-e 0+e 0+e],c2);patch([0 0 1 1-e 0+e 0+e],[0 1 1 1-e 1-e 0+e],c3);plot([0 1 1 0 0],[0 0 1 1 0]);disp('Weights');
  Mux : Mux  Inputs=1000
      mask Display: e = 0.06;c1 = [120 150 230]/255;c2 = ([120 150 230]+0)/383;c3 = ([120 150 230]+128)/383;patch([0 1 1 0],[0 0 1 1],c1);patch([0 1 1 1-e 1-e 0+e],[0 0 1 1-e 0+e 0+e],c2);patch([0 0 1 1-e 0+e 0+e],[0 1 1 1-e 1-e 0+e],c3);plot([0 1 1 0 0],[0 0 1 1 0]);disp('Mux');
  dotprod{1..1000} (1000 alike) : neural/Weight Functions/dotprod
  "iz{1,1}" : Outport
      mask Display: e = 0.06;c1 = [120 230 180]/255;c2 = ([120 230 180]+0)/(256+128);c3 = ([120 230 180]+128)/(256+128);patch([0 1 1 0],[0 0 1 1],c1);patch([0 1 1 1-e 1-e 0+e],[0 0 1 1-e 0+e 0+e],c2);patch([0 0 1 1-e 0+e 0+e],[0 1 1 1-e 1-e 0+e],c3);plot([0 1 1 0 0],[0 0 1 1 0]);
  wires:
  Mux/1 -> "iz{1,1}"/1
  dotprod1000/1 -> Mux/1000
  "IW{1,1}(1000,:)'"/1 -> dotprod1000/1
  dotprod999/1 -> Mux/999
  "IW{1,1}(999,:)'"/1 -> dotprod999/1
  dotprod998/1 -> Mux/998
  "IW{1,1}(998,:)'"/1 -> dotprod998/1
  dotprod997/1 -> Mux/997
  "IW{1,1}(997,:)'"/1 -> dotprod997/1
  dotprod996/1 -> Mux/996
  "IW{1,1}(996,:)'"/1 -> dotprod996/1
  dotprod995/1 -> Mux/995
  "IW{1,1}(995,:)'"/1 -> dotprod995/1
  dotprod994/1 -> Mux/994
  "IW{1,1}(994,:)'"/1 -> dotprod994/1
  dotprod993/1 -> Mux/993
  "IW{1,1}(993,:)'"/1 -> dotprod993/1
  dotprod992/1 -> Mux/992
  "IW{1,1}(992,:)'"/1 -> dotprod992/1
  dotprod991/1 -> Mux/991
  "IW{1,1}(991,:)'"/1 -> dotprod991/1
  dotprod990/1 -> Mux/990
  "IW{1,1}(990,:)'"/1 -> dotprod990/1
  dotprod989/1 -> Mux/989
  "IW{1,1}(989,:)'"/1 -> dotprod989/1
  dotprod988/1 -> Mux/988
  "IW{1,1}(988,:)'"/1 -> dotprod988/1
  dotprod987/1 -> Mux/987
  "IW{1,1}(987,:)'"/1 -> dotprod987/1
  dotprod986/1 -> Mux/986
  "IW{1,1}(986,:)'"/1 -> dotprod986/1
  dotprod985/1 -> Mux/985
  "IW{1,1}(985,:)'"/1 -> dotprod985/1
  dotprod984/1 -> Mux/984
  "IW{1,1}(984,:)'"/1 -> dotprod984/1
  dotprod983/1 -> Mux/983
  "IW{1,1}(983,:)'"/1 -> dotprod983/1
  dotprod982/1 -> Mux/982
  "IW{1,1}(982,:)'"/1 -> dotprod982/1
  dotprod981/1 -> Mux/981
  "IW{1,1}(981,:)'"/1 -> dotprod981/1
  dotprod980/1 -> Mux/980
  "IW{1,1}(980,:)'"/1 -> dotprod980/1
  dotprod979/1 -> Mux/979
  "IW{1,1}(979,:)'"/1 -> dotprod979/1
  dotprod978/1 -> Mux/978
  "IW{1,1}(978,:)'"/1 -> dotprod978/1
  dotprod977/1 -> Mux/977
  "IW{1,1}(977,:)'"/1 -> dotprod977/1
  dotprod976/1 -> Mux/976
  "IW{1,1}(976,:)'"/1 -> dotprod976/1
  dotprod975/1 -> Mux/975
  "IW{1,1}(975,:)'"/1 -> dotprod975/1
  dotprod974/1 -> Mux/974
  "IW{1,1}(974,:)'"/1 -> dotprod974/1
  dotprod973/1 -> Mux/973
  "IW{1,1}(973,:)'"/1 -> dotprod973/1
  dotprod972/1 -> Mux/972
  "IW{1,1}(972,:)'"/1 -> dotprod972/1
  dotprod971/1 -> Mux/971
  "IW{1,1}(971,:)'"/1 -> dotprod971/1
  dotprod970/1 -> Mux/970
  "IW{1,1}(970,:)'"/1 -> dotprod970/1
  dotprod969/1 -> Mux/969
  "IW{1,1}(969,:)'"/1 -> dotprod969/1
  dotprod968/1 -> Mux/968
  "IW{1,1}(968,:)'"/1 -> dotprod968/1
  dotprod967/1 -> Mux/967
  "IW{1,1}(967,:)'"/1 -> dotprod967/1
  dotprod966/1 -> Mux/966
  "IW{1,1}(966,:)'"/1 -> dotprod966/1
  dotprod965/1 -> Mux/965
  "IW{1,1}(965,:)'"/1 -> dotprod965/1
  dotprod964/1 -> Mux/964
  "IW{1,1}(964,:)'"/1 -> dotprod964/1
  dotprod963/1 -> Mux/963
  "IW{1,1}(963,:)'"/1 -> dotprod963/1
  dotprod962/1 -> Mux/962
  "IW{1,1}(962,:)'"/1 -> dotprod962/1
  dotprod961/1 -> Mux/961
  "IW{1,1}(961,:)'"/1 -> dotprod961/1
  dotprod960/1 -> Mux/960
  "IW{1,1}(960,:)'"/1 -> dotprod960/1
  dotprod959/1 -> Mux/959
  "IW{1,1}(959,:)'"/1 -> dotprod959/1
  dotprod958/1 -> Mux/958
  "IW{1,1}(958,:)'"/1 -> dotprod958/1
  dotprod957/1 -> Mux/957
  "IW{1,1}(957,:)'"/1 -> dotprod957/1
  dotprod956/1 -> Mux/956
  "IW{1,1}(956,:)'"/1 -> dotprod956/1
  dotprod955/1 -> Mux/955
  "IW{1,1}(955,:)'"/1 -> dotprod955/1
  dotprod954/1 -> Mux/954
  "IW{1,1}(954,:)'"/1 -> dotprod954/1
  dotprod953/1 -> Mux/953
  "IW{1,1}(953,:)'"/1 -> dotprod953/1
  dotprod952/1 -> Mux/952
  "IW{1,1}(952,:)'"/1 -> dotprod952/1
  dotprod951/1 -> Mux/951
  "IW{1,1}(951,:)'"/1 -> dotprod951/1
  dotprod950/1 -> Mux/950
  "IW{1,1}(950,:)'"/1 -> dotprod950/1
  dotprod949/1 -> Mux/949
  "IW{1,1}(949,:)'"/1 -> dotprod949/1
  dotprod948/1 -> Mux/948
  "IW{1,1}(948,:)'"/1 -> dotprod948/1
  dotprod947/1 -> Mux/947
  "IW{1,1}(947,:)'"/1 -> dotprod947/1
  dotprod946/1 -> Mux/946
  "IW{1,1}(946,:)'"/1 -> dotprod946/1
  dotprod945/1 -> Mux/945
  "IW{1,1}(945,:)'"/1 -> dotprod945/1
  dotprod944/1 -> Mux/944
  "IW{1,1}(944,:)'"/1 -> dotprod944/1
  dotprod943/1 -> Mux/943
  "IW{1,1}(943,:)'"/1 -> dotprod943/1
  dotprod942/1 -> Mux/942
  "IW{1,1}(942,:)'"/1 -> dotprod942/1
  dotprod941/1 -> Mux/941
  "IW{1,1}(941,:)'"/1 -> dotprod941/1
  dotprod940/1 -> Mux/940
  "IW{1,1}(940,:)'"/1 -> dotprod940/1
  dotprod939/1 -> Mux/939
  "IW{1,1}(939,:)'"/1 -> dotprod939/1
  dotprod938/1 -> Mux/938
  "IW{1,1}(938,:)'"/1 -> dotprod938/1
  dotprod937/1 -> Mux/937
  "IW{1,1}(937,:)'"/1 -> dotprod937/1
  dotprod936/1 -> Mux/936
  "IW{1,1}(936,:)'"/1 -> dotprod936/1
  dotprod935/1 -> Mux/935
  "IW{1,1}(935,:)'"/1 -> dotprod935/1
  dotprod934/1 -> Mux/934
  "IW{1,1}(934,:)'"/1 -> dotprod934/1
  dotprod933/1 -> Mux/933
  "IW{1,1}(933,:)'"/1 -> dotprod933/1
  dotprod932/1 -> Mux/932
  "IW{1,1}(932,:)'"/1 -> dotprod932/1
  dotprod931/1 -> Mux/931
  "IW{1,1}(931,:)'"/1 -> dotprod931/1
  dotprod930/1 -> Mux/930
  "IW{1,1}(930,:)'"/1 -> dotprod930/1
  dotprod929/1 -> Mux/929
  "IW{1,1}(929,:)'"/1 -> dotprod929/1
  dotprod928/1 -> Mux/928
  "IW{1,1}(928,:)'"/1 -> dotprod928/1
  dotprod927/1 -> Mux/927
  "IW{1,1}(927,:)'"/1 -> dotprod927/1
  dotprod926/1 -> Mux/926
  "IW{1,1}(926,:)'"/1 -> dotprod926/1
  dotprod925/1 -> Mux/925
  "IW{1,1}(925,:)'"/1 -> dotprod925/1
  dotprod924/1 -> Mux/924
  "IW{1,1}(924,:)'"/1 -> dotprod924/1
  dotprod923/1 -> Mux/923
  "IW{1,1}(923,:)'"/1 -> dotprod923/1
  dotprod922/1 -> Mux/922
  "IW{1,1}(922,:)'"/1 -> dotprod922/1
  dotprod921/1 -> Mux/921
  "IW{1,1}(921,:)'"/1 -> dotprod921/1
  dotprod920/1 -> Mux/920
  "IW{1,1}(920,:)'"/1 -> dotprod920/1
  dotprod919/1 -> Mux/919
  "IW{1,1}(919,:)'"/1 -> dotprod919/1
  dotprod918/1 -> Mux/918
  "IW{1,1}(918,:)'"/1 -> dotprod918/1
  dotprod917/1 -> Mux/917
  "IW{1,1}(917,:)'"/1 -> dotprod917/1
  dotprod916/1 -> Mux/916
  "IW{1,1}(916,:)'"/1 -> dotprod916/1
  dotprod915/1 -> Mux/915
  "IW{1,1}(915,:)'"/1 -> dotprod915/1
  dotprod914/1 -> Mux/914
  "IW{1,1}(914,:)'"/1 -> dotprod914/1
  dotprod913/1 -> Mux/913
  "IW{1,1}(913,:)'"/1 -> dotprod913/1
  dotprod912/1 -> Mux/912
  "IW{1,1}(912,:)'"/1 -> dotprod912/1
  dotprod911/1 -> Mux/911
  "IW{1,1}(911,:)'"/1 -> dotprod911/1
  dotprod910/1 -> Mux/910
  "IW{1,1}(910,:)'"/1 -> dotprod910/1
  dotprod909/1 -> Mux/909
  "IW{1,1}(909,:)'"/1 -> dotprod909/1
  dotprod908/1 -> Mux/908
  "IW{1,1}(908,:)'"/1 -> dotprod908/1
  dotprod907/1 -> Mux/907
  "IW{1,1}(907,:)'"/1 -> dotprod907/1
  dotprod906/1 -> Mux/906
  "IW{1,1}(906,:)'"/1 -> dotprod906/1
  dotprod905/1 -> Mux/905
  "IW{1,1}(905,:)'"/1 -> dotprod905/1
  dotprod904/1 -> Mux/904
  "IW{1,1}(904,:)'"/1 -> dotprod904/1
  dotprod903/1 -> Mux/903
  "IW{1,1}(903,:)'"/1 -> dotprod903/1
  dotprod902/1 -> Mux/902
  "IW{1,1}(902,:)'"/1 -> dotprod902/1
  dotprod901/1 -> Mux/901
  "IW{1,1}(901,:)'"/1 -> dotprod901/1
  dotprod900/1 -> Mux/900
  "IW{1,1}(900,:)'"/1 -> dotprod900/1
  dotprod899/1 -> Mux/899
  "IW{1,1}(899,:)'"/1 -> dotprod899/1
  dotprod898/1 -> Mux/898
  "IW{1,1}(898,:)'"/1 -> dotprod898/1
  dotprod897/1 -> Mux/897
  "IW{1,1}(897,:)'"/1 -> dotprod897/1
  dotprod896/1 -> Mux/896
  "IW{1,1}(896,:)'"/1 -> dotprod896/1
  dotprod895/1 -> Mux/895
  "IW{1,1}(895,:)'"/1 -> dotprod895/1
  dotprod894/1 -> Mux/894
  "IW{1,1}(894,:)'"/1 -> dotprod894/1
  dotprod893/1 -> Mux/893
  "IW{1,1}(893,:)'"/1 -> dotprod893/1
  dotprod892/1 -> Mux/892
  "IW{1,1}(892,:)'"/1 -> dotprod892/1
  dotprod891/1 -> Mux/891
  "IW{1,1}(891,:)'"/1 -> dotprod891/1
  dotprod890/1 -> Mux/890
  "IW{1,1}(890,:)'"/1 -> dotprod890/1
  dotprod889/1 -> Mux/889
  "IW{1,1}(889,:)'"/1 -> dotprod889/1
  dotprod888/1 -> Mux/888
  "IW{1,1}(888,:)'"/1 -> dotprod888/1
  dotprod887/1 -> Mux/887
  "IW{1,1}(887,:)'"/1 -> dotprod887/1
  dotprod886/1 -> Mux/886
  "IW{1,1}(886,:)'"/1 -> dotprod886/1
  dotprod885/1 -> Mux/885
  "IW{1,1}(885,:)'"/1 -> dotprod885/1
  dotprod884/1 -> Mux/884
  "IW{1,1}(884,:)'"/1 -> dotprod884/1
  dotprod883/1 -> Mux/883
  "IW{1,1}(883,:)'"/1 -> dotprod883/1
  dotprod882/1 -> Mux/882
  "IW{1,1}(882,:)'"/1 -> dotprod882/1
  dotprod881/1 -> Mux/881
  "IW{1,1}(881,:)'"/1 -> dotprod881/1
  dotprod880/1 -> Mux/880
  "IW{1,1}(880,:)'"/1 -> dotprod880/1
  dotprod879/1 -> Mux/879
  "IW{1,1}(879,:)'"/1 -> dotprod879/1
  dotprod878/1 -> Mux/878
  "IW{1,1}(878,:)'"/1 -> dotprod878/1
  dotprod877/1 -> Mux/877
  "IW{1,1}(877,:)'"/1 -> dotprod877/1
  dotprod876/1 -> Mux/876
  "IW{1,1}(876,:)'"/1 -> dotprod876/1
  dotprod875/1 -> Mux/875
  "IW{1,1}(875,:)'"/1 -> dotprod875/1
  dotprod874/1 -> Mux/874
  "IW{1,1}(874,:)'"/1 -> dotprod874/1
  dotprod873/1 -> Mux/873
  "IW{1,1}(873,:)'"/1 -> dotprod873/1
  dotprod872/1 -> Mux/872
  "IW{1,1}(872,:)'"/1 -> dotprod872/1
  dotprod871/1 -> Mux/871
  "IW{1,1}(871,:)'"/1 -> dotprod871/1
  dotprod870/1 -> Mux/870
  "IW{1,1}(870,:)'"/1 -> dotprod870/1
  dotprod869/1 -> Mux/869
  "IW{1,1}(869,:)'"/1 -> dotprod869/1
  dotprod868/1 -> Mux/868
  "IW{1,1}(868,:)'"/1 -> dotprod868/1
  dotprod867/1 -> Mux/867
  "IW{1,1}(867,:)'"/1 -> dotprod867/1
  dotprod866/1 -> Mux/866
  "IW{1,1}(866,:)'"/1 -> dotprod866/1
  dotprod865/1 -> Mux/865
  "IW{1,1}(865,:)'"/1 -> dotprod865/1
  dotprod864/1 -> Mux/864
  "IW{1,1}(864,:)'"/1 -> dotprod864/1
  dotprod863/1 -> Mux/863
  "IW{1,1}(863,:)'"/1 -> dotprod863/1
  dotprod862/1 -> Mux/862
  "IW{1,1}(862,:)'"/1 -> dotprod862/1
  dotprod861/1 -> Mux/861
  "IW{1,1}(861,:)'"/1 -> dotprod861/1
  dotprod860/1 -> Mux/860
  "IW{1,1}(860,:)'"/1 -> dotprod860/1
  dotprod859/1 -> Mux/859
  "IW{1,1}(859,:)'"/1 -> dotprod859/1
  dotprod858/1 -> Mux/858
  "IW{1,1}(858,:)'"/1 -> dotprod858/1
  dotprod857/1 -> Mux/857
  "IW{1,1}(857,:)'"/1 -> dotprod857/1
  dotprod856/1 -> Mux/856
  "IW{1,1}(856,:)'"/1 -> dotprod856/1
  dotprod855/1 -> Mux/855
  "IW{1,1}(855,:)'"/1 -> dotprod855/1
  dotprod854/1 -> Mux/854
  "IW{1,1}(854,:)'"/1 -> dotprod854/1
  dotprod853/1 -> Mux/853
  "IW{1,1}(853,:)'"/1 -> dotprod853/1
  dotprod852/1 -> Mux/852
  "IW{1,1}(852,:)'"/1 -> dotprod852/1
  dotprod851/1 -> Mux/851
  "IW{1,1}(851,:)'"/1 -> dotprod851/1
  dotprod850/1 -> Mux/850
  "IW{1,1}(850,:)'"/1 -> dotprod850/1
  dotprod849/1 -> Mux/849
  "IW{1,1}(849,:)'"/1 -> dotprod849/1
  dotprod848/1 -> Mux/848
  "IW{1,1}(848,:)'"/1 -> dotprod848/1
  dotprod847/1 -> Mux/847
  "IW{1,1}(847,:)'"/1 -> dotprod847/1
  dotprod846/1 -> Mux/846
  "IW{1,1}(846,:)'"/1 -> dotprod846/1
  dotprod845/1 -> Mux/845
  "IW{1,1}(845,:)'"/1 -> dotprod845/1
  dotprod844/1 -> Mux/844
  "IW{1,1}(844,:)'"/1 -> dotprod844/1
  dotprod843/1 -> Mux/843
  "IW{1,1}(843,:)'"/1 -> dotprod843/1
  dotprod842/1 -> Mux/842
  "IW{1,1}(842,:)'"/1 -> dotprod842/1
  dotprod841/1 -> Mux/841
  "IW{1,1}(841,:)'"/1 -> dotprod841/1
  dotprod840/1 -> Mux/840
  "IW{1,1}(840,:)'"/1 -> dotprod840/1
  dotprod839/1 -> Mux/839
  "IW{1,1}(839,:)'"/1 -> dotprod839/1
  dotprod838/1 -> Mux/838
  "IW{1,1}(838,:)'"/1 -> dotprod838/1
  dotprod837/1 -> Mux/837
  "IW{1,1}(837,:)'"/1 -> dotprod837/1
  dotprod836/1 -> Mux/836
  "IW{1,1}(836,:)'"/1 -> dotprod836/1
  dotprod835/1 -> Mux/835
  "IW{1,1}(835,:)'"/1 -> dotprod835/1
  dotprod834/1 -> Mux/834
  "IW{1,1}(834,:)'"/1 -> dotprod834/1
  dotprod833/1 -> Mux/833
  "IW{1,1}(833,:)'"/1 -> dotprod833/1
  dotprod832/1 -> Mux/832
  "IW{1,1}(832,:)'"/1 -> dotprod832/1
  dotprod831/1 -> Mux/831
  "IW{1,1}(831,:)'"/1 -> dotprod831/1
  dotprod830/1 -> Mux/830
  "IW{1,1}(830,:)'"/1 -> dotprod830/1
  dotprod829/1 -> Mux/829
  "IW{1,1}(829,:)'"/1 -> dotprod829/1
  dotprod828/1 -> Mux/828
  "IW{1,1}(828,:)'"/1 -> dotprod828/1
  dotprod827/1 -> Mux/827
  "IW{1,1}(827,:)'"/1 -> dotprod827/1
  dotprod826/1 -> Mux/826
  "IW{1,1}(826,:)'"/1 -> dotprod826/1
  dotprod825/1 -> Mux/825
  "IW{1,1}(825,:)'"/1 -> dotprod825/1
  dotprod824/1 -> Mux/824
  "IW{1,1}(824,:)'"/1 -> dotprod824/1
  dotprod823/1 -> Mux/823
  "IW{1,1}(823,:)'"/1 -> dotprod823/1
  dotprod822/1 -> Mux/822
  "IW{1,1}(822,:)'"/1 -> dotprod822/1
  dotprod821/1 -> Mux/821
  "IW{1,1}(821,:)'"/1 -> dotprod821/1
  dotprod820/1 -> Mux/820
  "IW{1,1}(820,:)'"/1 -> dotprod820/1
  dotprod819/1 -> Mux/819
  "IW{1,1}(819,:)'"/1 -> dotprod819/1
  dotprod818/1 -> Mux/818
  "IW{1,1}(818,:)'"/1 -> dotprod818/1
  dotprod817/1 -> Mux/817
  "IW{1,1}(817,:)'"/1 -> dotprod817/1
  dotprod816/1 -> Mux/816
  "IW{1,1}(816,:)'"/1 -> dotprod816/1
  dotprod815/1 -> Mux/815
  "IW{1,1}(815,:)'"/1 -> dotprod815/1
  dotprod814/1 -> Mux/814
  "IW{1,1}(814,:)'"/1 -> dotprod814/1
  dotprod813/1 -> Mux/813
  "IW{1,1}(813,:)'"/1 -> dotprod813/1
  dotprod812/1 -> Mux/812
  "IW{1,1}(812,:)'"/1 -> dotprod812/1
  dotprod811/1 -> Mux/811
  "IW{1,1}(811,:)'"/1 -> dotprod811/1
  dotprod810/1 -> Mux/810
  "IW{1,1}(810,:)'"/1 -> dotprod810/1
  dotprod809/1 -> Mux/809
  "IW{1,1}(809,:)'"/1 -> dotprod809/1
  dotprod808/1 -> Mux/808
  "IW{1,1}(808,:)'"/1 -> dotprod808/1
  dotprod807/1 -> Mux/807
  "IW{1,1}(807,:)'"/1 -> dotprod807/1
  dotprod806/1 -> Mux/806
  "IW{1,1}(806,:)'"/1 -> dotprod806/1
  dotprod805/1 -> Mux/805
  "IW{1,1}(805,:)'"/1 -> dotprod805/1
  dotprod804/1 -> Mux/804
  "IW{1,1}(804,:)'"/1 -> dotprod804/1
  dotprod803/1 -> Mux/803
  "IW{1,1}(803,:)'"/1 -> dotprod803/1
  dotprod802/1 -> Mux/802
  "IW{1,1}(802,:)'"/1 -> dotprod802/1
  dotprod801/1 -> Mux/801
  "IW{1,1}(801,:)'"/1 -> dotprod801/1
  dotprod800/1 -> Mux/800
  "IW{1,1}(800,:)'"/1 -> dotprod800/1
  dotprod799/1 -> Mux/799
  "IW{1,1}(799,:)'"/1 -> dotprod799/1
  dotprod798/1 -> Mux/798
  "IW{1,1}(798,:)'"/1 -> dotprod798/1
  dotprod797/1 -> Mux/797
  "IW{1,1}(797,:)'"/1 -> dotprod797/1
  dotprod796/1 -> Mux/796
  "IW{1,1}(796,:)'"/1 -> dotprod796/1
  dotprod795/1 -> Mux/795
  "IW{1,1}(795,:)'"/1 -> dotprod795/1
  dotprod794/1 -> Mux/794
  "IW{1,1}(794,:)'"/1 -> dotprod794/1
  dotprod793/1 -> Mux/793
  "IW{1,1}(793,:)'"/1 -> dotprod793/1
  dotprod792/1 -> Mux/792
  "IW{1,1}(792,:)'"/1 -> dotprod792/1
  dotprod791/1 -> Mux/791
  "IW{1,1}(791,:)'"/1 -> dotprod791/1
  dotprod790/1 -> Mux/790
  "IW{1,1}(790,:)'"/1 -> dotprod790/1
  dotprod789/1 -> Mux/789
  "IW{1,1}(789,:)'"/1 -> dotprod789/1
  dotprod788/1 -> Mux/788
  "IW{1,1}(788,:)'"/1 -> dotprod788/1
  dotprod787/1 -> Mux/787
  "IW{1,1}(787,:)'"/1 -> dotprod787/1
  dotprod786/1 -> Mux/786
  "IW{1,1}(786,:)'"/1 -> dotprod786/1
  dotprod785/1 -> Mux/785
  "IW{1,1}(785,:)'"/1 -> dotprod785/1
  dotprod784/1 -> Mux/784
  "IW{1,1}(784,:)'"/1 -> dotprod784/1
  dotprod783/1 -> Mux/783
  "IW{1,1}(783,:)'"/1 -> dotprod783/1
  dotprod782/1 -> Mux/782
  "IW{1,1}(782,:)'"/1 -> dotprod782/1
  dotprod781/1 -> Mux/781
  "IW{1,1}(781,:)'"/1 -> dotprod781/1
  dotprod780/1 -> Mux/780
  "IW{1,1}(780,:)'"/1 -> dotprod780/1
  dotprod779/1 -> Mux/779
  "IW{1,1}(779,:)'"/1 -> dotprod779/1
  dotprod778/1 -> Mux/778
  "IW{1,1}(778,:)'"/1 -> dotprod778/1
  dotprod777/1 -> Mux/777
  "IW{1,1}(777,:)'"/1 -> dotprod777/1
  dotprod776/1 -> Mux/776
  "IW{1,1}(776,:)'"/1 -> dotprod776/1
  dotprod775/1 -> Mux/775
  "IW{1,1}(775,:)'"/1 -> dotprod775/1
  dotprod774/1 -> Mux/774
  "IW{1,1}(774,:)'"/1 -> dotprod774/1
  dotprod773/1 -> Mux/773
  "IW{1,1}(773,:)'"/1 -> dotprod773/1
  dotprod772/1 -> Mux/772
  "IW{1,1}(772,:)'"/1 -> dotprod772/1
  dotprod771/1 -> Mux/771
  "IW{1,1}(771,:)'"/1 -> dotprod771/1
  dotprod770/1 -> Mux/770
  "IW{1,1}(770,:)'"/1 -> dotprod770/1
  dotprod769/1 -> Mux/769
  "IW{1,1}(769,:)'"/1 -> dotprod769/1
  dotprod768/1 -> Mux/768
  "IW{1,1}(768,:)'"/1 -> dotprod768/1
  dotprod767/1 -> Mux/767
  "IW{1,1}(767,:)'"/1 -> dotprod767/1
  dotprod766/1 -> Mux/766
  "IW{1,1}(766,:)'"/1 -> dotprod766/1
  dotprod765/1 -> Mux/765
  "IW{1,1}(765,:)'"/1 -> dotprod765/1
  dotprod764/1 -> Mux/764
  "IW{1,1}(764,:)'"/1 -> dotprod764/1
  dotprod763/1 -> Mux/763
  "IW{1,1}(763,:)'"/1 -> dotprod763/1
  dotprod762/1 -> Mux/762
  "IW{1,1}(762,:)'"/1 -> dotprod762/1
  dotprod761/1 -> Mux/761
  "IW{1,1}(761,:)'"/1 -> dotprod761/1
  dotprod760/1 -> Mux/760
  "IW{1,1}(760,:)'"/1 -> dotprod760/1
  dotprod759/1 -> Mux/759
  "IW{1,1}(759,:)'"/1 -> dotprod759/1
  dotprod758/1 -> Mux/758
  "IW{1,1}(758,:)'"/1 -> dotprod758/1
  dotprod757/1 -> Mux/757
  "IW{1,1}(757,:)'"/1 -> dotprod757/1
  dotprod756/1 -> Mux/756
  "IW{1,1}(756,:)'"/1 -> dotprod756/1
  dotprod755/1 -> Mux/755
  "IW{1,1}(755,:)'"/1 -> dotprod755/1
  dotprod754/1 -> Mux/754
  "IW{1,1}(754,:)'"/1 -> dotprod754/1
  dotprod753/1 -> Mux/753
  "IW{1,1}(753,:)'"/1 -> dotprod753/1
  dotprod752/1 -> Mux/752
  "IW{1,1}(752,:)'"/1 -> dotprod752/1
  dotprod751/1 -> Mux/751
  "IW{1,1}(751,:)'"/1 -> dotprod751/1
  dotprod750/1 -> Mux/750
  "IW{1,1}(750,:)'"/1 -> dotprod750/1
  dotprod749/1 -> Mux/749
  "IW{1,1}(749,:)'"/1 -> dotprod749/1
  dotprod748/1 -> Mux/748
  "IW{1,1}(748,:)'"/1 -> dotprod748/1
  dotprod747/1 -> Mux/747
  "IW{1,1}(747,:)'"/1 -> dotprod747/1
  dotprod746/1 -> Mux/746
  "IW{1,1}(746,:)'"/1 -> dotprod746/1
  dotprod745/1 -> Mux/745
  "IW{1,1}(745,:)'"/1 -> dotprod745/1
  dotprod744/1 -> Mux/744
  "IW{1,1}(744,:)'"/1 -> dotprod744/1
  dotprod743/1 -> Mux/743
  "IW{1,1}(743,:)'"/1 -> dotprod743/1
  dotprod742/1 -> Mux/742
  "IW{1,1}(742,:)'"/1 -> dotprod742/1
  dotprod741/1 -> Mux/741
  "IW{1,1}(741,:)'"/1 -> dotprod741/1
  dotprod740/1 -> Mux/740
  "IW{1,1}(740,:)'"/1 -> dotprod740/1
  dotprod739/1 -> Mux/739
  "IW{1,1}(739,:)'"/1 -> dotprod739/1
  dotprod738/1 -> Mux/738
  "IW{1,1}(738,:)'"/1 -> dotprod738/1
  dotprod737/1 -> Mux/737
  "IW{1,1}(737,:)'"/1 -> dotprod737/1
  dotprod736/1 -> Mux/736
  "IW{1,1}(736,:)'"/1 -> dotprod736/1
  dotprod735/1 -> Mux/735
  "IW{1,1}(735,:)'"/1 -> dotprod735/1
  dotprod734/1 -> Mux/734
  "IW{1,1}(734,:)'"/1 -> dotprod734/1
  dotprod733/1 -> Mux/733
  "IW{1,1}(733,:)'"/1 -> dotprod733/1
  dotprod732/1 -> Mux/732
  "IW{1,1}(732,:)'"/1 -> dotprod732/1
  dotprod731/1 -> Mux/731
  "IW{1,1}(731,:)'"/1 -> dotprod731/1
  dotprod730/1 -> Mux/730
  "IW{1,1}(730,:)'"/1 -> dotprod730/1
  dotprod729/1 -> Mux/729
  "IW{1,1}(729,:)'"/1 -> dotprod729/1
  dotprod728/1 -> Mux/728
  "IW{1,1}(728,:)'"/1 -> dotprod728/1
  dotprod727/1 -> Mux/727
  "IW{1,1}(727,:)'"/1 -> dotprod727/1
  dotprod726/1 -> Mux/726
  "IW{1,1}(726,:)'"/1 -> dotprod726/1
  dotprod725/1 -> Mux/725
  "IW{1,1}(725,:)'"/1 -> dotprod725/1
  dotprod724/1 -> Mux/724
  "IW{1,1}(724,:)'"/1 -> dotprod724/1
  dotprod723/1 -> Mux/723
  "IW{1,1}(723,:)'"/1 -> dotprod723/1
  dotprod722/1 -> Mux/722
  "IW{1,1}(722,:)'"/1 -> dotprod722/1
  dotprod721/1 -> Mux/721
  "IW{1,1}(721,:)'"/1 -> dotprod721/1
  dotprod720/1 -> Mux/720
  "IW{1,1}(720,:)'"/1 -> dotprod720/1
  dotprod719/1 -> Mux/719
  "IW{1,1}(719,:)'"/1 -> dotprod719/1
  dotprod718/1 -> Mux/718
  "IW{1,1}(718,:)'"/1 -> dotprod718/1
  dotprod717/1 -> Mux/717
  "IW{1,1}(717,:)'"/1 -> dotprod717/1
  dotprod716/1 -> Mux/716
  "IW{1,1}(716,:)'"/1 -> dotprod716/1
  dotprod715/1 -> Mux/715
  "IW{1,1}(715,:)'"/1 -> dotprod715/1
  dotprod714/1 -> Mux/714
  "IW{1,1}(714,:)'"/1 -> dotprod714/1
  dotprod713/1 -> Mux/713
  "IW{1,1}(713,:)'"/1 -> dotprod713/1
  dotprod712/1 -> Mux/712
  "IW{1,1}(712,:)'"/1 -> dotprod712/1
  dotprod711/1 -> Mux/711
  "IW{1,1}(711,:)'"/1 -> dotprod711/1
  dotprod710/1 -> Mux/710
  "IW{1,1}(710,:)'"/1 -> dotprod710/1
  dotprod709/1 -> Mux/709
  "IW{1,1}(709,:)'"/1 -> dotprod709/1
  dotprod708/1 -> Mux/708
  "IW{1,1}(708,:)'"/1 -> dotprod708/1
  dotprod707/1 -> Mux/707
  "IW{1,1}(707,:)'"/1 -> dotprod707/1
  dotprod706/1 -> Mux/706
  "IW{1,1}(706,:)'"/1 -> dotprod706/1
  dotprod705/1 -> Mux/705
  "IW{1,1}(705,:)'"/1 -> dotprod705/1
  dotprod704/1 -> Mux/704
  "IW{1,1}(704,:)'"/1 -> dotprod704/1
  dotprod703/1 -> Mux/703
  "IW{1,1}(703,:)'"/1 -> dotprod703/1
  dotprod702/1 -> Mux/702
  "IW{1,1}(702,:)'"/1 -> dotprod702/1
  dotprod701/1 -> Mux/701
  "IW{1,1}(701,:)'"/1 -> dotprod701/1
  dotprod700/1 -> Mux/700
  "IW{1,1}(700,:)'"/1 -> dotprod700/1
  dotprod699/1 -> Mux/699
  "IW{1,1}(699,:)'"/1 -> dotprod699/1
  dotprod698/1 -> Mux/698
  "IW{1,1}(698,:)'"/1 -> dotprod698/1
  dotprod697/1 -> Mux/697
  "IW{1,1}(697,:)'"/1 -> dotprod697/1
  dotprod696/1 -> Mux/696
  "IW{1,1}(696,:)'"/1 -> dotprod696/1
  dotprod695/1 -> Mux/695
  "IW{1,1}(695,:)'"/1 -> dotprod695/1
  dotprod694/1 -> Mux/694
  "IW{1,1}(694,:)'"/1 -> dotprod694/1
  dotprod693/1 -> Mux/693
  "IW{1,1}(693,:)'"/1 -> dotprod693/1
  dotprod692/1 -> Mux/692
  "IW{1,1}(692,:)'"/1 -> dotprod692/1
  dotprod691/1 -> Mux/691
  "IW{1,1}(691,:)'"/1 -> dotprod691/1
  dotprod690/1 -> Mux/690
  "IW{1,1}(690,:)'"/1 -> dotprod690/1
  dotprod689/1 -> Mux/689
  "IW{1,1}(689,:)'"/1 -> dotprod689/1
  dotprod688/1 -> Mux/688
  "IW{1,1}(688,:)'"/1 -> dotprod688/1
  dotprod687/1 -> Mux/687
  "IW{1,1}(687,:)'"/1 -> dotprod687/1
  dotprod686/1 -> Mux/686
  "IW{1,1}(686,:)'"/1 -> dotprod686/1
  dotprod685/1 -> Mux/685
  "IW{1,1}(685,:)'"/1 -> dotprod685/1
  dotprod684/1 -> Mux/684
  "IW{1,1}(684,:)'"/1 -> dotprod684/1
  dotprod683/1 -> Mux/683
  "IW{1,1}(683,:)'"/1 -> dotprod683/1
  dotprod682/1 -> Mux/682
  "IW{1,1}(682,:)'"/1 -> dotprod682/1
  dotprod681/1 -> Mux/681
  "IW{1,1}(681,:)'"/1 -> dotprod681/1
  dotprod680/1 -> Mux/680
  "IW{1,1}(680,:)'"/1 -> dotprod680/1
  dotprod679/1 -> Mux/679
  "IW{1,1}(679,:)'"/1 -> dotprod679/1
  dotprod678/1 -> Mux/678
  "IW{1,1}(678,:)'"/1 -> dotprod678/1
  dotprod677/1 -> Mux/677
  "IW{1,1}(677,:)'"/1 -> dotprod677/1
  dotprod676/1 -> Mux/676
  "IW{1,1}(676,:)'"/1 -> dotprod676/1
  dotprod675/1 -> Mux/675
  "IW{1,1}(675,:)'"/1 -> dotprod675/1
  dotprod674/1 -> Mux/674
  "IW{1,1}(674,:)'"/1 -> dotprod674/1
  dotprod673/1 -> Mux/673
  "IW{1,1}(673,:)'"/1 -> dotprod673/1
  dotprod672/1 -> Mux/672
  "IW{1,1}(672,:)'"/1 -> dotprod672/1
  dotprod671/1 -> Mux/671
  "IW{1,1}(671,:)'"/1 -> dotprod671/1
  dotprod670/1 -> Mux/670
  "IW{1,1}(670,:)'"/1 -> dotprod670/1
  dotprod669/1 -> Mux/669
  "IW{1,1}(669,:)'"/1 -> dotprod669/1
  dotprod668/1 -> Mux/668
  "IW{1,1}(668,:)'"/1 -> dotprod668/1
  dotprod667/1 -> Mux/667
  "IW{1,1}(667,:)'"/1 -> dotprod667/1
  dotprod666/1 -> Mux/666
  "IW{1,1}(666,:)'"/1 -> dotprod666/1
  dotprod665/1 -> Mux/665
  "IW{1,1}(665,:)'"/1 -> dotprod665/1
  dotprod664/1 -> Mux/664
  "IW{1,1}(664,:)'"/1 -> dotprod664/1
  dotprod663/1 -> Mux/663
  "IW{1,1}(663,:)'"/1 -> dotprod663/1
  dotprod662/1 -> Mux/662
  "IW{1,1}(662,:)'"/1 -> dotprod662/1
  dotprod661/1 -> Mux/661
  "IW{1,1}(661,:)'"/1 -> dotprod661/1
  dotprod660/1 -> Mux/660
  "IW{1,1}(660,:)'"/1 -> dotprod660/1
  dotprod659/1 -> Mux/659
  "IW{1,1}(659,:)'"/1 -> dotprod659/1
  dotprod658/1 -> Mux/658
  "IW{1,1}(658,:)'"/1 -> dotprod658/1
  dotprod657/1 -> Mux/657
  "IW{1,1}(657,:)'"/1 -> dotprod657/1
  dotprod656/1 -> Mux/656
  "IW{1,1}(656,:)'"/1 -> dotprod656/1
  dotprod655/1 -> Mux/655
  "IW{1,1}(655,:)'"/1 -> dotprod655/1
  dotprod654/1 -> Mux/654
  "IW{1,1}(654,:)'"/1 -> dotprod654/1
  dotprod653/1 -> Mux/653
  "IW{1,1}(653,:)'"/1 -> dotprod653/1
  dotprod652/1 -> Mux/652
  "IW{1,1}(652,:)'"/1 -> dotprod652/1
  dotprod651/1 -> Mux/651
  "IW{1,1}(651,:)'"/1 -> dotprod651/1
  dotprod650/1 -> Mux/650
  "IW{1,1}(650,:)'"/1 -> dotprod650/1
  dotprod649/1 -> Mux/649
  "IW{1,1}(649,:)'"/1 -> dotprod649/1
  dotprod648/1 -> Mux/648
  "IW{1,1}(648,:)'"/1 -> dotprod648/1
  dotprod647/1 -> Mux/647
  "IW{1,1}(647,:)'"/1 -> dotprod647/1
  dotprod646/1 -> Mux/646
  "IW{1,1}(646,:)'"/1 -> dotprod646/1
  dotprod645/1 -> Mux/645
  "IW{1,1}(645,:)'"/1 -> dotprod645/1
  dotprod644/1 -> Mux/644
  "IW{1,1}(644,:)'"/1 -> dotprod644/1
  dotprod643/1 -> Mux/643
  "IW{1,1}(643,:)'"/1 -> dotprod643/1
  dotprod642/1 -> Mux/642
  "IW{1,1}(642,:)'"/1 -> dotprod642/1
  dotprod641/1 -> Mux/641
  "IW{1,1}(641,:)'"/1 -> dotprod641/1
  dotprod640/1 -> Mux/640
  "IW{1,1}(640,:)'"/1 -> dotprod640/1
  dotprod639/1 -> Mux/639
  "IW{1,1}(639,:)'"/1 -> dotprod639/1
  dotprod638/1 -> Mux/638
  "IW{1,1}(638,:)'"/1 -> dotprod638/1
  dotprod637/1 -> Mux/637
  "IW{1,1}(637,:)'"/1 -> dotprod637/1
  dotprod636/1 -> Mux/636
  "IW{1,1}(636,:)'"/1 -> dotprod636/1
  dotprod635/1 -> Mux/635
  "IW{1,1}(635,:)'"/1 -> dotprod635/1
  dotprod634/1 -> Mux/634
  "IW{1,1}(634,:)'"/1 -> dotprod634/1
  dotprod633/1 -> Mux/633
  "IW{1,1}(633,:)'"/1 -> dotprod633/1
  dotprod632/1 -> Mux/632
  "IW{1,1}(632,:)'"/1 -> dotprod632/1
  dotprod631/1 -> Mux/631
  "IW{1,1}(631,:)'"/1 -> dotprod631/1
  dotprod630/1 -> Mux/630
  "IW{1,1}(630,:)'"/1 -> dotprod630/1
  dotprod629/1 -> Mux/629
  "IW{1,1}(629,:)'"/1 -> dotprod629/1
  dotprod628/1 -> Mux/628
  "IW{1,1}(628,:)'"/1 -> dotprod628/1
  dotprod627/1 -> Mux/627
  "IW{1,1}(627,:)'"/1 -> dotprod627/1
  dotprod626/1 -> Mux/626
  "IW{1,1}(626,:)'"/1 -> dotprod626/1
  dotprod625/1 -> Mux/625
  "IW{1,1}(625,:)'"/1 -> dotprod625/1
  dotprod624/1 -> Mux/624
  "IW{1,1}(624,:)'"/1 -> dotprod624/1
  dotprod623/1 -> Mux/623
  "IW{1,1}(623,:)'"/1 -> dotprod623/1
  dotprod622/1 -> Mux/622
  "IW{1,1}(622,:)'"/1 -> dotprod622/1
  dotprod621/1 -> Mux/621
  "IW{1,1}(621,:)'"/1 -> dotprod621/1
  dotprod620/1 -> Mux/620
  "IW{1,1}(620,:)'"/1 -> dotprod620/1
  dotprod619/1 -> Mux/619
  "IW{1,1}(619,:)'"/1 -> dotprod619/1
  dotprod618/1 -> Mux/618
  "IW{1,1}(618,:)'"/1 -> dotprod618/1
  dotprod617/1 -> Mux/617
  "IW{1,1}(617,:)'"/1 -> dotprod617/1
  dotprod616/1 -> Mux/616
  "IW{1,1}(616,:)'"/1 -> dotprod616/1
  dotprod615/1 -> Mux/615
  "IW{1,1}(615,:)'"/1 -> dotprod615/1
  dotprod614/1 -> Mux/614
  "IW{1,1}(614,:)'"/1 -> dotprod614/1
  dotprod613/1 -> Mux/613
  "IW{1,1}(613,:)'"/1 -> dotprod613/1
  dotprod612/1 -> Mux/612
  "IW{1,1}(612,:)'"/1 -> dotprod612/1
  dotprod611/1 -> Mux/611
  "IW{1,1}(611,:)'"/1 -> dotprod611/1
  dotprod610/1 -> Mux/610
  "IW{1,1}(610,:)'"/1 -> dotprod610/1
  dotprod609/1 -> Mux/609
  "IW{1,1}(609,:)'"/1 -> dotprod609/1
  dotprod608/1 -> Mux/608
  "IW{1,1}(608,:)'"/1 -> dotprod608/1
  dotprod607/1 -> Mux/607
  "IW{1,1}(607,:)'"/1 -> dotprod607/1
  dotprod606/1 -> Mux/606
  "IW{1,1}(606,:)'"/1 -> dotprod606/1
  dotprod605/1 -> Mux/605
  "IW{1,1}(605,:)'"/1 -> dotprod605/1
  dotprod604/1 -> Mux/604
  "IW{1,1}(604,:)'"/1 -> dotprod604/1
  dotprod603/1 -> Mux/603
  "IW{1,1}(603,:)'"/1 -> dotprod603/1
  dotprod602/1 -> Mux/602
  "IW{1,1}(602,:)'"/1 -> dotprod602/1
  dotprod601/1 -> Mux/601
  "IW{1,1}(601,:)'"/1 -> dotprod601/1
  dotprod600/1 -> Mux/600
  "IW{1,1}(600,:)'"/1 -> dotprod600/1
  dotprod599/1 -> Mux/599
  "IW{1,1}(599,:)'"/1 -> dotprod599/1
  dotprod598/1 -> Mux/598
  "IW{1,1}(598,:)'"/1 -> dotprod598/1
  dotprod597/1 -> Mux/597
  "IW{1,1}(597,:)'"/1 -> dotprod597/1
  dotprod596/1 -> Mux/596
  "IW{1,1}(596,:)'"/1 -> dotprod596/1
  dotprod595/1 -> Mux/595
  "IW{1,1}(595,:)'"/1 -> dotprod595/1
  dotprod594/1 -> Mux/594
  "IW{1,1}(594,:)'"/1 -> dotprod594/1
  dotprod593/1 -> Mux/593
  "IW{1,1}(593,:)'"/1 -> dotprod593/1
  dotprod592/1 -> Mux/592
  "IW{1,1}(592,:)'"/1 -> dotprod592/1
  dotprod591/1 -> Mux/591
  "IW{1,1}(591,:)'"/1 -> dotprod591/1
  dotprod590/1 -> Mux/590
  "IW{1,1}(590,:)'"/1 -> dotprod590/1
  dotprod589/1 -> Mux/589
  "IW{1,1}(589,:)'"/1 -> dotprod589/1
  dotprod588/1 -> Mux/588
  "IW{1,1}(588,:)'"/1 -> dotprod588/1
  dotprod587/1 -> Mux/587
  "IW{1,1}(587,:)'"/1 -> dotprod587/1
  dotprod586/1 -> Mux/586
  "IW{1,1}(586,:)'"/1 -> dotprod586/1
  dotprod585/1 -> Mux/585
  "IW{1,1}(585,:)'"/1 -> dotprod585/1
  dotprod584/1 -> Mux/584
  "IW{1,1}(584,:)'"/1 -> dotprod584/1
  dotprod583/1 -> Mux/583
  "IW{1,1}(583,:)'"/1 -> dotprod583/1
  dotprod582/1 -> Mux/582
  "IW{1,1}(582,:)'"/1 -> dotprod582/1
  dotprod581/1 -> Mux/581
  "IW{1,1}(581,:)'"/1 -> dotprod581/1
  dotprod580/1 -> Mux/580
  "IW{1,1}(580,:)'"/1 -> dotprod580/1
  dotprod579/1 -> Mux/579
  "IW{1,1}(579,:)'"/1 -> dotprod579/1
  dotprod578/1 -> Mux/578
  "IW{1,1}(578,:)'"/1 -> dotprod578/1
  dotprod577/1 -> Mux/577
  "IW{1,1}(577,:)'"/1 -> dotprod577/1
  dotprod576/1 -> Mux/576
  "IW{1,1}(576,:)'"/1 -> dotprod576/1
  dotprod575/1 -> Mux/575
  "IW{1,1}(575,:)'"/1 -> dotprod575/1
  dotprod574/1 -> Mux/574
  "IW{1,1}(574,:)'"/1 -> dotprod574/1
  dotprod573/1 -> Mux/573
  "IW{1,1}(573,:)'"/1 -> dotprod573/1
  dotprod572/1 -> Mux/572
  "IW{1,1}(572,:)'"/1 -> dotprod572/1
  dotprod571/1 -> Mux/571
  "IW{1,1}(571,:)'"/1 -> dotprod571/1
  dotprod570/1 -> Mux/570
  "IW{1,1}(570,:)'"/1 -> dotprod570/1
  dotprod569/1 -> Mux/569
  "IW{1,1}(569,:)'"/1 -> dotprod569/1
  dotprod568/1 -> Mux/568
  "IW{1,1}(568,:)'"/1 -> dotprod568/1
  dotprod567/1 -> Mux/567
  "IW{1,1}(567,:)'"/1 -> dotprod567/1
  dotprod566/1 -> Mux/566
  "IW{1,1}(566,:)'"/1 -> dotprod566/1
  dotprod565/1 -> Mux/565
  "IW{1,1}(565,:)'"/1 -> dotprod565/1
  dotprod564/1 -> Mux/564
  "IW{1,1}(564,:)'"/1 -> dotprod564/1
  dotprod563/1 -> Mux/563
  "IW{1,1}(563,:)'"/1 -> dotprod563/1
  dotprod562/1 -> Mux/562
  "IW{1,1}(562,:)'"/1 -> dotprod562/1
  dotprod561/1 -> Mux/561
  "IW{1,1}(561,:)'"/1 -> dotprod561/1
  dotprod560/1 -> Mux/560
  "IW{1,1}(560,:)'"/1 -> dotprod560/1
  dotprod559/1 -> Mux/559
  "IW{1,1}(559,:)'"/1 -> dotprod559/1
  dotprod558/1 -> Mux/558
  "IW{1,1}(558,:)'"/1 -> dotprod558/1
  dotprod557/1 -> Mux/557
  "IW{1,1}(557,:)'"/1 -> dotprod557/1
  dotprod556/1 -> Mux/556
  "IW{1,1}(556,:)'"/1 -> dotprod556/1
  dotprod555/1 -> Mux/555
  "IW{1,1}(555,:)'"/1 -> dotprod555/1
  dotprod554/1 -> Mux/554
  "IW{1,1}(554,:)'"/1 -> dotprod554/1
  dotprod553/1 -> Mux/553
  "IW{1,1}(553,:)'"/1 -> dotprod553/1
  dotprod552/1 -> Mux/552
  "IW{1,1}(552,:)'"/1 -> dotprod552/1
  dotprod551/1 -> Mux/551
  "IW{1,1}(551,:)'"/1 -> dotprod551/1
  dotprod550/1 -> Mux/550
  "IW{1,1}(550,:)'"/1 -> dotprod550/1
  dotprod549/1 -> Mux/549
  "IW{1,1}(549,:)'"/1 -> dotprod549/1
  dotprod548/1 -> Mux/548
  "IW{1,1}(548,:)'"/1 -> dotprod548/1
  dotprod547/1 -> Mux/547
  "IW{1,1}(547,:)'"/1 -> dotprod547/1
  dotprod546/1 -> Mux/546
  "IW{1,1}(546,:)'"/1 -> dotprod546/1
  dotprod545/1 -> Mux/545
  "IW{1,1}(545,:)'"/1 -> dotprod545/1
  dotprod544/1 -> Mux/544
  "IW{1,1}(544,:)'"/1 -> dotprod544/1
  dotprod543/1 -> Mux/543
  "IW{1,1}(543,:)'"/1 -> dotprod543/1
  dotprod542/1 -> Mux/542
  "IW{1,1}(542,:)'"/1 -> dotprod542/1
  dotprod541/1 -> Mux/541
  "IW{1,1}(541,:)'"/1 -> dotprod541/1
  dotprod540/1 -> Mux/540
  "IW{1,1}(540,:)'"/1 -> dotprod540/1
  dotprod539/1 -> Mux/539
  "IW{1,1}(539,:)'"/1 -> dotprod539/1
  dotprod538/1 -> Mux/538
  "IW{1,1}(538,:)'"/1 -> dotprod538/1
  dotprod537/1 -> Mux/537
  "IW{1,1}(537,:)'"/1 -> dotprod537/1
  dotprod536/1 -> Mux/536
  "IW{1,1}(536,:)'"/1 -> dotprod536/1
  dotprod535/1 -> Mux/535
  "IW{1,1}(535,:)'"/1 -> dotprod535/1
  dotprod534/1 -> Mux/534
  "IW{1,1}(534,:)'"/1 -> dotprod534/1
  dotprod533/1 -> Mux/533
  "IW{1,1}(533,:)'"/1 -> dotprod533/1
  dotprod532/1 -> Mux/532
  "IW{1,1}(532,:)'"/1 -> dotprod532/1
  dotprod531/1 -> Mux/531
  "IW{1,1}(531,:)'"/1 -> dotprod531/1
  dotprod530/1 -> Mux/530
  "IW{1,1}(530,:)'"/1 -> dotprod530/1
  dotprod529/1 -> Mux/529
  "IW{1,1}(529,:)'"/1 -> dotprod529/1
  dotprod528/1 -> Mux/528
  "IW{1,1}(528,:)'"/1 -> dotprod528/1
  dotprod527/1 -> Mux/527
  "IW{1,1}(527,:)'"/1 -> dotprod527/1
  dotprod526/1 -> Mux/526
  "IW{1,1}(526,:)'"/1 -> dotprod526/1
  dotprod525/1 -> Mux/525
  "IW{1,1}(525,:)'"/1 -> dotprod525/1
  dotprod524/1 -> Mux/524
  "IW{1,1}(524,:)'"/1 -> dotprod524/1
  dotprod523/1 -> Mux/523
  "IW{1,1}(523,:)'"/1 -> dotprod523/1
  dotprod522/1 -> Mux/522
  "IW{1,1}(522,:)'"/1 -> dotprod522/1
  dotprod521/1 -> Mux/521
  "IW{1,1}(521,:)'"/1 -> dotprod521/1
  dotprod520/1 -> Mux/520
  "IW{1,1}(520,:)'"/1 -> dotprod520/1
  dotprod519/1 -> Mux/519
  "IW{1,1}(519,:)'"/1 -> dotprod519/1
  dotprod518/1 -> Mux/518
  "IW{1,1}(518,:)'"/1 -> dotprod518/1
  dotprod517/1 -> Mux/517
  "IW{1,1}(517,:)'"/1 -> dotprod517/1
  dotprod516/1 -> Mux/516
  "IW{1,1}(516,:)'"/1 -> dotprod516/1
  dotprod515/1 -> Mux/515
  "IW{1,1}(515,:)'"/1 -> dotprod515/1
  dotprod514/1 -> Mux/514
  "IW{1,1}(514,:)'"/1 -> dotprod514/1
  dotprod513/1 -> Mux/513
  "IW{1,1}(513,:)'"/1 -> dotprod513/1
  dotprod512/1 -> Mux/512
  "IW{1,1}(512,:)'"/1 -> dotprod512/1
  dotprod511/1 -> Mux/511
  "IW{1,1}(511,:)'"/1 -> dotprod511/1
  dotprod510/1 -> Mux/510
  "IW{1,1}(510,:)'"/1 -> dotprod510/1
  dotprod509/1 -> Mux/509
  "IW{1,1}(509,:)'"/1 -> dotprod509/1
  dotprod508/1 -> Mux/508
  "IW{1,1}(508,:)'"/1 -> dotprod508/1
  dotprod507/1 -> Mux/507
  "IW{1,1}(507,:)'"/1 -> dotprod507/1
  dotprod506/1 -> Mux/506
  "IW{1,1}(506,:)'"/1 -> dotprod506/1
  dotprod505/1 -> Mux/505
  "IW{1,1}(505,:)'"/1 -> dotprod505/1
  dotprod504/1 -> Mux/504
  "IW{1,1}(504,:)'"/1 -> dotprod504/1
  dotprod503/1 -> Mux/503
  "IW{1,1}(503,:)'"/1 -> dotprod503/1
  dotprod502/1 -> Mux/502
  "IW{1,1}(502,:)'"/1 -> dotprod502/1
  dotprod501/1 -> Mux/501
  "IW{1,1}(501,:)'"/1 -> dotprod501/1
  dotprod500/1 -> Mux/500
  "IW{1,1}(500,:)'"/1 -> dotprod500/1
  dotprod499/1 -> Mux/499
  "IW{1,1}(499,:)'"/1 -> dotprod499/1
  dotprod498/1 -> Mux/498
  "IW{1,1}(498,:)'"/1 -> dotprod498/1
  dotprod497/1 -> Mux/497
  "IW{1,1}(497,:)'"/1 -> dotprod497/1
  dotprod496/1 -> Mux/496
  "IW{1,1}(496,:)'"/1 -> dotprod496/1
  dotprod495/1 -> Mux/495
  "IW{1,1}(495,:)'"/1 -> dotprod495/1
  dotprod494/1 -> Mux/494
  "IW{1,1}(494,:)'"/1 -> dotprod494/1
  dotprod493/1 -> Mux/493
  "IW{1,1}(493,:)'"/1 -> dotprod493/1
  dotprod492/1 -> Mux/492
  "IW{1,1}(492,:)'"/1 -> dotprod492/1
  dotprod491/1 -> Mux/491
  "IW{1,1}(491,:)'"/1 -> dotprod491/1
  dotprod490/1 -> Mux/490
  "IW{1,1}(490,:)'"/1 -> dotprod490/1
  dotprod489/1 -> Mux/489
  "IW{1,1}(489,:)'"/1 -> dotprod489/1
  dotprod488/1 -> Mux/488
  "IW{1,1}(488,:)'"/1 -> dotprod488/1
  dotprod487/1 -> Mux/487
  "IW{1,1}(487,:)'"/1 -> dotprod487/1
  dotprod486/1 -> Mux/486
  "IW{1,1}(486,:)'"/1 -> dotprod486/1
  dotprod485/1 -> Mux/485
  "IW{1,1}(485,:)'"/1 -> dotprod485/1
  dotprod484/1 -> Mux/484
  "IW{1,1}(484,:)'"/1 -> dotprod484/1
  dotprod483/1 -> Mux/483
  "IW{1,1}(483,:)'"/1 -> dotprod483/1
  dotprod482/1 -> Mux/482
  "IW{1,1}(482,:)'"/1 -> dotprod482/1
  dotprod481/1 -> Mux/481
  "IW{1,1}(481,:)'"/1 -> dotprod481/1
  dotprod480/1 -> Mux/480
  "IW{1,1}(480,:)'"/1 -> dotprod480/1
  dotprod479/1 -> Mux/479
  "IW{1,1}(479,:)'"/1 -> dotprod479/1
  dotprod478/1 -> Mux/478
  "IW{1,1}(478,:)'"/1 -> dotprod478/1
  dotprod477/1 -> Mux/477
  "IW{1,1}(477,:)'"/1 -> dotprod477/1
  dotprod476/1 -> Mux/476
  "IW{1,1}(476,:)'"/1 -> dotprod476/1
  dotprod475/1 -> Mux/475
  "IW{1,1}(475,:)'"/1 -> dotprod475/1
  dotprod474/1 -> Mux/474
  "IW{1,1}(474,:)'"/1 -> dotprod474/1
  dotprod473/1 -> Mux/473
  "IW{1,1}(473,:)'"/1 -> dotprod473/1
  dotprod472/1 -> Mux/472
  "IW{1,1}(472,:)'"/1 -> dotprod472/1
  dotprod471/1 -> Mux/471
  "IW{1,1}(471,:)'"/1 -> dotprod471/1
  dotprod470/1 -> Mux/470
  "IW{1,1}(470,:)'"/1 -> dotprod470/1
  dotprod469/1 -> Mux/469
  "IW{1,1}(469,:)'"/1 -> dotprod469/1
  dotprod468/1 -> Mux/468
  "IW{1,1}(468,:)'"/1 -> dotprod468/1
  dotprod467/1 -> Mux/467
  "IW{1,1}(467,:)'"/1 -> dotprod467/1
  dotprod466/1 -> Mux/466
  "IW{1,1}(466,:)'"/1 -> dotprod466/1
  dotprod465/1 -> Mux/465
  "IW{1,1}(465,:)'"/1 -> dotprod465/1
  dotprod464/1 -> Mux/464
  "IW{1,1}(464,:)'"/1 -> dotprod464/1
  dotprod463/1 -> Mux/463
  "IW{1,1}(463,:)'"/1 -> dotprod463/1
  dotprod462/1 -> Mux/462
  "IW{1,1}(462,:)'"/1 -> dotprod462/1
  dotprod461/1 -> Mux/461
  "IW{1,1}(461,:)'"/1 -> dotprod461/1
  dotprod460/1 -> Mux/460
  "IW{1,1}(460,:)'"/1 -> dotprod460/1
  dotprod459/1 -> Mux/459
  "IW{1,1}(459,:)'"/1 -> dotprod459/1
  dotprod458/1 -> Mux/458
  "IW{1,1}(458,:)'"/1 -> dotprod458/1
  dotprod457/1 -> Mux/457
  "IW{1,1}(457,:)'"/1 -> dotprod457/1
  dotprod456/1 -> Mux/456
  "IW{1,1}(456,:)'"/1 -> dotprod456/1
  dotprod455/1 -> Mux/455
  "IW{1,1}(455,:)'"/1 -> dotprod455/1
  dotprod454/1 -> Mux/454
  "IW{1,1}(454,:)'"/1 -> dotprod454/1
  dotprod453/1 -> Mux/453
  "IW{1,1}(453,:)'"/1 -> dotprod453/1
  dotprod452/1 -> Mux/452
  "IW{1,1}(452,:)'"/1 -> dotprod452/1
  dotprod451/1 -> Mux/451
  "IW{1,1}(451,:)'"/1 -> dotprod451/1
  dotprod450/1 -> Mux/450
  "IW{1,1}(450,:)'"/1 -> dotprod450/1
  dotprod449/1 -> Mux/449
  "IW{1,1}(449,:)'"/1 -> dotprod449/1
  dotprod448/1 -> Mux/448
  "IW{1,1}(448,:)'"/1 -> dotprod448/1
  dotprod447/1 -> Mux/447
  "IW{1,1}(447,:)'"/1 -> dotprod447/1
  dotprod446/1 -> Mux/446
  "IW{1,1}(446,:)'"/1 -> dotprod446/1
  dotprod445/1 -> Mux/445
  "IW{1,1}(445,:)'"/1 -> dotprod445/1
  dotprod444/1 -> Mux/444
  "IW{1,1}(444,:)'"/1 -> dotprod444/1
  dotprod443/1 -> Mux/443
  "IW{1,1}(443,:)'"/1 -> dotprod443/1
  dotprod442/1 -> Mux/442
  "IW{1,1}(442,:)'"/1 -> dotprod442/1
  dotprod441/1 -> Mux/441
  "IW{1,1}(441,:)'"/1 -> dotprod441/1
  dotprod440/1 -> Mux/440
  "IW{1,1}(440,:)'"/1 -> dotprod440/1
  dotprod439/1 -> Mux/439
  "IW{1,1}(439,:)'"/1 -> dotprod439/1
  dotprod438/1 -> Mux/438
  "IW{1,1}(438,:)'"/1 -> dotprod438/1
  dotprod437/1 -> Mux/437
  "IW{1,1}(437,:)'"/1 -> dotprod437/1
  dotprod436/1 -> Mux/436
  "IW{1,1}(436,:)'"/1 -> dotprod436/1
  dotprod435/1 -> Mux/435
  "IW{1,1}(435,:)'"/1 -> dotprod435/1
  dotprod434/1 -> Mux/434
  "IW{1,1}(434,:)'"/1 -> dotprod434/1
  dotprod433/1 -> Mux/433
  "IW{1,1}(433,:)'"/1 -> dotprod433/1
  dotprod432/1 -> Mux/432
  "IW{1,1}(432,:)'"/1 -> dotprod432/1
  dotprod431/1 -> Mux/431
  "IW{1,1}(431,:)'"/1 -> dotprod431/1
  dotprod430/1 -> Mux/430
  "IW{1,1}(430,:)'"/1 -> dotprod430/1
  dotprod429/1 -> Mux/429
  "IW{1,1}(429,:)'"/1 -> dotprod429/1
  dotprod428/1 -> Mux/428
  "IW{1,1}(428,:)'"/1 -> dotprod428/1
  dotprod427/1 -> Mux/427
  "IW{1,1}(427,:)'"/1 -> dotprod427/1
  dotprod426/1 -> Mux/426
  "IW{1,1}(426,:)'"/1 -> dotprod426/1
  dotprod425/1 -> Mux/425
  "IW{1,1}(425,:)'"/1 -> dotprod425/1
  dotprod424/1 -> Mux/424
  "IW{1,1}(424,:)'"/1 -> dotprod424/1
  dotprod423/1 -> Mux/423
  "IW{1,1}(423,:)'"/1 -> dotprod423/1
  dotprod422/1 -> Mux/422
  "IW{1,1}(422,:)'"/1 -> dotprod422/1
  dotprod421/1 -> Mux/421
  "IW{1,1}(421,:)'"/1 -> dotprod421/1
  dotprod420/1 -> Mux/420
  "IW{1,1}(420,:)'"/1 -> dotprod420/1
  dotprod419/1 -> Mux/419
  "IW{1,1}(419,:)'"/1 -> dotprod419/1
  dotprod418/1 -> Mux/418
  "IW{1,1}(418,:)'"/1 -> dotprod418/1
  dotprod417/1 -> Mux/417
  "IW{1,1}(417,:)'"/1 -> dotprod417/1
  dotprod416/1 -> Mux/416
  "IW{1,1}(416,:)'"/1 -> dotprod416/1
  dotprod415/1 -> Mux/415
  "IW{1,1}(415,:)'"/1 -> dotprod415/1
  dotprod414/1 -> Mux/414
  "IW{1,1}(414,:)'"/1 -> dotprod414/1
  dotprod413/1 -> Mux/413
  "IW{1,1}(413,:)'"/1 -> dotprod413/1
  dotprod412/1 -> Mux/412
  "IW{1,1}(412,:)'"/1 -> dotprod412/1
  dotprod411/1 -> Mux/411
  "IW{1,1}(411,:)'"/1 -> dotprod411/1
  dotprod410/1 -> Mux/410
  "IW{1,1}(410,:)'"/1 -> dotprod410/1
  dotprod409/1 -> Mux/409
  "IW{1,1}(409,:)'"/1 -> dotprod409/1
  dotprod408/1 -> Mux/408
  "IW{1,1}(408,:)'"/1 -> dotprod408/1
  dotprod407/1 -> Mux/407
  "IW{1,1}(407,:)'"/1 -> dotprod407/1
  dotprod406/1 -> Mux/406
  "IW{1,1}(406,:)'"/1 -> dotprod406/1
  dotprod405/1 -> Mux/405
  "IW{1,1}(405,:)'"/1 -> dotprod405/1
  dotprod404/1 -> Mux/404
  "IW{1,1}(404,:)'"/1 -> dotprod404/1
  dotprod403/1 -> Mux/403
  "IW{1,1}(403,:)'"/1 -> dotprod403/1
  dotprod402/1 -> Mux/402
  "IW{1,1}(402,:)'"/1 -> dotprod402/1
  dotprod401/1 -> Mux/401
  "IW{1,1}(401,:)'"/1 -> dotprod401/1
  dotprod400/1 -> Mux/400
  "IW{1,1}(400,:)'"/1 -> dotprod400/1
  dotprod399/1 -> Mux/399
  "IW{1,1}(399,:)'"/1 -> dotprod399/1
  dotprod398/1 -> Mux/398
  "IW{1,1}(398,:)'"/1 -> dotprod398/1
  dotprod397/1 -> Mux/397
  "IW{1,1}(397,:)'"/1 -> dotprod397/1
  dotprod396/1 -> Mux/396
  "IW{1,1}(396,:)'"/1 -> dotprod396/1
  dotprod395/1 -> Mux/395
  "IW{1,1}(395,:)'"/1 -> dotprod395/1
  dotprod394/1 -> Mux/394
  "IW{1,1}(394,:)'"/1 -> dotprod394/1
  dotprod393/1 -> Mux/393
  "IW{1,1}(393,:)'"/1 -> dotprod393/1
  dotprod392/1 -> Mux/392
  "IW{1,1}(392,:)'"/1 -> dotprod392/1
  dotprod391/1 -> Mux/391
  "IW{1,1}(391,:)'"/1 -> dotprod391/1
  dotprod390/1 -> Mux/390
  "IW{1,1}(390,:)'"/1 -> dotprod390/1
  dotprod389/1 -> Mux/389
  "IW{1,1}(389,:)'"/1 -> dotprod389/1
  dotprod388/1 -> Mux/388
  "IW{1,1}(388,:)'"/1 -> dotprod388/1
  dotprod387/1 -> Mux/387
  "IW{1,1}(387,:)'"/1 -> dotprod387/1
  dotprod386/1 -> Mux/386
  "IW{1,1}(386,:)'"/1 -> dotprod386/1
  dotprod385/1 -> Mux/385
  "IW{1,1}(385,:)'"/1 -> dotprod385/1
  dotprod384/1 -> Mux/384
  "IW{1,1}(384,:)'"/1 -> dotprod384/1
  dotprod383/1 -> Mux/383
  "IW{1,1}(383,:)'"/1 -> dotprod383/1
  dotprod382/1 -> Mux/382
  "IW{1,1}(382,:)'"/1 -> dotprod382/1
  dotprod381/1 -> Mux/381
  "IW{1,1}(381,:)'"/1 -> dotprod381/1
  dotprod380/1 -> Mux/380
  "IW{1,1}(380,:)'"/1 -> dotprod380/1
  dotprod379/1 -> Mux/379
  "IW{1,1}(379,:)'"/1 -> dotprod379/1
  dotprod378/1 -> Mux/378
  "IW{1,1}(378,:)'"/1 -> dotprod378/1
  dotprod377/1 -> Mux/377
  "IW{1,1}(377,:)'"/1 -> dotprod377/1
  dotprod376/1 -> Mux/376
  "IW{1,1}(376,:)'"/1 -> dotprod376/1
  dotprod375/1 -> Mux/375
  "IW{1,1}(375,:)'"/1 -> dotprod375/1
  dotprod374/1 -> Mux/374
  "IW{1,1}(374,:)'"/1 -> dotprod374/1
  dotprod373/1 -> Mux/373
  "IW{1,1}(373,:)'"/1 -> dotprod373/1
  dotprod372/1 -> Mux/372
  "IW{1,1}(372,:)'"/1 -> dotprod372/1
  dotprod371/1 -> Mux/371
  "IW{1,1}(371,:)'"/1 -> dotprod371/1
  dotprod370/1 -> Mux/370
  "IW{1,1}(370,:)'"/1 -> dotprod370/1
  dotprod369/1 -> Mux/369
  "IW{1,1}(369,:)'"/1 -> dotprod369/1
  dotprod368/1 -> Mux/368
  "IW{1,1}(368,:)'"/1 -> dotprod368/1
  dotprod367/1 -> Mux/367
  "IW{1,1}(367,:)'"/1 -> dotprod367/1
  dotprod366/1 -> Mux/366
  "IW{1,1}(366,:)'"/1 -> dotprod366/1
  dotprod365/1 -> Mux/365
  "IW{1,1}(365,:)'"/1 -> dotprod365/1
  dotprod364/1 -> Mux/364
  "IW{1,1}(364,:)'"/1 -> dotprod364/1
  dotprod363/1 -> Mux/363
  "IW{1,1}(363,:)'"/1 -> dotprod363/1
  dotprod362/1 -> Mux/362
  "IW{1,1}(362,:)'"/1 -> dotprod362/1
  dotprod361/1 -> Mux/361
  "IW{1,1}(361,:)'"/1 -> dotprod361/1
  dotprod360/1 -> Mux/360
  "IW{1,1}(360,:)'"/1 -> dotprod360/1
  dotprod359/1 -> Mux/359
  "IW{1,1}(359,:)'"/1 -> dotprod359/1
  dotprod358/1 -> Mux/358
  "IW{1,1}(358,:)'"/1 -> dotprod358/1
  dotprod357/1 -> Mux/357
  "IW{1,1}(357,:)'"/1 -> dotprod357/1
  dotprod356/1 -> Mux/356
  "IW{1,1}(356,:)'"/1 -> dotprod356/1
  dotprod355/1 -> Mux/355
  "IW{1,1}(355,:)'"/1 -> dotprod355/1
  dotprod354/1 -> Mux/354
  "IW{1,1}(354,:)'"/1 -> dotprod354/1
  dotprod353/1 -> Mux/353
  "IW{1,1}(353,:)'"/1 -> dotprod353/1
  dotprod352/1 -> Mux/352
  "IW{1,1}(352,:)'"/1 -> dotprod352/1
  dotprod351/1 -> Mux/351
  "IW{1,1}(351,:)'"/1 -> dotprod351/1
  dotprod350/1 -> Mux/350
  "IW{1,1}(350,:)'"/1 -> dotprod350/1
  dotprod349/1 -> Mux/349
  "IW{1,1}(349,:)'"/1 -> dotprod349/1
  dotprod348/1 -> Mux/348
  "IW{1,1}(348,:)'"/1 -> dotprod348/1
  dotprod347/1 -> Mux/347
  "IW{1,1}(347,:)'"/1 -> dotprod347/1
  dotprod346/1 -> Mux/346
  "IW{1,1}(346,:)'"/1 -> dotprod346/1
  dotprod345/1 -> Mux/345
  "IW{1,1}(345,:)'"/1 -> dotprod345/1
  dotprod344/1 -> Mux/344
  "IW{1,1}(344,:)'"/1 -> dotprod344/1
  dotprod343/1 -> Mux/343
  "IW{1,1}(343,:)'"/1 -> dotprod343/1
  dotprod342/1 -> Mux/342
  "IW{1,1}(342,:)'"/1 -> dotprod342/1
  dotprod341/1 -> Mux/341
  "IW{1,1}(341,:)'"/1 -> dotprod341/1
  dotprod340/1 -> Mux/340
  "IW{1,1}(340,:)'"/1 -> dotprod340/1
  dotprod339/1 -> Mux/339
  "IW{1,1}(339,:)'"/1 -> dotprod339/1
  dotprod338/1 -> Mux/338
  "IW{1,1}(338,:)'"/1 -> dotprod338/1
  dotprod337/1 -> Mux/337
  "IW{1,1}(337,:)'"/1 -> dotprod337/1
  dotprod336/1 -> Mux/336
  "IW{1,1}(336,:)'"/1 -> dotprod336/1
  dotprod335/1 -> Mux/335
  "IW{1,1}(335,:)'"/1 -> dotprod335/1
  dotprod334/1 -> Mux/334
  "IW{1,1}(334,:)'"/1 -> dotprod334/1
  dotprod333/1 -> Mux/333
  "IW{1,1}(333,:)'"/1 -> dotprod333/1
  dotprod332/1 -> Mux/332
  "IW{1,1}(332,:)'"/1 -> dotprod332/1
  dotprod331/1 -> Mux/331
  "IW{1,1}(331,:)'"/1 -> dotprod331/1
  dotprod330/1 -> Mux/330
  "IW{1,1}(330,:)'"/1 -> dotprod330/1
  dotprod329/1 -> Mux/329
  "IW{1,1}(329,:)'"/1 -> dotprod329/1
  dotprod328/1 -> Mux/328
  "IW{1,1}(328,:)'"/1 -> dotprod328/1
  dotprod327/1 -> Mux/327
  "IW{1,1}(327,:)'"/1 -> dotprod327/1
  dotprod326/1 -> Mux/326
  "IW{1,1}(326,:)'"/1 -> dotprod326/1
  dotprod325/1 -> Mux/325
  "IW{1,1}(325,:)'"/1 -> dotprod325/1
  dotprod324/1 -> Mux/324
  "IW{1,1}(324,:)'"/1 -> dotprod324/1
  dotprod323/1 -> Mux/323
  "IW{1,1}(323,:)'"/1 -> dotprod323/1
  dotprod322/1 -> Mux/322
  "IW{1,1}(322,:)'"/1 -> dotprod322/1
  dotprod321/1 -> Mux/321
  "IW{1,1}(321,:)'"/1 -> dotprod321/1
  dotprod320/1 -> Mux/320
  "IW{1,1}(320,:)'"/1 -> dotprod320/1
  dotprod319/1 -> Mux/319
  "IW{1,1}(319,:)'"/1 -> dotprod319/1
  dotprod318/1 -> Mux/318
  "IW{1,1}(318,:)'"/1 -> dotprod318/1
  dotprod317/1 -> Mux/317
  "IW{1,1}(317,:)'"/1 -> dotprod317/1
  dotprod316/1 -> Mux/316
  "IW{1,1}(316,:)'"/1 -> dotprod316/1
  dotprod315/1 -> Mux/315
  "IW{1,1}(315,:)'"/1 -> dotprod315/1
  dotprod314/1 -> Mux/314
  "IW{1,1}(314,:)'"/1 -> dotprod314/1
  dotprod313/1 -> Mux/313
  "IW{1,1}(313,:)'"/1 -> dotprod313/1
  dotprod312/1 -> Mux/312
  "IW{1,1}(312,:)'"/1 -> dotprod312/1
  dotprod311/1 -> Mux/311
  "IW{1,1}(311,:)'"/1 -> dotprod311/1
  dotprod310/1 -> Mux/310
  "IW{1,1}(310,:)'"/1 -> dotprod310/1
  dotprod309/1 -> Mux/309
  "IW{1,1}(309,:)'"/1 -> dotprod309/1
  dotprod308/1 -> Mux/308
  "IW{1,1}(308,:)'"/1 -> dotprod308/1
  dotprod307/1 -> Mux/307
  "IW{1,1}(307,:)'"/1 -> dotprod307/1
  dotprod306/1 -> Mux/306
  "IW{1,1}(306,:)'"/1 -> dotprod306/1
  dotprod305/1 -> Mux/305
  "IW{1,1}(305,:)'"/1 -> dotprod305/1
  dotprod304/1 -> Mux/304
  "IW{1,1}(304,:)'"/1 -> dotprod304/1
  dotprod303/1 -> Mux/303
  "IW{1,1}(303,:)'"/1 -> dotprod303/1
  dotprod302/1 -> Mux/302
  "IW{1,1}(302,:)'"/1 -> dotprod302/1
  dotprod301/1 -> Mux/301
  "IW{1,1}(301,:)'"/1 -> dotprod301/1
  dotprod300/1 -> Mux/300
  "IW{1,1}(300,:)'"/1 -> dotprod300/1
  dotprod299/1 -> Mux/299
  "IW{1,1}(299,:)'"/1 -> dotprod299/1
  dotprod298/1 -> Mux/298
  "IW{1,1}(298,:)'"/1 -> dotprod298/1
  dotprod297/1 -> Mux/297
  "IW{1,1}(297,:)'"/1 -> dotprod297/1
  dotprod296/1 -> Mux/296
  "IW{1,1}(296,:)'"/1 -> dotprod296/1
  dotprod295/1 -> Mux/295
  "IW{1,1}(295,:)'"/1 -> dotprod295/1
  dotprod294/1 -> Mux/294
  "IW{1,1}(294,:)'"/1 -> dotprod294/1
  dotprod293/1 -> Mux/293
  "IW{1,1}(293,:)'"/1 -> dotprod293/1
  dotprod292/1 -> Mux/292
  "IW{1,1}(292,:)'"/1 -> dotprod292/1
  dotprod291/1 -> Mux/291
  "IW{1,1}(291,:)'"/1 -> dotprod291/1
  dotprod290/1 -> Mux/290
  "IW{1,1}(290,:)'"/1 -> dotprod290/1
  dotprod289/1 -> Mux/289
  "IW{1,1}(289,:)'"/1 -> dotprod289/1
  dotprod288/1 -> Mux/288
  "IW{1,1}(288,:)'"/1 -> dotprod288/1
  dotprod287/1 -> Mux/287
  "IW{1,1}(287,:)'"/1 -> dotprod287/1
  dotprod286/1 -> Mux/286
  "IW{1,1}(286,:)'"/1 -> dotprod286/1
  dotprod285/1 -> Mux/285
  "IW{1,1}(285,:)'"/1 -> dotprod285/1
  dotprod284/1 -> Mux/284
  "IW{1,1}(284,:)'"/1 -> dotprod284/1
  dotprod283/1 -> Mux/283
  "IW{1,1}(283,:)'"/1 -> dotprod283/1
  dotprod282/1 -> Mux/282
  "IW{1,1}(282,:)'"/1 -> dotprod282/1
  dotprod281/1 -> Mux/281
  "IW{1,1}(281,:)'"/1 -> dotprod281/1
  dotprod280/1 -> Mux/280
  "IW{1,1}(280,:)'"/1 -> dotprod280/1
  dotprod279/1 -> Mux/279
  "IW{1,1}(279,:)'"/1 -> dotprod279/1
  dotprod278/1 -> Mux/278
  "IW{1,1}(278,:)'"/1 -> dotprod278/1
  dotprod277/1 -> Mux/277
  "IW{1,1}(277,:)'"/1 -> dotprod277/1
  dotprod276/1 -> Mux/276
  "IW{1,1}(276,:)'"/1 -> dotprod276/1
  dotprod275/1 -> Mux/275
  "IW{1,1}(275,:)'"/1 -> dotprod275/1
  dotprod274/1 -> Mux/274
  "IW{1,1}(274,:)'"/1 -> dotprod274/1
  dotprod273/1 -> Mux/273
  "IW{1,1}(273,:)'"/1 -> dotprod273/1
  dotprod272/1 -> Mux/272
  "IW{1,1}(272,:)'"/1 -> dotprod272/1
  dotprod271/1 -> Mux/271
  "IW{1,1}(271,:)'"/1 -> dotprod271/1
  dotprod270/1 -> Mux/270
  "IW{1,1}(270,:)'"/1 -> dotprod270/1
  dotprod269/1 -> Mux/269
  "IW{1,1}(269,:)'"/1 -> dotprod269/1
  dotprod268/1 -> Mux/268
  "IW{1,1}(268,:)'"/1 -> dotprod268/1
  dotprod267/1 -> Mux/267
  "IW{1,1}(267,:)'"/1 -> dotprod267/1
  dotprod266/1 -> Mux/266
  "IW{1,1}(266,:)'"/1 -> dotprod266/1
  dotprod265/1 -> Mux/265
  "IW{1,1}(265,:)'"/1 -> dotprod265/1
  dotprod264/1 -> Mux/264
  "IW{1,1}(264,:)'"/1 -> dotprod264/1
  dotprod263/1 -> Mux/263
  "IW{1,1}(263,:)'"/1 -> dotprod263/1
  dotprod262/1 -> Mux/262
  "IW{1,1}(262,:)'"/1 -> dotprod262/1
  dotprod261/1 -> Mux/261
  "IW{1,1}(261,:)'"/1 -> dotprod261/1
  dotprod260/1 -> Mux/260
  "IW{1,1}(260,:)'"/1 -> dotprod260/1
  dotprod259/1 -> Mux/259
  "IW{1,1}(259,:)'"/1 -> dotprod259/1
  dotprod258/1 -> Mux/258
  "IW{1,1}(258,:)'"/1 -> dotprod258/1
  dotprod257/1 -> Mux/257
  "IW{1,1}(257,:)'"/1 -> dotprod257/1
  dotprod256/1 -> Mux/256
  "IW{1,1}(256,:)'"/1 -> dotprod256/1
  dotprod255/1 -> Mux/255
  "IW{1,1}(255,:)'"/1 -> dotprod255/1
  dotprod254/1 -> Mux/254
  "IW{1,1}(254,:)'"/1 -> dotprod254/1
  dotprod253/1 -> Mux/253
  "IW{1,1}(253,:)'"/1 -> dotprod253/1
  dotprod252/1 -> Mux/252
  "IW{1,1}(252,:)'"/1 -> dotprod252/1
  dotprod251/1 -> Mux/251
  "IW{1,1}(251,:)'"/1 -> dotprod251/1
  dotprod250/1 -> Mux/250
  "IW{1,1}(250,:)'"/1 -> dotprod250/1
  dotprod249/1 -> Mux/249
  "IW{1,1}(249,:)'"/1 -> dotprod249/1
  dotprod248/1 -> Mux/248
  "IW{1,1}(248,:)'"/1 -> dotprod248/1
  dotprod247/1 -> Mux/247
  "IW{1,1}(247,:)'"/1 -> dotprod247/1
  dotprod246/1 -> Mux/246
  "IW{1,1}(246,:)'"/1 -> dotprod246/1
  dotprod245/1 -> Mux/245
  "IW{1,1}(245,:)'"/1 -> dotprod245/1
  dotprod244/1 -> Mux/244
  "IW{1,1}(244,:)'"/1 -> dotprod244/1
  dotprod243/1 -> Mux/243
  "IW{1,1}(243,:)'"/1 -> dotprod243/1
  dotprod242/1 -> Mux/242
  "IW{1,1}(242,:)'"/1 -> dotprod242/1
  dotprod241/1 -> Mux/241
  "IW{1,1}(241,:)'"/1 -> dotprod241/1
  dotprod240/1 -> Mux/240
  "IW{1,1}(240,:)'"/1 -> dotprod240/1
  dotprod239/1 -> Mux/239
  "IW{1,1}(239,:)'"/1 -> dotprod239/1
  dotprod238/1 -> Mux/238
  "IW{1,1}(238,:)'"/1 -> dotprod238/1
  dotprod237/1 -> Mux/237
  "IW{1,1}(237,:)'"/1 -> dotprod237/1
  dotprod236/1 -> Mux/236
  "IW{1,1}(236,:)'"/1 -> dotprod236/1
  dotprod235/1 -> Mux/235
  "IW{1,1}(235,:)'"/1 -> dotprod235/1
  dotprod234/1 -> Mux/234
  "IW{1,1}(234,:)'"/1 -> dotprod234/1
  dotprod233/1 -> Mux/233
  "IW{1,1}(233,:)'"/1 -> dotprod233/1
  dotprod232/1 -> Mux/232
  "IW{1,1}(232,:)'"/1 -> dotprod232/1
  dotprod231/1 -> Mux/231
  "IW{1,1}(231,:)'"/1 -> dotprod231/1
  dotprod230/1 -> Mux/230
  "IW{1,1}(230,:)'"/1 -> dotprod230/1
  dotprod229/1 -> Mux/229
  "IW{1,1}(229,:)'"/1 -> dotprod229/1
  dotprod228/1 -> Mux/228
  "IW{1,1}(228,:)'"/1 -> dotprod228/1
  dotprod227/1 -> Mux/227
  "IW{1,1}(227,:)'"/1 -> dotprod227/1
  dotprod226/1 -> Mux/226
  "IW{1,1}(226,:)'"/1 -> dotprod226/1
  dotprod225/1 -> Mux/225
  "IW{1,1}(225,:)'"/1 -> dotprod225/1
  dotprod224/1 -> Mux/224
  "IW{1,1}(224,:)'"/1 -> dotprod224/1
  dotprod223/1 -> Mux/223
  "IW{1,1}(223,:)'"/1 -> dotprod223/1
  dotprod222/1 -> Mux/222
  "IW{1,1}(222,:)'"/1 -> dotprod222/1
  dotprod221/1 -> Mux/221
  "IW{1,1}(221,:)'"/1 -> dotprod221/1
  dotprod220/1 -> Mux/220
  "IW{1,1}(220,:)'"/1 -> dotprod220/1
  dotprod219/1 -> Mux/219
  "IW{1,1}(219,:)'"/1 -> dotprod219/1
  dotprod218/1 -> Mux/218
  "IW{1,1}(218,:)'"/1 -> dotprod218/1
  dotprod217/1 -> Mux/217
  "IW{1,1}(217,:)'"/1 -> dotprod217/1
  dotprod216/1 -> Mux/216
  "IW{1,1}(216,:)'"/1 -> dotprod216/1
  dotprod215/1 -> Mux/215
  "IW{1,1}(215,:)'"/1 -> dotprod215/1
  dotprod214/1 -> Mux/214
  "IW{1,1}(214,:)'"/1 -> dotprod214/1
  dotprod213/1 -> Mux/213
  "IW{1,1}(213,:)'"/1 -> dotprod213/1
  dotprod212/1 -> Mux/212
  "IW{1,1}(212,:)'"/1 -> dotprod212/1
  dotprod211/1 -> Mux/211
  "IW{1,1}(211,:)'"/1 -> dotprod211/1
  dotprod210/1 -> Mux/210
  "IW{1,1}(210,:)'"/1 -> dotprod210/1
  dotprod209/1 -> Mux/209
  "IW{1,1}(209,:)'"/1 -> dotprod209/1
  dotprod208/1 -> Mux/208
  "IW{1,1}(208,:)'"/1 -> dotprod208/1
  dotprod207/1 -> Mux/207
  "IW{1,1}(207,:)'"/1 -> dotprod207/1
  dotprod206/1 -> Mux/206
  "IW{1,1}(206,:)'"/1 -> dotprod206/1
  dotprod205/1 -> Mux/205
  "IW{1,1}(205,:)'"/1 -> dotprod205/1
  dotprod204/1 -> Mux/204
  "IW{1,1}(204,:)'"/1 -> dotprod204/1
  dotprod203/1 -> Mux/203
  "IW{1,1}(203,:)'"/1 -> dotprod203/1
  dotprod202/1 -> Mux/202
  "IW{1,1}(202,:)'"/1 -> dotprod202/1
  dotprod201/1 -> Mux/201
  "IW{1,1}(201,:)'"/1 -> dotprod201/1
  dotprod200/1 -> Mux/200
  "IW{1,1}(200,:)'"/1 -> dotprod200/1
  dotprod199/1 -> Mux/199
  "IW{1,1}(199,:)'"/1 -> dotprod199/1
  dotprod198/1 -> Mux/198
  "IW{1,1}(198,:)'"/1 -> dotprod198/1
  dotprod197/1 -> Mux/197
  "IW{1,1}(197,:)'"/1 -> dotprod197/1
  dotprod196/1 -> Mux/196
  "IW{1,1}(196,:)'"/1 -> dotprod196/1
  dotprod195/1 -> Mux/195
  "IW{1,1}(195,:)'"/1 -> dotprod195/1
  dotprod194/1 -> Mux/194
  "IW{1,1}(194,:)'"/1 -> dotprod194/1
  dotprod193/1 -> Mux/193
  "IW{1,1}(193,:)'"/1 -> dotprod193/1
  dotprod192/1 -> Mux/192
  "IW{1,1}(192,:)'"/1 -> dotprod192/1
  dotprod191/1 -> Mux/191
  "IW{1,1}(191,:)'"/1 -> dotprod191/1
  dotprod190/1 -> Mux/190
  "IW{1,1}(190,:)'"/1 -> dotprod190/1
  dotprod189/1 -> Mux/189
  "IW{1,1}(189,:)'"/1 -> dotprod189/1
  dotprod188/1 -> Mux/188
  "IW{1,1}(188,:)'"/1 -> dotprod188/1
  dotprod187/1 -> Mux/187
  "IW{1,1}(187,:)'"/1 -> dotprod187/1
  dotprod186/1 -> Mux/186
  "IW{1,1}(186,:)'"/1 -> dotprod186/1
  dotprod185/1 -> Mux/185
  "IW{1,1}(185,:)'"/1 -> dotprod185/1
  dotprod184/1 -> Mux/184
  "IW{1,1}(184,:)'"/1 -> dotprod184/1
  dotprod183/1 -> Mux/183
  "IW{1,1}(183,:)'"/1 -> dotprod183/1
  dotprod182/1 -> Mux/182
  "IW{1,1}(182,:)'"/1 -> dotprod182/1
  dotprod181/1 -> Mux/181
  "IW{1,1}(181,:)'"/1 -> dotprod181/1
  dotprod180/1 -> Mux/180
  "IW{1,1}(180,:)'"/1 -> dotprod180/1
  dotprod179/1 -> Mux/179
  "IW{1,1}(179,:)'"/1 -> dotprod179/1
  dotprod178/1 -> Mux/178
  "IW{1,1}(178,:)'"/1 -> dotprod178/1
  dotprod177/1 -> Mux/177
  "IW{1,1}(177,:)'"/1 -> dotprod177/1
  dotprod176/1 -> Mux/176
  "IW{1,1}(176,:)'"/1 -> dotprod176/1
  dotprod175/1 -> Mux/175
  "IW{1,1}(175,:)'"/1 -> dotprod175/1
  dotprod174/1 -> Mux/174
  "IW{1,1}(174,:)'"/1 -> dotprod174/1
  dotprod173/1 -> Mux/173
  "IW{1,1}(173,:)'"/1 -> dotprod173/1
  dotprod172/1 -> Mux/172
  "IW{1,1}(172,:)'"/1 -> dotprod172/1
  dotprod171/1 -> Mux/171
  "IW{1,1}(171,:)'"/1 -> dotprod171/1
  dotprod170/1 -> Mux/170
  "IW{1,1}(170,:)'"/1 -> dotprod170/1
  dotprod169/1 -> Mux/169
  "IW{1,1}(169,:)'"/1 -> dotprod169/1
  dotprod168/1 -> Mux/168
  "IW{1,1}(168,:)'"/1 -> dotprod168/1
  dotprod167/1 -> Mux/167
  "IW{1,1}(167,:)'"/1 -> dotprod167/1
  dotprod166/1 -> Mux/166
  "IW{1,1}(166,:)'"/1 -> dotprod166/1
  dotprod165/1 -> Mux/165
  "IW{1,1}(165,:)'"/1 -> dotprod165/1
  dotprod164/1 -> Mux/164
  "IW{1,1}(164,:)'"/1 -> dotprod164/1
  dotprod163/1 -> Mux/163
  "IW{1,1}(163,:)'"/1 -> dotprod163/1
  dotprod162/1 -> Mux/162
  "IW{1,1}(162,:)'"/1 -> dotprod162/1
  dotprod161/1 -> Mux/161
  "IW{1,1}(161,:)'"/1 -> dotprod161/1
  dotprod160/1 -> Mux/160
  "IW{1,1}(160,:)'"/1 -> dotprod160/1
  dotprod159/1 -> Mux/159
  "IW{1,1}(159,:)'"/1 -> dotprod159/1
  dotprod158/1 -> Mux/158
  "IW{1,1}(158,:)'"/1 -> dotprod158/1
  dotprod157/1 -> Mux/157
  "IW{1,1}(157,:)'"/1 -> dotprod157/1
  dotprod156/1 -> Mux/156
  "IW{1,1}(156,:)'"/1 -> dotprod156/1
  dotprod155/1 -> Mux/155
  "IW{1,1}(155,:)'"/1 -> dotprod155/1
  dotprod154/1 -> Mux/154
  "IW{1,1}(154,:)'"/1 -> dotprod154/1
  dotprod153/1 -> Mux/153
  "IW{1,1}(153,:)'"/1 -> dotprod153/1
  dotprod152/1 -> Mux/152
  "IW{1,1}(152,:)'"/1 -> dotprod152/1
  dotprod151/1 -> Mux/151
  "IW{1,1}(151,:)'"/1 -> dotprod151/1
  dotprod150/1 -> Mux/150
  "IW{1,1}(150,:)'"/1 -> dotprod150/1
  dotprod149/1 -> Mux/149
  "IW{1,1}(149,:)'"/1 -> dotprod149/1
  dotprod148/1 -> Mux/148
  "IW{1,1}(148,:)'"/1 -> dotprod148/1
  dotprod147/1 -> Mux/147
  "IW{1,1}(147,:)'"/1 -> dotprod147/1
  dotprod146/1 -> Mux/146
  "IW{1,1}(146,:)'"/1 -> dotprod146/1
  dotprod145/1 -> Mux/145
  "IW{1,1}(145,:)'"/1 -> dotprod145/1
  dotprod144/1 -> Mux/144
  "IW{1,1}(144,:)'"/1 -> dotprod144/1
  dotprod143/1 -> Mux/143
  "IW{1,1}(143,:)'"/1 -> dotprod143/1
  dotprod142/1 -> Mux/142
  "IW{1,1}(142,:)'"/1 -> dotprod142/1
  dotprod141/1 -> Mux/141
  "IW{1,1}(141,:)'"/1 -> dotprod141/1
  dotprod140/1 -> Mux/140
  "IW{1,1}(140,:)'"/1 -> dotprod140/1
  dotprod139/1 -> Mux/139
  "IW{1,1}(139,:)'"/1 -> dotprod139/1
  dotprod138/1 -> Mux/138
  "IW{1,1}(138,:)'"/1 -> dotprod138/1
  dotprod137/1 -> Mux/137
  "IW{1,1}(137,:)'"/1 -> dotprod137/1
  dotprod136/1 -> Mux/136
  "IW{1,1}(136,:)'"/1 -> dotprod136/1
  dotprod135/1 -> Mux/135
  "IW{1,1}(135,:)'"/1 -> dotprod135/1
  dotprod134/1 -> Mux/134
  "IW{1,1}(134,:)'"/1 -> dotprod134/1
  dotprod133/1 -> Mux/133
  "IW{1,1}(133,:)'"/1 -> dotprod133/1
  dotprod132/1 -> Mux/132
  "IW{1,1}(132,:)'"/1 -> dotprod132/1
  dotprod131/1 -> Mux/131
  "IW{1,1}(131,:)'"/1 -> dotprod131/1
  dotprod130/1 -> Mux/130
  "IW{1,1}(130,:)'"/1 -> dotprod130/1
  dotprod129/1 -> Mux/129
  "IW{1,1}(129,:)'"/1 -> dotprod129/1
  dotprod128/1 -> Mux/128
  "IW{1,1}(128,:)'"/1 -> dotprod128/1
  dotprod127/1 -> Mux/127
  "IW{1,1}(127,:)'"/1 -> dotprod127/1
  dotprod126/1 -> Mux/126
  "IW{1,1}(126,:)'"/1 -> dotprod126/1
  dotprod125/1 -> Mux/125
  "IW{1,1}(125,:)'"/1 -> dotprod125/1
  dotprod124/1 -> Mux/124
  "IW{1,1}(124,:)'"/1 -> dotprod124/1
  dotprod123/1 -> Mux/123
  "IW{1,1}(123,:)'"/1 -> dotprod123/1
  dotprod122/1 -> Mux/122
  "IW{1,1}(122,:)'"/1 -> dotprod122/1
  dotprod121/1 -> Mux/121
  "IW{1,1}(121,:)'"/1 -> dotprod121/1
  dotprod120/1 -> Mux/120
  "IW{1,1}(120,:)'"/1 -> dotprod120/1
  dotprod119/1 -> Mux/119
  "IW{1,1}(119,:)'"/1 -> dotprod119/1
  dotprod118/1 -> Mux/118
  "IW{1,1}(118,:)'"/1 -> dotprod118/1
  dotprod117/1 -> Mux/117
  "IW{1,1}(117,:)'"/1 -> dotprod117/1
  dotprod116/1 -> Mux/116
  "IW{1,1}(116,:)'"/1 -> dotprod116/1
  dotprod115/1 -> Mux/115
  "IW{1,1}(115,:)'"/1 -> dotprod115/1
  dotprod114/1 -> Mux/114
  "IW{1,1}(114,:)'"/1 -> dotprod114/1
  dotprod113/1 -> Mux/113
  "IW{1,1}(113,:)'"/1 -> dotprod113/1
  dotprod112/1 -> Mux/112
  "IW{1,1}(112,:)'"/1 -> dotprod112/1
  dotprod111/1 -> Mux/111
  "IW{1,1}(111,:)'"/1 -> dotprod111/1
  dotprod110/1 -> Mux/110
  "IW{1,1}(110,:)'"/1 -> dotprod110/1
  dotprod109/1 -> Mux/109
  "IW{1,1}(109,:)'"/1 -> dotprod109/1
  dotprod108/1 -> Mux/108
  "IW{1,1}(108,:)'"/1 -> dotprod108/1
  dotprod107/1 -> Mux/107
  "IW{1,1}(107,:)'"/1 -> dotprod107/1
  dotprod106/1 -> Mux/106
  "IW{1,1}(106,:)'"/1 -> dotprod106/1
  dotprod105/1 -> Mux/105
  "IW{1,1}(105,:)'"/1 -> dotprod105/1
  dotprod104/1 -> Mux/104
  "IW{1,1}(104,:)'"/1 -> dotprod104/1
  dotprod103/1 -> Mux/103
  "IW{1,1}(103,:)'"/1 -> dotprod103/1
  dotprod102/1 -> Mux/102
  "IW{1,1}(102,:)'"/1 -> dotprod102/1
  dotprod101/1 -> Mux/101
  "IW{1,1}(101,:)'"/1 -> dotprod101/1
  dotprod100/1 -> Mux/100
  "IW{1,1}(100,:)'"/1 -> dotprod100/1
  dotprod99/1 -> Mux/99
  "IW{1,1}(99,:)'"/1 -> dotprod99/1
  dotprod98/1 -> Mux/98
  "IW{1,1}(98,:)'"/1 -> dotprod98/1
  dotprod97/1 -> Mux/97
  "IW{1,1}(97,:)'"/1 -> dotprod97/1
  dotprod96/1 -> Mux/96
  "IW{1,1}(96,:)'"/1 -> dotprod96/1
  dotprod95/1 -> Mux/95
  "IW{1,1}(95,:)'"/1 -> dotprod95/1
  dotprod94/1 -> Mux/94
  "IW{1,1}(94,:)'"/1 -> dotprod94/1
  dotprod93/1 -> Mux/93
  "IW{1,1}(93,:)'"/1 -> dotprod93/1
  dotprod92/1 -> Mux/92
  "IW{1,1}(92,:)'"/1 -> dotprod92/1
  dotprod91/1 -> Mux/91
  "IW{1,1}(91,:)'"/1 -> dotprod91/1
  dotprod90/1 -> Mux/90
  "IW{1,1}(90,:)'"/1 -> dotprod90/1
  dotprod89/1 -> Mux/89
  "IW{1,1}(89,:)'"/1 -> dotprod89/1
  dotprod88/1 -> Mux/88
  "IW{1,1}(88,:)'"/1 -> dotprod88/1
  dotprod87/1 -> Mux/87
  "IW{1,1}(87,:)'"/1 -> dotprod87/1
  dotprod86/1 -> Mux/86
  "IW{1,1}(86,:)'"/1 -> dotprod86/1
  dotprod85/1 -> Mux/85
  "IW{1,1}(85,:)'"/1 -> dotprod85/1
  dotprod84/1 -> Mux/84
  "IW{1,1}(84,:)'"/1 -> dotprod84/1
  dotprod83/1 -> Mux/83
  "IW{1,1}(83,:)'"/1 -> dotprod83/1
  dotprod82/1 -> Mux/82
  "IW{1,1}(82,:)'"/1 -> dotprod82/1
  dotprod81/1 -> Mux/81
  "IW{1,1}(81,:)'"/1 -> dotprod81/1
  dotprod80/1 -> Mux/80
  "IW{1,1}(80,:)'"/1 -> dotprod80/1
  dotprod79/1 -> Mux/79
  "IW{1,1}(79,:)'"/1 -> dotprod79/1
  dotprod78/1 -> Mux/78
  "IW{1,1}(78,:)'"/1 -> dotprod78/1
  dotprod77/1 -> Mux/77
  "IW{1,1}(77,:)'"/1 -> dotprod77/1
  dotprod76/1 -> Mux/76
  "IW{1,1}(76,:)'"/1 -> dotprod76/1
  dotprod75/1 -> Mux/75
  "IW{1,1}(75,:)'"/1 -> dotprod75/1
  dotprod74/1 -> Mux/74
  "IW{1,1}(74,:)'"/1 -> dotprod74/1
  dotprod73/1 -> Mux/73
  "IW{1,1}(73,:)'"/1 -> dotprod73/1
  dotprod72/1 -> Mux/72
  "IW{1,1}(72,:)'"/1 -> dotprod72/1
  dotprod71/1 -> Mux/71
  "IW{1,1}(71,:)'"/1 -> dotprod71/1
  dotprod70/1 -> Mux/70
  "IW{1,1}(70,:)'"/1 -> dotprod70/1
  dotprod69/1 -> Mux/69
  "IW{1,1}(69,:)'"/1 -> dotprod69/1
  dotprod68/1 -> Mux/68
  "IW{1,1}(68,:)'"/1 -> dotprod68/1
  dotprod67/1 -> Mux/67
  "IW{1,1}(67,:)'"/1 -> dotprod67/1
  dotprod66/1 -> Mux/66
  "IW{1,1}(66,:)'"/1 -> dotprod66/1
  dotprod65/1 -> Mux/65
  "IW{1,1}(65,:)'"/1 -> dotprod65/1
  dotprod64/1 -> Mux/64
  "IW{1,1}(64,:)'"/1 -> dotprod64/1
  dotprod63/1 -> Mux/63
  "IW{1,1}(63,:)'"/1 -> dotprod63/1
  dotprod62/1 -> Mux/62
  "IW{1,1}(62,:)'"/1 -> dotprod62/1
  dotprod61/1 -> Mux/61
  "IW{1,1}(61,:)'"/1 -> dotprod61/1
  dotprod60/1 -> Mux/60
  "IW{1,1}(60,:)'"/1 -> dotprod60/1
  dotprod59/1 -> Mux/59
  "IW{1,1}(59,:)'"/1 -> dotprod59/1
  dotprod58/1 -> Mux/58
  "IW{1,1}(58,:)'"/1 -> dotprod58/1
  dotprod57/1 -> Mux/57
  "IW{1,1}(57,:)'"/1 -> dotprod57/1
  dotprod56/1 -> Mux/56
  "IW{1,1}(56,:)'"/1 -> dotprod56/1
  dotprod55/1 -> Mux/55
  "IW{1,1}(55,:)'"/1 -> dotprod55/1
  dotprod54/1 -> Mux/54
  "IW{1,1}(54,:)'"/1 -> dotprod54/1
  dotprod53/1 -> Mux/53
  "IW{1,1}(53,:)'"/1 -> dotprod53/1
  dotprod52/1 -> Mux/52
  "IW{1,1}(52,:)'"/1 -> dotprod52/1
  dotprod51/1 -> Mux/51
  "IW{1,1}(51,:)'"/1 -> dotprod51/1
  dotprod50/1 -> Mux/50
  "IW{1,1}(50,:)'"/1 -> dotprod50/1
  dotprod49/1 -> Mux/49
  "IW{1,1}(49,:)'"/1 -> dotprod49/1
  dotprod48/1 -> Mux/48
  "IW{1,1}(48,:)'"/1 -> dotprod48/1
  dotprod47/1 -> Mux/47
  "IW{1,1}(47,:)'"/1 -> dotprod47/1
  dotprod46/1 -> Mux/46
  "IW{1,1}(46,:)'"/1 -> dotprod46/1
  dotprod45/1 -> Mux/45
  "IW{1,1}(45,:)'"/1 -> dotprod45/1
  dotprod44/1 -> Mux/44
  "IW{1,1}(44,:)'"/1 -> dotprod44/1
  dotprod43/1 -> Mux/43
  "IW{1,1}(43,:)'"/1 -> dotprod43/1
  dotprod42/1 -> Mux/42
  "IW{1,1}(42,:)'"/1 -> dotprod42/1
  dotprod41/1 -> Mux/41
  "IW{1,1}(41,:)'"/1 -> dotprod41/1
  dotprod40/1 -> Mux/40
  "IW{1,1}(40,:)'"/1 -> dotprod40/1
  dotprod39/1 -> Mux/39
  "IW{1,1}(39,:)'"/1 -> dotprod39/1
  dotprod38/1 -> Mux/38
  "IW{1,1}(38,:)'"/1 -> dotprod38/1
  dotprod37/1 -> Mux/37
  "IW{1,1}(37,:)'"/1 -> dotprod37/1
  dotprod36/1 -> Mux/36
  "IW{1,1}(36,:)'"/1 -> dotprod36/1
  dotprod35/1 -> Mux/35
  "IW{1,1}(35,:)'"/1 -> dotprod35/1
  dotprod34/1 -> Mux/34
  "IW{1,1}(34,:)'"/1 -> dotprod34/1
  dotprod33/1 -> Mux/33
  "IW{1,1}(33,:)'"/1 -> dotprod33/1
  dotprod32/1 -> Mux/32
  "IW{1,1}(32,:)'"/1 -> dotprod32/1
  dotprod31/1 -> Mux/31
  "IW{1,1}(31,:)'"/1 -> dotprod31/1
  dotprod30/1 -> Mux/30
  "IW{1,1}(30,:)'"/1 -> dotprod30/1
  dotprod29/1 -> Mux/29
  "IW{1,1}(29,:)'"/1 -> dotprod29/1
  dotprod28/1 -> Mux/28
  "IW{1,1}(28,:)'"/1 -> dotprod28/1
  dotprod27/1 -> Mux/27
  "IW{1,1}(27,:)'"/1 -> dotprod27/1
  dotprod26/1 -> Mux/26
  "IW{1,1}(26,:)'"/1 -> dotprod26/1
  dotprod25/1 -> Mux/25
  "IW{1,1}(25,:)'"/1 -> dotprod25/1
  dotprod24/1 -> Mux/24
  "IW{1,1}(24,:)'"/1 -> dotprod24/1
  dotprod23/1 -> Mux/23
  "IW{1,1}(23,:)'"/1 -> dotprod23/1
  dotprod22/1 -> Mux/22
  "IW{1,1}(22,:)'"/1 -> dotprod22/1
  dotprod21/1 -> Mux/21
  "IW{1,1}(21,:)'"/1 -> dotprod21/1
  dotprod20/1 -> Mux/20
  "IW{1,1}(20,:)'"/1 -> dotprod20/1
  dotprod19/1 -> Mux/19
  "IW{1,1}(19,:)'"/1 -> dotprod19/1
  dotprod18/1 -> Mux/18
  "IW{1,1}(18,:)'"/1 -> dotprod18/1
  dotprod17/1 -> Mux/17
  "IW{1,1}(17,:)'"/1 -> dotprod17/1
  dotprod16/1 -> Mux/16
  "IW{1,1}(16,:)'"/1 -> dotprod16/1
  dotprod15/1 -> Mux/15
  "IW{1,1}(15,:)'"/1 -> dotprod15/1
  dotprod14/1 -> Mux/14
  "IW{1,1}(14,:)'"/1 -> dotprod14/1
  dotprod13/1 -> Mux/13
  "IW{1,1}(13,:)'"/1 -> dotprod13/1
  dotprod12/1 -> Mux/12
  "IW{1,1}(12,:)'"/1 -> dotprod12/1
  dotprod11/1 -> Mux/11
  "IW{1,1}(11,:)'"/1 -> dotprod11/1
  dotprod10/1 -> Mux/10
  "IW{1,1}(10,:)'"/1 -> dotprod10/1
  dotprod9/1 -> Mux/9
  "IW{1,1}(9,:)'"/1 -> dotprod9/1
  dotprod8/1 -> Mux/8
  "IW{1,1}(8,:)'"/1 -> dotprod8/1
  dotprod7/1 -> Mux/7
  "IW{1,1}(7,:)'"/1 -> dotprod7/1
  dotprod6/1 -> Mux/6
  "IW{1,1}(6,:)'"/1 -> dotprod6/1
  dotprod5/1 -> Mux/5
  "IW{1,1}(5,:)'"/1 -> dotprod5/1
  dotprod4/1 -> Mux/4
  "IW{1,1}(4,:)'"/1 -> dotprod4/1
  dotprod3/1 -> Mux/3
  "IW{1,1}(3,:)'"/1 -> dotprod3/1
  dotprod2/1 -> Mux/2
  "IW{1,1}(2,:)'"/1 -> dotprod2/1
  dotprod1/1 -> Mux/1
